simulink model "solar_pv_protected_c07_circuit"  (R2026b)
settings: Solver=VariableStepAuto
model workspace (MAT data in the model file):
  candidate_owner = 'pv_protection_integration_20261023_r01'
  solar_edit_metadata.source = 'micropython-connected-drawing-20261019-r03'
  solar_edit_metadata.transform.pixels_per_mm = 7.87401574803
  solar_edit_metadata.transform.offset_mm = [0 0]
  solar_edit_metadata.transform.offset_px = [80 80]
  solar_edit_metadata.behavior_models_implemented = 0
libraries: fl_lib x149, ee_lib x16, ltc4364demo_lib x3, batteryecm_lib x1, solarprotect_lib x1
(part 1 of 16)
settings Model: PreStartFcn=error('solar:NativeMigrationIncomplete','標準部品への移行版です。専用IC等の動作モデルと実部品パラメータを設定してから、試験計画に沿って実行してください。');  Creator=hosik  LastModifiedBy=hosik
settings SimscapeCC: SimscapeLogType=all  SimscapeNominalValues="[{\"value\":\"1\",\"unit\":\"A\"},{\"value\":\"1\",\"unit\":\"bar\"},{\"value\":\"1\",\"unit\":\"cm^2\"},{\"value\":\"1\",\"unit\":\"cm^3/s\"},{\"value\":\"1\",\"unit\":\"kJ/kg\"},{\"value\":\"1\",\"unit\":\"kW\"},{\"value\":\"1\",\"unit\":\"l\"},{\"value\":\"1\",\"unit\":\"N\"},{\"value\":\"1\",\"unit\":\"N*m\"},{\"value\":\"1\",\"unit\":\"V\"},{\"value\":\"0.001\",\"unit\":\"Wb\"}]"  SimscapeUseEnergyAccounting=off

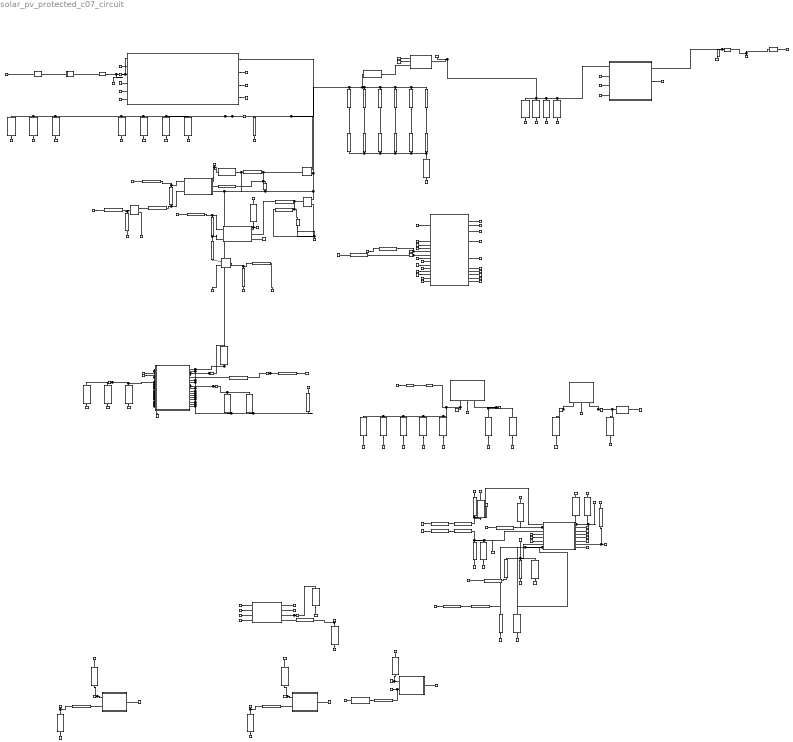
== system solar_pv_protected_c07_circuit ==
  note: 太陽光充電システム c07
  BT1 : batteryecm_lib/Battery  Description=|  Vnom=51.2 V  prm_dir=simscape.enum.battery.prm_dir.disabled  R1_dis=2 Ohm  R1_ch=2 Ohm  R1=2 Ohm  prm_AH=simscape.enum.battery.prm_AH.infinite  AH=100 A*hr  V1=11.5 V  AH1=25 A*hr  prm_R2=simscape.enum.battery.prm_R2.disabled  R2=2000 Ohm  Tmeas=298.15 K  charge_measurement_port=simscape.enum.battery.enable.no  prm_dyn=simscape.enum.battery.prm_dyn.off  Rp1=0.005 Ohm  tau1=30 s  Rp2=0.005 Ohm  tau2=30 s  Rp3=0.005 Ohm  tau3=30 s  Rp4=0.005 Ohm  tau4=30 s  Rp5=0.005 Ohm  tau5=30 s  prm_fade=simscape.enum.battery.prm_fade.disabled  N_fade=100  AH_fade=45 A*hr  R1_fade=2.02 Ohm  R1_ch_fade=2.02 Ohm  V1_fade=10.35 V  prm_age=simscape.enum.battery.prm_age.disabled  prm_age_OCV=simscape.enum.battery.prm_age_OCV.OCV  OCV_age=0.9  SOC_age=60  Tmeas_age=298.15 K  delta_time_age_vec=[0] d  temperature_age_vec=[273] K  OCV_scaling_age=2.2134e6  OCV_offset_age=1.632e6  temp_exp_age=0.515833569 V  t_exp_age=0.75  Vnom_T2=12 V  R1_T2=2.2 Ohm  R1_T2_dis=2.2 Ohm  R1_T2_ch=2.2 Ohm  V1_T2=11.4 V  R2_T2=2200 Ohm  Rp1_T2=0.005 Ohm  tau1_T2=30 s  Rp2_T2=0.005 Ohm  tau2_T2=30 s  Rp3_T2=0.005 Ohm  tau3_T2=30 s  Rp4_T2=0.005 Ohm  tau4_T2=30 s  Rp5_T2=0.005 Ohm  tau5_T2=30 s  Tmeas2=273.15 K  thermal_port=simscape.enum.thermaleffects.omit  thermal_mass=30000 J/K  i_specify=off  i_priority=None  i=0 A  i_nominal_specify=off  i_nominal_value=1  i_nominal_unit=A  v_specify=off  v_priority=None  v=0 V  v_nominal_specify=off  v_nominal_value=1  v_nominal_unit=V  charge_specify=off  charge_priority=High  charge=50 A*hr  charge_nominal_specify=off  charge_nominal_value=1  charge_nominal_unit=A*hr  num_cycles_specify=off  num_cycles_priority=High  num_cycles=0  num_cycles_nominal_specify=off  num_cycles_nominal_value=1  num_cycles_nominal_unit=1  temperature_specify=off  temperature_priority=High  temperature=298.15 K  temperature_nominal_specify=off  temperature_nominal_value=1  temperature_nominal_unit=K
      | この回路での名前　　; BT1
      | 部品名　　　　　　　; LiTime 51.2V 100Ah
      | この回路での役割　　; 太陽光で発電した電力を充電して蓄える、今回の設計対象の電池パック。
      | ここでの動き　　　　; 主充電経路から充電を受ける一方、別の補助電源分岐から制御回路などへ電力を供給する。充電器停止時にも電池側に電圧が残るため、逆流を防ぐ設計が必要になる。
      | 
      | 【詳しい働き・仕様・接続・確認の範囲】
      | 部品種別　　　　　　; 完成蓄電池パック
      | 公称値　　　　　　　; 51.2V 100Ah LiFePO4
      | 配置目的　　　　　　; 太陽光充電器の充電先。電池側に電圧源が存在することを表し、充電器停止時の逆流防止も検討対象にする。
      | 意図する動作　　　　; 公称51.2 V・100 AhのLiFePO4パックを設計対象とする。内部BMSの詳細動作、SOC・温度・内部抵抗の実測同定は未実施。
      | 端子と接続　　　　　; + + → BAT_RAW、- - → GND
      | モデルの範囲　　　　; Simscape電池ブロックへ既知の公称値を割り当てた図面用表現。LiTimeパックのSOC/温度依存・内部抵抗・BMSへ同定済みではない。
      | 確認の範囲　　　　　; 本説明は保存回路の部品情報・端子割当・既存設計意図を整理したもの。今回の説明更新によって新たな動作試験や実機検証を実施した意味ではない。
      | 設計記録　　　　　　; evaluation\component_annotations_20261022_r01\before_graph.json
      | evaluation\component_annotations_20261022_r01\before_metadata.json
      | evaluation\protection_capacitor_integration_20261021_r01\final_delivery\independent_readback\physical_bom.json
      | 
      | 【この説明欄の略語・記号】
      | 用語1　　　　　　　 ; BMS：Battery Management System（電池管理システム）。電池内部の監視・保護などを担当する仕組み。現モデルは実パックの詳細動作を同定したものではない。
      | 用語2　　　　　　　 ; SOC：State of Charge（充電状態）。電池に残る充電量の割合。電圧だけで正確に決まる量ではない。
      | 用語3　　　　　　　 ; LiFePO4：Lithium Iron Phosphate（リン酸鉄リチウム）。電池の正極材料を示す化学式。英語の頭文字を並べた略語ではない。
      | 用語4　　　　　　　 ; GND：Ground（回路の基準電位・電流帰路）。この図の共通基準。保護接地や大地への接続を意味するとは限らない。
      settings: AttributesFormatString=51.2V 100Ah LiFePO4
  C1 : fl_lib/Electrical/Electrical Elements/Capacitor  Description=|  c=2.2e-08 F  r=1e-6 Ohm  g=0 1/Ohm  i_specify=off  i_priority=None  i=0 A  i_nominal_specify=off  i_nominal_value=1  i_nominal_unit=A  v_specify=off  v_priority=None  v=0 V  v_nominal_specify=off  v_nominal_value=1  v_nominal_unit=V  vc_specify=off  vc_priority=High  vc=0 V  vc_nominal_specify=off  vc_nominal_value=1  vc_nominal_unit=V
      | この回路での名前　　; C1
      | 部品名　　　　　　　; C3225C0G2J223J230AA
      | この回路での役割　　; 主電力段のスイッチが切り替わった後に起こる、電圧の振動を抑えるためのコンデンサ。
      | ここでの動き　　　　; Q1・Q2の切替えで生じる振動に対し、抵抗R3〜R14と組み合わせて電流を流し、そのエネルギーを抵抗で消費する経路を作る。この組合せをスナバと呼ぶ。
      | 
      | 【詳しい働き・仕様・接続・確認の範囲】
      | 部品種別　　　　　　; 積層セラミックコンデンサ（MLCC）
      | 部品分類　　　　　　; 積層セラミックコンデンサ（MLCC）
      | 公称値　　　　　　　; 22 nF
      | 配置目的　　　　　　; SWスナバ。対象はQ1/Q2、R3〜R14、SW。
      | 意図する動作　　　　; スナバ抵抗とC1の往復ループをSW/QLソースに局所化。 スナバ機能は大容量CINと異なる。寄生・リンギング・パルス電力が未確認のため削除しない。
      | 端子と接続　　　　　; 1 p → SNUB_C、2 n → GND
      | モデルの範囲　　　　; Simscape標準コンデンサの集中定数表現。材質、DCバイアス、周波数依存ESR/ESL、寿命・温度特性を型番から自動再現するモデルではない。
      | モデル設定　　　　　; c=22 nF、r=1 µΩ、g=0 S。これらは保存モデルの設定値であり、すべてが実部品の保証値という意味ではない。
      | 損失の扱い　　　　　; 保存モデルの直列抵抗rと実部品の周波数・温度依存ESRは区別する。容量値が一致しても損失・リプル電流・寿命の成立確認にはならない。
      | 確認の範囲　　　　　; 本説明は保存回路の部品情報・端子割当・既存設計意図を整理したもの。今回の説明更新によって新たな動作試験や実機検証を実施した意味ではない。
      | 設計記録　　　　　　; evaluation\component_annotations_20261022_r01\before_graph.json
      | evaluation\component_annotations_20261022_r01\before_metadata.json
      | evaluation\protection_capacitor_integration_20261021_r01\final_delivery\independent_readback\physical_bom.json
      | evaluation\protection_capacitor_integration_20261021_r01\capacitor_review\capacitor_inventory_after_c04.json
      | 
      | 【周波数・ノイズと配置の説明】
      | 周波数面の役割　　　; スイッチング端の振動を抵抗と組み合わせて減衰させるスナバ容量。
      | 対象周波数の目安　　; 対象はQ1/Q2の切替えで励起される寄生共振の周波数。主スイッチング50 kHz仮定そのものより高い成分が対象になり得るが、現回路の共振周波数は未測定なのでMHzなどの固定値は割り当てない。
      | ノイズの発生源　　　; Q1/Q2、主配線の寄生インダクタンスとMOSFET等の寄生容量が、切替え時の急な電流・電圧変化によって振動する。
      | 他のコンデンサとの差; C8～C10は電源をまたぐバイパスで、本品22 nFはスナバ抵抗R3～R14と組み合わせて振動エネルギーを消費するための容量。
      | 周波数説明の範囲　　; この説明はスナバの設計意図。寄生共振、抵抗のパルス電力、損失、温度を含むこの値の最適性は未確認。
      | 周波数説明の根拠　　; 村田製作所：コンデンサのインピーダンス・ESRと周波数の関係
      | https://article.murata.com/en-global/article/impedance-esr-frequency-characteristics-in-capacitors
      | 
      | 【この説明欄の略語・記号】
      | 用語1　　　　　　　 ; MLCC：Multilayer Ceramic Capacitor（積層セラミックコンデンサ）。薄いセラミック誘電体と電極を重ねたコンデンサ。対象周波数は容量・実装・寄生成分で変わるため、MLCCという分類だけでは決めない。
      | 用語2　　　　　　　 ; ESR：Equivalent Series Resistance（等価直列抵抗）。コンデンサの損失を直列抵抗で表した量。周波数・温度で変わり、損失とリプル電圧に関係する。
      | 用語3　　　　　　　 ; ESL：Equivalent Series Inductance（等価直列インダクタンス）。端子や電極などの寄生インダクタンスを表す。高い周波数ではバイパス効果を制限する。
      | 用語4　　　　　　　 ; DC：Direct Current（直流）。ここでは直流電源または直流成分。DCバイアスはコンデンサに重なる直流電圧を指す。
      | 用語5　　　　　　　 ; MOSFET：Metal-Oxide-Semiconductor Field-Effect Transistor（金属・酸化膜・半導体構造の電界効果トランジスタ）。ゲートとソースの電圧でドレインとソースの導通を制御する素子。N-MOSはNチャネル型を表す。
      | 用語6　　　　　　　 ; GND：Ground（回路の基準電位・電流帰路）。この図の共通基準。保護接地や大地への接続を意味するとは限らない。
      | 用語7　　　　　　　 ; SW：Switching Node（スイッチング点）。主電力段の上下MOSFETとL1がつながる、電圧が高速に切り替わる点。GNDとは別電位。
      | 用語8　　　　　　　 ; CIN：Input Capacitor（入力側コンデンサ）。個別部品番号ではなく、入力側の容量群を指す機能名。
      | 用語9　　　　　　　 ; QH/QL：主電力段の上側・下側MOSFETを指す機能名。HはHigh側、LはLow側。この図のQ1/Q2との対応を回路説明で確認する。
      settings: AttributesFormatString=|
      | MLCC
      | 22 nF
  C10 : fl_lib/Electrical/Electrical Elements/Capacitor  Description=|  c=2.2000000000000001e-06 F  r=1e-6 Ohm  g=0 1/Ohm  i_specify=off  i_priority=None  i=0 A  i_nominal_specify=off  i_nominal_value=1  i_nominal_unit=A  v_specify=off  v_priority=None  v=0 V  v_nominal_specify=off  v_nominal_value=1  v_nominal_unit=V  vc_specify=off  vc_priority=High  vc=0 V  vc_nominal_specify=off  vc_nominal_value=1  vc_nominal_unit=V
      | この回路での名前　　; C10
      | 部品名　　　　　　　; C5750X7T2E225K250KE
      | この回路での役割　　; 主電力段のすぐ近くで速い電流変化を受け止め、遠い電源配線へ流れ出す高周波成分を減らすためのコンデンサ。
      | ここでの動き　　　　; 入力電源VINと共通GNDの間に2.2 µFを3個並列に置き、Q1・Q2が切り替わる瞬間の電流に短い往復経路を作る。C2〜C4の大きな電荷蓄積を補う役割。
      | 
      | 【詳しい働き・仕様・接続・確認の範囲】
      | 部品種別　　　　　　; 積層セラミックコンデンサ（MLCC）
      | 部品分類　　　　　　; 積層セラミックコンデンサ（MLCC）
      | 公称値　　　　　　　; 2.2 uF
      | 配置目的　　　　　　; 入力高速バイパス。対象はQ1ドレインとQ2ソース間のホットループ。
      | 意図する動作　　　　; 現構成は2.2 µFを3個。電力段付近でパルス電流の短い往復経路を作る意図。DCバイアス下の実効容量と高周波の分流・寄生は公称容量だけでは保証しない。
      | 端子と接続　　　　　; 2 n → GND、1 p → VIN
      | モデルの範囲　　　　; Simscape標準コンデンサの集中定数表現。材質、DCバイアス、周波数依存ESR/ESL、寿命・温度特性を型番から自動再現するモデルではない。
      | モデル設定　　　　　; c=2.2 µF、r=1 µΩ、g=0 S。これらは保存モデルの設定値であり、すべてが実部品の保証値という意味ではない。
      | 損失の扱い　　　　　; 保存モデルの直列抵抗rと実部品の周波数・温度依存ESRは区別する。容量値が一致しても損失・リプル電流・寿命の成立確認にはならない。
      | 確認の範囲　　　　　; 本説明は保存回路の部品情報・端子割当・既存設計意図を整理したもの。今回の説明更新によって新たな動作試験や実機検証を実施した意味ではない。
      | 設計記録　　　　　　; evaluation\component_annotations_20261022_r01\before_graph.json
      | evaluation\component_annotations_20261022_r01\before_metadata.json
      | evaluation\protection_capacitor_integration_20261021_r01\final_delivery\independent_readback\physical_bom.json
      | evaluation\protection_capacitor_integration_20261021_r01\capacitor_review\capacitor_inventory_after_c04.json
      | 
      | 【周波数・ノイズと配置の説明】
      | 材質の分類　　　　　; 本品の温度特性分類はX7T。-55～125 ℃の範囲で容量変化+22/-33%を規定する分類コードであり、英単語の略ではない。これは温度による変化の分類で、直流電圧を加えた際の実効容量や高周波特性は別に確認する。
      | 周波数面の役割　　　; 入力側の速い電流変化を電力段の近くで受け止め、遠い電源配線へ流れる高周波成分を減らす。
      | 対象周波数の目安　　; 主スイッチング周波数とその高調波、切替え端の速い変化を対象とする。主電力段の既存比較計算では50 kHzを仮定している。これは比較シナリオの値であり、今回の保存図から実行中PWM周波数を測定した値ではない。 50 kHzなら100 kHz、150 kHzなども成分となり、端の速さや寄生共振によってMHz域も検討対象になる。ただしMHz域での本品の有効性を保証した意味ではない。
      | ノイズの発生源　　　; Q1のオン期間に主電力段へ流れ込む入力電流が脈動し、Q1/Q2の切替え時には寄生容量の充放電電流も加わる。配線の寄生インダクタンスは急な電流変化を電圧の突起や振動に変える。
      | 他のコンデンサとの差; C2～C4の470 µF電解が比較的長い時間の電荷を補い、本品2.2 µFは短い局所経路を作る。C7フィルムとも分担し、3種類の役割には重なりがある。
      | 周波数説明の範囲　　; 狙うノイズの周波数と、この部品が実装後に有効な周波数範囲は別である。実効容量、等価直列抵抗、等価直列インダクタンス、配線を含む自己共振で変わるため、型番名や公称容量だけから有効帯域の上限を断定しない。
      | 周波数説明の根拠　　; TDK：C5750X7T2E225K250KE
      | https://product.tdk.com/ja/search/capacitor/ceramic/mlcc/info?part_no=C5750X7T2E225K250KE
      | 村田製作所：コンデンサのインピーダンス・ESRと周波数の関係
      | https://article.murata.com/en-global/article/impedance-esr-frequency-characteristics-in-capacitors
      | 村田製作所：コンデンサを使いこなす
      | https://www.murata.com/en-GB/products/emc/emifil/library/knowhow/basic/chapter06-p8
      | 
      | 【この説明欄の略語・記号】
      | 用語1　　　　　　　 ; MLCC：Multilayer Ceramic Capacitor（積層セラミックコンデンサ）。薄いセラミック誘電体と電極を重ねたコンデンサ。対象周波数は容量・実装・寄生成分で変わるため、MLCCという分類だけでは決めない。
      | 用語2　　　　　　　 ; ESR：Equivalent Series Resistance（等価直列抵抗）。コンデンサの損失を直列抵抗で表した量。周波数・温度で変わり、損失とリプル電圧に関係する。
      | 用語3　　　　　　　 ; ESL：Equivalent Series Inductance（等価直列インダクタンス）。端子や電極などの寄生インダクタンスを表す。高い周波数ではバイパス効果を制限する。
      | 用語4　　　　　　　 ; DC：Direct Current（直流）。ここでは直流電源または直流成分。DCバイアスはコンデンサに重なる直流電圧を指す。
      | 用語5　　　　　　　 ; X7T：セラミックコンデンサの温度特性記号。英語の頭文字ではなく分類コード。X＝下限−55 ℃、7＝上限+125 ℃、T＝容量変化+22%/−33%。直流バイアスによる容量変化は別に確認する。
      | 用語6　　　　　　　 ; PWM：Pulse Width Modulation（パルス幅変調）。周期に対するON時間の割合を変えて、スイッチの平均的な電力伝達を調整する方式。
      | 用語7　　　　　　　 ; GND：Ground（回路の基準電位・電流帰路）。この図の共通基準。保護接地や大地への接続を意味するとは限らない。
      | 用語8　　　　　　　 ; VIN/VOUT：入力電圧・出力電圧を表す端子／ネット名。INは入力、OUTは出力。電源変換器の電力端子なのか、検出用端子なのかは対象部品によって異なるため、端子と接続の説明に従う。
      settings: AttributesFormatString=|
      | MLCC
      | 2.2 µF
  C13 : fl_lib/Electrical/Electrical Elements/Capacitor  Description=|  c=0.00047 F  r=1e-6 Ohm  g=0 1/Ohm  i_specify=off  i_priority=None  i=0 A  i_nominal_specify=off  i_nominal_value=1  i_nominal_unit=A  v_specify=off  v_priority=None  v=0 V  v_nominal_specify=off  v_nominal_value=1  v_nominal_unit=V  vc_specify=off  vc_priority=High  vc=0 V  vc_nominal_specify=off  vc_nominal_value=1  vc_nominal_unit=V
      | この回路での名前　　; C13
      | 部品名　　　　　　　; 100ZLH470MEFC16X31.5
      | この回路での役割　　; インダクタL1から入る電流とバッテリーへ送る電流の差を、電荷の出し入れで一時的に受け持ち、降圧回路の出力電圧をならすためのコンデンサ。
      | ここでの動き　　　　; インダクタL1と電流検出抵抗R2を通った後の出力VOUTと共通GNDの間に、470 µFを2個並列に置く。保護回路が遮断すると、VOUTからバッテリー側のP_COUTへ向かう正側の給電経路が切り離される。GND側の基準は共通のまま。
      | 
      | 【詳しい働き・仕様・接続・確認の範囲】
      | 部品種別　　　　　　; アルミ電解コンデンサ（有極性）
      | 部品分類　　　　　　; アルミ電解コンデンサ（有極性）
      | 公称値　　　　　　　; 470 uF
      | 配置目的　　　　　　; 出力バルク。対象はL1・R2の後のVOUT、保護回路の入力側。
      | 意図する動作　　　　; 大容量電解として出力の電荷・エネルギーを受け持つ。C15/C16の高速バイパスと併用する。保護OFF時、下流BAT_PLUSのP_COUTとは別ノードになる。
      | 端子と接続　　　　　; 1 p → VOUT、2 n → GND
      | 比較する部品　　　　; C15/C16はMLCC 10 µF。本品は電解470 µFであり、同じ容量・材質の部品ではない。
      | モデルの範囲　　　　; Simscape標準コンデンサの集中定数表現。材質、DCバイアス、周波数依存ESR/ESL、寿命・温度特性を型番から自動再現するモデルではない。
      | モデル設定　　　　　; c=470 µF、r=1 µΩ、g=0 S。これらは保存モデルの設定値であり、すべてが実部品の保証値という意味ではない。
      | 損失の扱い　　　　　; 保存モデルの直列抵抗rと実部品の周波数・温度依存ESRは区別する。容量値が一致しても損失・リプル電流・寿命の成立確認にはならない。
      | 確認の範囲　　　　　; 本説明は保存回路の部品情報・端子割当・既存設計意図を整理したもの。今回の説明更新によって新たな動作試験や実機検証を実施した意味ではない。
      | 設計記録　　　　　　; evaluation\component_annotations_20261022_r01\before_graph.json
      | evaluation\component_annotations_20261022_r01\before_metadata.json
      | evaluation\protection_capacitor_integration_20261021_r01\final_delivery\independent_readback\physical_bom.json
      | evaluation\protection_capacitor_integration_20261021_r01\capacitor_review\capacitor_inventory_after_c04.json
      | 
      | 【周波数・ノイズと配置の説明】
      | 周波数面の役割　　　; 出力側で電荷を蓄え、インダクタ電流とバッテリーへ送る電流の差を受け止める。
      | 対象周波数の目安　　; 負荷や制御の変化による低い周波数側と、主スイッチング周期に残る出力リプルを対象とする。主電力段の既存比較計算では50 kHzを仮定している。これは比較シナリオの値であり、今回の保存図から実行中PWM周波数を測定した値ではない。
      | ノイズの発生源　　　; L1の電流はスイッチング周期で増減する。この電流と下流へ流れる電流の差がコンデンサへ入り、出力電圧の脈動を生む。
      | 他のコンデンサとの差; 470 µF×2個は蓄積量を担当し、10 µFのC15/C16はより速い高調波・突起への局所帰路を補う。保護出力側のP_COUTとは遮断時に別ノードとなる。
      | 周波数説明の範囲　　; 狙うノイズの周波数と、この部品が実装後に有効な周波数範囲は別である。実効容量、等価直列抵抗、等価直列インダクタンス、配線を含む自己共振で変わるため、型番名や公称容量だけから有効帯域の上限を断定しない。
      | 周波数説明の根拠　　; 村田製作所：コンデンサのインピーダンス・ESRと周波数の関係
      | https://article.murata.com/en-global/article/impedance-esr-frequency-characteristics-in-capacitors
      | 村田製作所：コンデンサを使いこなす
      | https://www.murata.com/en-GB/products/emc/emifil/library/knowhow/basic/chapter06-p8
      | 
      | 【この説明欄の略語・記号】
      | 用語1　　　　　　　 ; MLCC：Multilayer Ceramic Capacitor（積層セラミックコンデンサ）。薄いセラミック誘電体と電極を重ねたコンデンサ。対象周波数は容量・実装・寄生成分で変わるため、MLCCという分類だけでは決めない。
      | 用語2　　　　　　　 ; ESR：Equivalent Series Resistance（等価直列抵抗）。コンデンサの損失を直列抵抗で表した量。周波数・温度で変わり、損失とリプル電圧に関係する。
      | 用語3　　　　　　　 ; ESL：Equivalent Series Inductance（等価直列インダクタンス）。端子や電極などの寄生インダクタンスを表す。高い周波数ではバイパス効果を制限する。
      | 用語4　　　　　　　 ; DC：Direct Current（直流）。ここでは直流電源または直流成分。DCバイアスはコンデンサに重なる直流電圧を指す。
      | 用語5　　　　　　　 ; PWM：Pulse Width Modulation（パルス幅変調）。周期に対するON時間の割合を変えて、スイッチの平均的な電力伝達を調整する方式。
      | 用語6　　　　　　　 ; GND：Ground（回路の基準電位・電流帰路）。この図の共通基準。保護接地や大地への接続を意味するとは限らない。
      | 用語7　　　　　　　 ; VIN/VOUT：入力電圧・出力電圧を表す端子／ネット名。INは入力、OUTは出力。電源変換器の電力端子なのか、検出用端子なのかは対象部品によって異なるため、端子と接続の説明に従う。
      settings: AttributesFormatString=|
      | 電解
      | 470 µF
  C14 : fl_lib/Electrical/Electrical Elements/Capacitor  Description=|  c=0.00047 F  r=1e-6 Ohm  g=0 1/Ohm  i_specify=off  i_priority=None  i=0 A  i_nominal_specify=off  i_nominal_value=1  i_nominal_unit=A  v_specify=off  v_priority=None  v=0 V  v_nominal_specify=off  v_nominal_value=1  v_nominal_unit=V  vc_specify=off  vc_priority=High  vc=0 V  vc_nominal_specify=off  vc_nominal_value=1  vc_nominal_unit=V
      | この回路での名前　　; C14
      | 部品名　　　　　　　; 100ZLH470MEFC16X31.5
      | この回路での役割　　; インダクタL1から入る電流とバッテリーへ送る電流の差を、電荷の出し入れで一時的に受け持ち、降圧回路の出力電圧をならすためのコンデンサ。
      | ここでの動き　　　　; インダクタL1と電流検出抵抗R2を通った後の出力VOUTと共通GNDの間に、470 µFを2個並列に置く。保護回路が遮断すると、VOUTからバッテリー側のP_COUTへ向かう正側の給電経路が切り離される。GND側の基準は共通のまま。
      | 
      | 【詳しい働き・仕様・接続・確認の範囲】
      | 部品種別　　　　　　; アルミ電解コンデンサ（有極性）
      | 部品分類　　　　　　; アルミ電解コンデンサ（有極性）
      | 公称値　　　　　　　; 470 uF
      | 配置目的　　　　　　; 出力バルク。対象はL1・R2の後のVOUT、保護回路の入力側。
      | 意図する動作　　　　; 大容量電解として出力の電荷・エネルギーを受け持つ。C15/C16の高速バイパスと併用する。保護OFF時、下流BAT_PLUSのP_COUTとは別ノードになる。
      | 端子と接続　　　　　; 1 p → VOUT、2 n → GND
      | 比較する部品　　　　; C15/C16はMLCC 10 µF。本品は電解470 µFであり、同じ容量・材質の部品ではない。
      | モデルの範囲　　　　; Simscape標準コンデンサの集中定数表現。材質、DCバイアス、周波数依存ESR/ESL、寿命・温度特性を型番から自動再現するモデルではない。
      | モデル設定　　　　　; c=470 µF、r=1 µΩ、g=0 S。これらは保存モデルの設定値であり、すべてが実部品の保証値という意味ではない。
      | 損失の扱い　　　　　; 保存モデルの直列抵抗rと実部品の周波数・温度依存ESRは区別する。容量値が一致しても損失・リプル電流・寿命の成立確認にはならない。
      | 確認の範囲　　　　　; 本説明は保存回路の部品情報・端子割当・既存設計意図を整理したもの。今回の説明更新によって新たな動作試験や実機検証を実施した意味ではない。
      | 設計記録　　　　　　; evaluation\component_annotations_20261022_r01\before_graph.json
      | evaluation\component_annotations_20261022_r01\before_metadata.json
      | evaluation\protection_capacitor_integration_20261021_r01\final_delivery\independent_readback\physical_bom.json
      | evaluation\protection_capacitor_integration_20261021_r01\capacitor_review\capacitor_inventory_after_c04.json
      | 
      | 【周波数・ノイズと配置の説明】
      | 周波数面の役割　　　; 出力側で電荷を蓄え、インダクタ電流とバッテリーへ送る電流の差を受け止める。
      | 対象周波数の目安　　; 負荷や制御の変化による低い周波数側と、主スイッチング周期に残る出力リプルを対象とする。主電力段の既存比較計算では50 kHzを仮定している。これは比較シナリオの値であり、今回の保存図から実行中PWM周波数を測定した値ではない。
      | ノイズの発生源　　　; L1の電流はスイッチング周期で増減する。この電流と下流へ流れる電流の差がコンデンサへ入り、出力電圧の脈動を生む。
      | 他のコンデンサとの差; 470 µF×2個は蓄積量を担当し、10 µFのC15/C16はより速い高調波・突起への局所帰路を補う。保護出力側のP_COUTとは遮断時に別ノードとなる。
      | 周波数説明の範囲　　; 狙うノイズの周波数と、この部品が実装後に有効な周波数範囲は別である。実効容量、等価直列抵抗、等価直列インダクタンス、配線を含む自己共振で変わるため、型番名や公称容量だけから有効帯域の上限を断定しない。
      | 周波数説明の根拠　　; 村田製作所：コンデンサのインピーダンス・ESRと周波数の関係
      | https://article.murata.com/en-global/article/impedance-esr-frequency-characteristics-in-capacitors
      | 村田製作所：コンデンサを使いこなす
      | https://www.murata.com/en-GB/products/emc/emifil/library/knowhow/basic/chapter06-p8
      | 
      | 【この説明欄の略語・記号】
      | 用語1　　　　　　　 ; MLCC：Multilayer Ceramic Capacitor（積層セラミックコンデンサ）。薄いセラミック誘電体と電極を重ねたコンデンサ。対象周波数は容量・実装・寄生成分で変わるため、MLCCという分類だけでは決めない。
      | 用語2　　　　　　　 ; ESR：Equivalent Series Resistance（等価直列抵抗）。コンデンサの損失を直列抵抗で表した量。周波数・温度で変わり、損失とリプル電圧に関係する。
      | 用語3　　　　　　　 ; ESL：Equivalent Series Inductance（等価直列インダクタンス）。端子や電極などの寄生インダクタンスを表す。高い周波数ではバイパス効果を制限する。
      | 用語4　　　　　　　 ; DC：Direct Current（直流）。ここでは直流電源または直流成分。DCバイアスはコンデンサに重なる直流電圧を指す。
      | 用語5　　　　　　　 ; PWM：Pulse Width Modulation（パルス幅変調）。周期に対するON時間の割合を変えて、スイッチの平均的な電力伝達を調整する方式。
      | 用語6　　　　　　　 ; GND：Ground（回路の基準電位・電流帰路）。この図の共通基準。保護接地や大地への接続を意味するとは限らない。
      | 用語7　　　　　　　 ; VIN/VOUT：入力電圧・出力電圧を表す端子／ネット名。INは入力、OUTは出力。電源変換器の電力端子なのか、検出用端子なのかは対象部品によって異なるため、端子と接続の説明に従う。
      settings: AttributesFormatString=|
      | 電解
      | 470 µF
  C15 : fl_lib/Electrical/Electrical Elements/Capacitor  Description=|  c=1e-05 F  r=1e-6 Ohm  g=0 1/Ohm  i_specify=off  i_priority=None  i=0 A  i_nominal_specify=off  i_nominal_value=1  i_nominal_unit=A  v_specify=off  v_priority=None  v=0 V  v_nominal_specify=off  v_nominal_value=1  v_nominal_unit=V  vc_specify=off  vc_priority=High  vc=0 V  vc_nominal_specify=off  vc_nominal_value=1  vc_nominal_unit=V
      | この回路での名前　　; C15
      | 部品名　　　　　　　; GRM32EC72A106KE05L
      | この回路での役割　　; 降圧回路の出力側で速い電圧・電流の変化を受け止め、大容量の出力コンデンサを補うためのコンデンサ。
      | ここでの動き　　　　; 出力VOUTと共通GNDの間で、高周波の電流が近くを往復する経路を作る。電荷を多く蓄えるC13・C14と併用し、保護回路へ入る電源の変動を抑える設計。
      | 
      | 【詳しい働き・仕様・接続・確認の範囲】
      | 部品種別　　　　　　; 積層セラミックコンデンサ（MLCC）
      | 部品分類　　　　　　; 積層セラミックコンデンサ（MLCC）
      | 公称値　　　　　　　; 10 uF
      | 配置目的　　　　　　; 出力高速バイパス。対象はVOUT、出力バルク、保護VIN。
      | 意図する動作　　　　; MLCCとして出力側の高周波電流を局所的に受け持ち、C13/C14の大容量電解を補う。同じVOUT–GND接続でも材質・容量・周波数特性と役割が異なる。DCバイアス下の実効容量は10 µFより小さくなり得る。
      | 端子と接続　　　　　; 1 p → VOUT、2 n → GND
      | 比較する部品　　　　; C13/C14は電解470 µF。本品はMLCC 10 µF。並列でも担当する周波数域・電荷量・実効容量の条件が異なる。
      | モデルの範囲　　　　; Simscape標準コンデンサの集中定数表現。材質、DCバイアス、周波数依存ESR/ESL、寿命・温度特性を型番から自動再現するモデルではない。
      | モデル設定　　　　　; c=10 µF、r=1 µΩ、g=0 S。これらは保存モデルの設定値であり、すべてが実部品の保証値という意味ではない。
      | 損失の扱い　　　　　; 保存モデルの直列抵抗rと実部品の周波数・温度依存ESRは区別する。容量値が一致しても損失・リプル電流・寿命の成立確認にはならない。
      | 確認の範囲　　　　　; 本説明は保存回路の部品情報・端子割当・既存設計意図を整理したもの。今回の説明更新によって新たな動作試験や実機検証を実施した意味ではない。
      | 設計記録　　　　　　; evaluation\component_annotations_20261022_r01\before_graph.json
      | evaluation\component_annotations_20261022_r01\before_metadata.json
      | evaluation\protection_capacitor_integration_20261021_r01\final_delivery\independent_readback\physical_bom.json
      | evaluation\protection_capacitor_integration_20261021_r01\capacitor_review\capacitor_inventory_after_c04.json
      | 
      | 【周波数・ノイズと配置の説明】
      | 材質の分類　　　　　; 本品の温度特性分類はX7S。-55～125 ℃の範囲で容量変化±22%を規定する分類コードであり、英単語の略ではない。これは温度による変化の分類で、直流電圧を加えた際の実効容量や高周波特性は別に確認する。
      | 周波数面の役割　　　; 出力側の高周波電流を局所的に受け、C13/C14の電解を補う。
      | 対象周波数の目安　　; 主スイッチングの高調波や切替え端から結合する高周波成分を対象にする。主電力段の既存比較計算では50 kHzを仮定している。これは比較シナリオの値であり、今回の保存図から実行中PWM周波数を測定した値ではない。 MHz域まで調べるべき成分があり得るが、本品の有効帯域や実回路のノイズ分布は未測定。
      | ノイズの発生源　　　; L1のリプル電流、Q1/Q2の切替え、寄生容量/共通配線を通る結合が出力側に影響する。
      | 他のコンデンサとの差; C13/C14の470 µF電解と比較すると公称容量は小さいが、短い配線と低い寄生成分で速い変化への経路を作る意図。10 µFは直流電圧印加時の実効容量保証値ではない。
      | 周波数説明の範囲　　; 狙うノイズの周波数と、この部品が実装後に有効な周波数範囲は別である。実効容量、等価直列抵抗、等価直列インダクタンス、配線を含む自己共振で変わるため、型番名や公称容量だけから有効帯域の上限を断定しない。
      | 周波数説明の根拠　　; 村田製作所：GRM32EC72A106KE05 Reference Sheet
      | https://search.murata.co.jp/Ceramy/image/img/A01X/G101/ENG/GRM32EC72A106KE05-01.pdf
      | 村田製作所：コンデンサのインピーダンス・ESRと周波数の関係
      | https://article.murata.com/en-global/article/impedance-esr-frequency-characteristics-in-capacitors
      | 村田製作所：コンデンサを使いこなす
      | https://www.murata.com/en-GB/products/emc/emifil/library/knowhow/basic/chapter06-p8
      | TDK：電解コンデンサからMLCCへの置換ガイド
      | https://product.tdk.com/en/techlibrary/solutionguide/mlcc_replace-guide.html
      | 
      | 【この説明欄の略語・記号】
      | 用語1　　　　　　　 ; MLCC：Multilayer Ceramic Capacitor（積層セラミックコンデンサ）。薄いセラミック誘電体と電極を重ねたコンデンサ。対象周波数は容量・実装・寄生成分で変わるため、MLCCという分類だけでは決めない。
      | 用語2　　　　　　　 ; ESR：Equivalent Series Resistance（等価直列抵抗）。コンデンサの損失を直列抵抗で表した量。周波数・温度で変わり、損失とリプル電圧に関係する。
      | 用語3　　　　　　　 ; ESL：Equivalent Series Inductance（等価直列インダクタンス）。端子や電極などの寄生インダクタンスを表す。高い周波数ではバイパス効果を制限する。
      | 用語4　　　　　　　 ; DC：Direct Current（直流）。ここでは直流電源または直流成分。DCバイアスはコンデンサに重なる直流電圧を指す。
      | 用語5　　　　　　　 ; X7S：セラミックコンデンサの温度特性記号。英語の頭文字ではなく分類コード。X＝下限−55 ℃、7＝上限+125 ℃、S＝その範囲の容量変化±22%。直流バイアスによる容量変化は別に確認する。
      | 用語6　　　　　　　 ; PWM：Pulse Width Modulation（パルス幅変調）。周期に対するON時間の割合を変えて、スイッチの平均的な電力伝達を調整する方式。
      | 用語7　　　　　　　 ; GND：Ground（回路の基準電位・電流帰路）。この図の共通基準。保護接地や大地への接続を意味するとは限らない。
      | 用語8　　　　　　　 ; VIN/VOUT：入力電圧・出力電圧を表す端子／ネット名。INは入力、OUTは出力。電源変換器の電力端子なのか、検出用端子なのかは対象部品によって異なるため、端子と接続の説明に従う。
      settings: AttributesFormatString=|
      | MLCC
      | 10 µF
  C16 : fl_lib/Electrical/Electrical Elements/Capacitor  Description=|  c=1e-05 F  r=1e-6 Ohm  g=0 1/Ohm  i_specify=off  i_priority=None  i=0 A  i_nominal_specify=off  i_nominal_value=1  i_nominal_unit=A  v_specify=off  v_priority=None  v=0 V  v_nominal_specify=off  v_nominal_value=1  v_nominal_unit=V  vc_specify=off  vc_priority=High  vc=0 V  vc_nominal_specify=off  vc_nominal_value=1  vc_nominal_unit=V
      | この回路での名前　　; C16
      | 部品名　　　　　　　; GRM32EC72A106KE05L
      | この回路での役割　　; 降圧回路の出力側で速い電圧・電流の変化を受け止め、大容量の出力コンデンサを補うためのコンデンサ。
      | ここでの動き　　　　; 出力VOUTと共通GNDの間で、高周波の電流が近くを往復する経路を作る。電荷を多く蓄えるC13・C14と併用し、保護回路へ入る電源の変動を抑える設計。
      | 
      | 【詳しい働き・仕様・接続・確認の範囲】
      | 部品種別　　　　　　; 積層セラミックコンデンサ（MLCC）
      | 部品分類　　　　　　; 積層セラミックコンデンサ（MLCC）
      | 公称値　　　　　　　; 10 uF
      | 配置目的　　　　　　; 出力高速バイパス。対象はVOUT、出力バルク、保護VIN。
      | 意図する動作　　　　; MLCCとして出力側の高周波電流を局所的に受け持ち、C13/C14の大容量電解を補う。同じVOUT–GND接続でも材質・容量・周波数特性と役割が異なる。DCバイアス下の実効容量は10 µFより小さくなり得る。
      | 端子と接続　　　　　; 1 p → VOUT、2 n → GND
      | 比較する部品　　　　; C13/C14は電解470 µF。本品はMLCC 10 µF。並列でも担当する周波数域・電荷量・実効容量の条件が異なる。
      | モデルの範囲　　　　; Simscape標準コンデンサの集中定数表現。材質、DCバイアス、周波数依存ESR/ESL、寿命・温度特性を型番から自動再現するモデルではない。
      | モデル設定　　　　　; c=10 µF、r=1 µΩ、g=0 S。これらは保存モデルの設定値であり、すべてが実部品の保証値という意味ではない。
      | 損失の扱い　　　　　; 保存モデルの直列抵抗rと実部品の周波数・温度依存ESRは区別する。容量値が一致しても損失・リプル電流・寿命の成立確認にはならない。
      | 確認の範囲　　　　　; 本説明は保存回路の部品情報・端子割当・既存設計意図を整理したもの。今回の説明更新によって新たな動作試験や実機検証を実施した意味ではない。
      | 設計記録　　　　　　; evaluation\component_annotations_20261022_r01\before_graph.json
      | evaluation\component_annotations_20261022_r01\before_metadata.json
      | evaluation\protection_capacitor_integration_20261021_r01\final_delivery\independent_readback\physical_bom.json
      | evaluation\protection_capacitor_integration_20261021_r01\capacitor_review\capacitor_inventory_after_c04.json
      | 
      | 【周波数・ノイズと配置の説明】
      | 材質の分類　　　　　; 本品の温度特性分類はX7S。-55～125 ℃の範囲で容量変化±22%を規定する分類コードであり、英単語の略ではない。これは温度による変化の分類で、直流電圧を加えた際の実効容量や高周波特性は別に確認する。
      | 周波数面の役割　　　; 出力側の高周波電流を局所的に受け、C13/C14の電解を補う。
      | 対象周波数の目安　　; 主スイッチングの高調波や切替え端から結合する高周波成分を対象にする。主電力段の既存比較計算では50 kHzを仮定している。これは比較シナリオの値であり、今回の保存図から実行中PWM周波数を測定した値ではない。 MHz域まで調べるべき成分があり得るが、本品の有効帯域や実回路のノイズ分布は未測定。
      | ノイズの発生源　　　; L1のリプル電流、Q1/Q2の切替え、寄生容量/共通配線を通る結合が出力側に影響する。
      | 他のコンデンサとの差; C13/C14の470 µF電解と比較すると公称容量は小さいが、短い配線と低い寄生成分で速い変化への経路を作る意図。10 µFは直流電圧印加時の実効容量保証値ではない。
      | 周波数説明の範囲　　; 狙うノイズの周波数と、この部品が実装後に有効な周波数範囲は別である。実効容量、等価直列抵抗、等価直列インダクタンス、配線を含む自己共振で変わるため、型番名や公称容量だけから有効帯域の上限を断定しない。
      | 周波数説明の根拠　　; 村田製作所：GRM32EC72A106KE05 Reference Sheet
      | https://search.murata.co.jp/Ceramy/image/img/A01X/G101/ENG/GRM32EC72A106KE05-01.pdf
      | 村田製作所：コンデンサのインピーダンス・ESRと周波数の関係
      | https://article.murata.com/en-global/article/impedance-esr-frequency-characteristics-in-capacitors
      | 村田製作所：コンデンサを使いこなす
      | https://www.murata.com/en-GB/products/emc/emifil/library/knowhow/basic/chapter06-p8
      | TDK：電解コンデンサからMLCCへの置換ガイド
      | https://product.tdk.com/en/techlibrary/solutionguide/mlcc_replace-guide.html
      | 
      | 【この説明欄の略語・記号】
      | 用語1　　　　　　　 ; MLCC：Multilayer Ceramic Capacitor（積層セラミックコンデンサ）。薄いセラミック誘電体と電極を重ねたコンデンサ。対象周波数は容量・実装・寄生成分で変わるため、MLCCという分類だけでは決めない。
      | 用語2　　　　　　　 ; ESR：Equivalent Series Resistance（等価直列抵抗）。コンデンサの損失を直列抵抗で表した量。周波数・温度で変わり、損失とリプル電圧に関係する。
      | 用語3　　　　　　　 ; ESL：Equivalent Series Inductance（等価直列インダクタンス）。端子や電極などの寄生インダクタンスを表す。高い周波数ではバイパス効果を制限する。
      | 用語4　　　　　　　 ; DC：Direct Current（直流）。ここでは直流電源または直流成分。DCバイアスはコンデンサに重なる直流電圧を指す。
      | 用語5　　　　　　　 ; X7S：セラミックコンデンサの温度特性記号。英語の頭文字ではなく分類コード。X＝下限−55 ℃、7＝上限+125 ℃、S＝その範囲の容量変化±22%。直流バイアスによる容量変化は別に確認する。
      | 用語6　　　　　　　 ; PWM：Pulse Width Modulation（パルス幅変調）。周期に対するON時間の割合を変えて、スイッチの平均的な電力伝達を調整する方式。
      | 用語7　　　　　　　 ; GND：Ground（回路の基準電位・電流帰路）。この図の共通基準。保護接地や大地への接続を意味するとは限らない。
      | 用語8　　　　　　　 ; VIN/VOUT：入力電圧・出力電圧を表す端子／ネット名。INは入力、OUTは出力。電源変換器の電力端子なのか、検出用端子なのかは対象部品によって異なるため、端子と接続の説明に従う。
      settings: AttributesFormatString=|
      | MLCC
      | 10 µF
  C17 : fl_lib/Electrical/Electrical Elements/Capacitor  Description=|  c=1e-07 F  r=1e-6 Ohm  g=0 1/Ohm  i_specify=off  i_priority=None  i=0 A  i_nominal_specify=off  i_nominal_value=1  i_nominal_unit=A  v_specify=off  v_priority=None  v=0 V  v_nominal_specify=off  v_nominal_value=1  v_nominal_unit=V  vc_specify=off  vc_priority=High  vc=0 V  vc_nominal_specify=off  vc_nominal_value=1  vc_nominal_unit=V
      | この回路での名前　　; C17
      | 部品名　　　　　　　; C0805C104K4RACTU
      | この回路での役割　　; 測定電圧を数値に変換するU1の3.3 V電源を、瞬間的な変動から支えるためのコンデンサ。
      | ここでの動き　　　　; U1の電源端子の近くで一時的な電流を供給し、高周波の電流に短い帰り道を作る。離れた電源側の容量だけに任せず、U1自身の近くに置く役割。
      | 
      | 【詳しい働き・仕様・接続・確認の範囲】
      | 部品種別　　　　　　; 積層セラミックコンデンサ（MLCC）
      | 部品分類　　　　　　; 積層セラミックコンデンサ（MLCC）
      | 公称値　　　　　　　; 100 nF
      | 配置目的　　　　　　; ADC電源バイパス。対象ICはU1（MCP3208-CI/SL）。
      | 意図する動作　　　　; U1電源ピン直近、静かな帰路。SPIやゲート帰路と共有インピーダンスを抑える。 100nF局所バイパス。C18やPico搭載Cは配線インダクタンス越しの代替にならない。
      | 端子と接続　　　　　; 1 1 → 3V3、2 2 → GND
      | モデルの範囲　　　　; Simscape標準コンデンサの集中定数表現。材質、DCバイアス、周波数依存ESR/ESL、寿命・温度特性を型番から自動再現するモデルではない。
      | モデル設定　　　　　; c=100 nF、r=1 µΩ、g=0 S。これらは保存モデルの設定値であり、すべてが実部品の保証値という意味ではない。
      | 損失の扱い　　　　　; 保存モデルの直列抵抗rと実部品の周波数・温度依存ESRは区別する。容量値が一致しても損失・リプル電流・寿命の成立確認にはならない。
      | 確認の範囲　　　　　; 本説明は保存回路の部品情報・端子割当・既存設計意図を整理したもの。今回の説明更新によって新たな動作試験や実機検証を実施した意味ではない。
      | 設計記録　　　　　　; evaluation\component_annotations_20261022_r01\before_graph.json
      | evaluation\component_annotations_20261022_r01\before_metadata.json
      | evaluation\protection_capacitor_integration_20261021_r01\final_delivery\independent_readback\physical_bom.json
      | evaluation\protection_capacitor_integration_20261021_r01\capacitor_review\capacitor_inventory_after_c04.json
      | evaluation\layout_readability_20261022_r01\capacitor_review\exact_snapshot_capacitor_review.json
      | 
      | 【周波数・ノイズと配置の説明】
      | 周波数面の役割　　　; U1（MCP3208、アナログ電圧を数値に変換するIC）の電源端子直近で、瞬間的な電流を供給する局所バイパス。
      | 対象周波数の目安　　; そのICの内部動作や周辺の通信、周囲のスイッチングによる高周波成分を対象にする。100 nFという容量だけから「何MHzまで効く」とは決められない。
      | ノイズの発生源　　　; IC内部の回路動作に伴う電源電流の変化、3.3 V配線を経由する電源変動、近傍のデジタル信号やゲート駆動からの結合。
      | 他のコンデンサとの差; 離れたC18や電源装置側の大きな容量は低い周波数側の蓄積を補う。配線の寄生インダクタンスがあるため、同じ電源ネットでもIC直近の本品を完全に代替できない。
      | 周波数説明の範囲　　; 狙うノイズの周波数と、この部品が実装後に有効な周波数範囲は別である。実効容量、等価直列抵抗、等価直列インダクタンス、配線を含む自己共振で変わるため、型番名や公称容量だけから有効帯域の上限を断定しない。
      | 周波数説明の根拠　　; TDK：Low-ESL Multilayer Ceramic Capacitors
      | https://product.tdk.com/system/files/dam/doc/content/emc-guidebook/en/eemc_product_01.pdf
      | 村田製作所：コンデンサを使いこなす
      | https://www.murata.com/en-GB/products/emc/emifil/library/knowhow/basic/chapter06-p8
      | 
      | 【この説明欄の略語・記号】
      | 用語1　　　　　　　 ; MLCC：Multilayer Ceramic Capacitor（積層セラミックコンデンサ）。薄いセラミック誘電体と電極を重ねたコンデンサ。対象周波数は容量・実装・寄生成分で変わるため、MLCCという分類だけでは決めない。
      | 用語2　　　　　　　 ; ESR：Equivalent Series Resistance（等価直列抵抗）。コンデンサの損失を直列抵抗で表した量。周波数・温度で変わり、損失とリプル電圧に関係する。
      | 用語3　　　　　　　 ; ESL：Equivalent Series Inductance（等価直列インダクタンス）。端子や電極などの寄生インダクタンスを表す。高い周波数ではバイパス効果を制限する。
      | 用語4　　　　　　　 ; DC：Direct Current（直流）。ここでは直流電源または直流成分。DCバイアスはコンデンサに重なる直流電圧を指す。
      | 用語5　　　　　　　 ; ADC：Analog-to-Digital Converter（アナログ・デジタル変換器）。測定電圧をデジタル値へ変換する回路。電流や温度も、センサーで電圧へ変換した後に読み取る。
      | 用語6　　　　　　　 ; IC：Integrated Circuit（集積回路）。複数の電子素子と機能を小さな半導体チップに集積した部品。
      | 用語7　　　　　　　 ; SPI：Serial Peripheral Interface（同期式シリアル通信）。クロックとデータ線を使う通信方式。本回路ではRP2040と外付け測定用ADCの通信に使う。
      | 用語8　　　　　　　 ; GND：Ground（回路の基準電位・電流帰路）。この図の共通基準。保護接地や大地への接続を意味するとは限らない。
      settings: AttributesFormatString=|
      | MLCC
      | 100 nF
  C18 : fl_lib/Electrical/Electrical Elements/Capacitor  Description=|  c=2.2e-06 F  r=1e-6 Ohm  g=0 1/Ohm  i_specify=off  i_priority=None  i=0 A  i_nominal_specify=off  i_nominal_value=1  i_nominal_unit=A  v_specify=off  v_priority=None  v=0 V  v_nominal_specify=off  v_nominal_value=1  v_nominal_unit=V  vc_specify=off  vc_priority=High  vc=0 V  vc_nominal_specify=off  vc_nominal_value=1  vc_nominal_unit=V
      | この回路での名前　　; C18
      | 部品名　　　　　　　; C3225X7R2A225K230AB
      | この回路での役割　　; 3.3 Vで動く計測回路の近くに電荷を蓄え、計測回路全体の消費電流の変化を支えるためのコンデンサ。
      | ここでの動き　　　　; 計測回路へ給電する3V3と共通GNDの間に2.2 µFを置き、電流が一時的に増えたときに電荷を補う。各ICの直近にあるC17などの100 nFとは、蓄える量と配置先を分担する。
      | 
      | 【詳しい働き・仕様・接続・確認の範囲】
      | 部品種別　　　　　　; 積層セラミックコンデンサ（MLCC）
      | 部品分類　　　　　　; 積層セラミックコンデンサ（MLCC）
      | 公称値　　　　　　　; 2.2 uF
      | 配置目的　　　　　　; 3V3測定群の局所バルク。対象ICはU1（MCP3208-CI/SL）。
      | 意図する動作　　　　; ADC/計測群の3V3給電枝。旧名称LDO_OUTは機能確認なしに維持理由としない。 Pico3V3からの配線長と過渡が未確定。旧LDO出力由来だが計測群バルクとして残し、重複候補は保留。
      | 端子と接続　　　　　; 1 1 → 3V3、2 2 → GND
      | モデルの範囲　　　　; Simscape標準コンデンサの集中定数表現。材質、DCバイアス、周波数依存ESR/ESL、寿命・温度特性を型番から自動再現するモデルではない。
      | モデル設定　　　　　; c=2.2 µF、r=1 µΩ、g=0 S。これらは保存モデルの設定値であり、すべてが実部品の保証値という意味ではない。
      | 損失の扱い　　　　　; 保存モデルの直列抵抗rと実部品の周波数・温度依存ESRは区別する。容量値が一致しても損失・リプル電流・寿命の成立確認にはならない。
      | 確認の範囲　　　　　; 本説明は保存回路の部品情報・端子割当・既存設計意図を整理したもの。今回の説明更新によって新たな動作試験や実機検証を実施した意味ではない。
      | 設計記録　　　　　　; evaluation\component_annotations_20261022_r01\before_graph.json
      | evaluation\component_annotations_20261022_r01\before_metadata.json
      | evaluation\protection_capacitor_integration_20261021_r01\final_delivery\independent_readback\physical_bom.json
      | evaluation\protection_capacitor_integration_20261021_r01\capacitor_review\capacitor_inventory_after_c04.json
      | evaluation\layout_readability_20261022_r01\capacitor_review\exact_snapshot_capacitor_review.json
      | 
      | 【周波数・ノイズと配置の説明】
      | 周波数面の役割　　　; 3.3 V計測回路へまとまった電荷を供給する局所バルク。
      | 対象周波数の目安　　; 計測群の動作開始や複数ICの消費電流変化に伴う比較的低い周波数側の変動を、100 nF局所バイパス群と分担する。実効帯域の数値は未確定。
      | ノイズの発生源　　　; ADCや計測ICの消費電流変化、Pico側から計測群へ至る給電配線の電圧降下。
      | 他のコンデンサとの差; 本品はMLCCでも蓄積側の役割を持つ。C17等の100 nFを各IC直近へ置く理由とは異なり、MLCCをすべて高速ノイズ専用とは扱わない。
      | 周波数説明の範囲　　; 狙うノイズの周波数と、この部品が実装後に有効な周波数範囲は別である。実効容量、等価直列抵抗、等価直列インダクタンス、配線を含む自己共振で変わるため、型番名や公称容量だけから有効帯域の上限を断定しない。
      | 周波数説明の根拠　　; TDK：Low-ESL Multilayer Ceramic Capacitors
      | https://product.tdk.com/system/files/dam/doc/content/emc-guidebook/en/eemc_product_01.pdf
      | 村田製作所：コンデンサを使いこなす
      | https://www.murata.com/en-GB/products/emc/emifil/library/knowhow/basic/chapter06-p8
      | 
      | 【この説明欄の略語・記号】
      | 用語1　　　　　　　 ; MLCC：Multilayer Ceramic Capacitor（積層セラミックコンデンサ）。薄いセラミック誘電体と電極を重ねたコンデンサ。対象周波数は容量・実装・寄生成分で変わるため、MLCCという分類だけでは決めない。
      | 用語2　　　　　　　 ; ESR：Equivalent Series Resistance（等価直列抵抗）。コンデンサの損失を直列抵抗で表した量。周波数・温度で変わり、損失とリプル電圧に関係する。
      | 用語3　　　　　　　 ; ESL：Equivalent Series Inductance（等価直列インダクタンス）。端子や電極などの寄生インダクタンスを表す。高い周波数ではバイパス効果を制限する。
      | 用語4　　　　　　　 ; DC：Direct Current（直流）。ここでは直流電源または直流成分。DCバイアスはコンデンサに重なる直流電圧を指す。
      | 用語5　　　　　　　 ; ADC：Analog-to-Digital Converter（アナログ・デジタル変換器）。測定電圧をデジタル値へ変換する回路。電流や温度も、センサーで電圧へ変換した後に読み取る。
      | 用語6　　　　　　　 ; IC：Integrated Circuit（集積回路）。複数の電子素子と機能を小さな半導体チップに集積した部品。
      | 用語7　　　　　　　 ; LDO：Low-Dropout Regulator（低ドロップアウトのリニア電圧調整器）。入力と出力の電圧差が小さい条件でも動作できる電圧調整器。LDO_OUTはその出力を表す設計上の名前。
      | 用語8　　　　　　　 ; GND：Ground（回路の基準電位・電流帰路）。この図の共通基準。保護接地や大地への接続を意味するとは限らない。
      settings: AttributesFormatString=|
      | MLCC
      | 2.2 µF
  C19 : fl_lib/Electrical/Electrical Elements/Capacitor  Description=|  c=1e-07 F  r=1e-6 Ohm  g=0 1/Ohm  i_specify=off  i_priority=None  i=0 A  i_nominal_specify=off  i_nominal_value=1  i_nominal_unit=A  v_specify=off  v_priority=None  v=0 V  v_nominal_specify=off  v_nominal_value=1  v_nominal_unit=V  vc_specify=off  vc_priority=High  vc=0 V  vc_nominal_specify=off  vc_nominal_value=1  vc_nominal_unit=V
      | この回路での名前　　; C19
      | 部品名　　　　　　　; CC0603KRX7R9BB104
      | この回路での役割　　; 太陽光パネル側の入力電圧を測る信号の速い揺れを抑え、U1が読み取りやすくするためのコンデンサ。
      | ここでの動き　　　　; 分圧抵抗R16〜R18で下げた測定電圧を、U1のCH0へ入れる直前のADC_VPVと共通GNDの間で受ける。抵抗と組み合わせて速い変化を弱め、読み取り時の電荷を補う一方、測定値の変化には遅れが加わる。
      | 
      | 【詳しい働き・仕様・接続・確認の範囲】
      | 部品種別　　　　　　; 積層セラミックコンデンサ（MLCC）
      | 部品分類　　　　　　; 積層セラミックコンデンサ（MLCC）
      | 公称値　　　　　　　; 100 nF
      | 配置目的　　　　　　; 電圧分圧RC/ADC取得電荷。対象はR16/R17/R18→U1CH0。
      | 意図する動作　　　　; ADC入力近傍、分圧下側の静かなGNDへ帰還。 分圧Thevenin約3.229kΩとの100nFでτ≈323µs。削除はノイズ/取得と制御遅延を変える。維持して時定数を計測条件へ渡す。
      | 端子と接続　　　　　; 1 1 → ADC_VPV、2 2 → GND
      | モデルの範囲　　　　; Simscape標準コンデンサの集中定数表現。材質、DCバイアス、周波数依存ESR/ESL、寿命・温度特性を型番から自動再現するモデルではない。
      | モデル設定　　　　　; c=100 nF、r=1 µΩ、g=0 S。これらは保存モデルの設定値であり、すべてが実部品の保証値という意味ではない。
      | 損失の扱い　　　　　; 保存モデルの直列抵抗rと実部品の周波数・温度依存ESRは区別する。容量値が一致しても損失・リプル電流・寿命の成立確認にはならない。
      | 確認の範囲　　　　　; 本説明は保存回路の部品情報・端子割当・既存設計意図を整理したもの。今回の説明更新によって新たな動作試験や実機検証を実施した意味ではない。
      | 設計記録　　　　　　; evaluation\component_annotations_20261022_r01\before_graph.json
      | evaluation\component_annotations_20261022_r01\before_metadata.json
      | evaluation\protection_capacitor_integration_20261021_r01\final_delivery\independent_readback\physical_bom.json
      | evaluation\protection_capacitor_integration_20261021_r01\capacitor_review\capacitor_inventory_after_c04.json
      | 
      | 【周波数・ノイズと配置の説明】
      | 周波数面の役割　　　; パネル側入力電圧を測る分圧回路の低域通過フィルタと、ADCの取得時に必要な局所電荷の保持。
      | 対象周波数の目安　　; 公称値で(75 kΩ+75 kΩ)と3.3 kΩの並列合成抵抗は約3.229 kΩ。100 nFとの理想1次RC遮断周波数は約493 Hz、時定数は約323 µs。遮断周波数以上を徐々に弱める特性で、その周波数を超えると急にゼロになるものではない。
      | ノイズの発生源　　　; 電力段のリプルが分圧器へ入り、測定配線へスイッチングの突起や通信信号が結合する。ADCがCH0の入力電荷を取り込む際にも瞬間的な電流が流れる。
      | 他のコンデンサとの差; 同じ100 nFでも電源バイパスC17等とは役割が異なる。ここでは抵抗と組み合わせて測定値の変化を平滑化し、応答にも遅れを加える。
      | 周波数説明の範囲　　; この周波数は公称抵抗・公称容量、理想信号源、高入力インピーダンスを仮定した回路計算。ADCの取得スイッチ、実効容量、信号源インピーダンスを含む総整定時間やサンプリング適合の検証結果ではない。
      | 周波数説明の根拠　　; TI Precision Labs：Passive Components and Circuits
      | https://www.ti.com/content/dam/videos/external-videos/en-us/4/3816841626001/6119035031001.mp4/subassets/passive_components_and_circuits_2.pdf
      | Microchip：MCP3204/3208 datasheet
      | https://ww1.microchip.com/downloads/en/DeviceDoc/21298E.pdf
      | 
      | 【この説明欄の略語・記号】
      | 用語1　　　　　　　 ; MLCC：Multilayer Ceramic Capacitor（積層セラミックコンデンサ）。薄いセラミック誘電体と電極を重ねたコンデンサ。対象周波数は容量・実装・寄生成分で変わるため、MLCCという分類だけでは決めない。
      | 用語2　　　　　　　 ; ESR：Equivalent Series Resistance（等価直列抵抗）。コンデンサの損失を直列抵抗で表した量。周波数・温度で変わり、損失とリプル電圧に関係する。
      | 用語3　　　　　　　 ; ESL：Equivalent Series Inductance（等価直列インダクタンス）。端子や電極などの寄生インダクタンスを表す。高い周波数ではバイパス効果を制限する。
      | 用語4　　　　　　　 ; DC：Direct Current（直流）。ここでは直流電源または直流成分。DCバイアスはコンデンサに重なる直流電圧を指す。
      | 用語5　　　　　　　 ; ADC：Analog-to-Digital Converter（アナログ・デジタル変換器）。測定電圧をデジタル値へ変換する回路。電流や温度も、センサーで電圧へ変換した後に読み取る。
      | 用語6　　　　　　　 ; CH：Channel（測定チャネル）。CH0〜CH7はADCの入力番号であり、同時測定を意味しない。
      | 用語7　　　　　　　 ; RC：Resistor-Capacitor（抵抗とコンデンサの組合せ）。主に測定信号のフィルタや時定数を作る。カットオフ周波数は実際の接続と抵抗・容量から求める。
      | 用語8　　　　　　　 ; τ：Time Constant（時定数）。1次RC回路では抵抗Rと容量Cの積で、単位は秒。入力が急変した後の応答の速さを表す。τだけ経過すると最終変化量の約63%まで変化する。
      | 用語9　　　　　　　 ; GND：Ground（回路の基準電位・電流帰路）。この図の共通基準。保護接地や大地への接続を意味するとは限らない。
      settings: AttributesFormatString=|
      | MLCC
      | 100 nF
  C2 : fl_lib/Electrical/Electrical Elements/Capacitor  Description=|  c=0.00046999999999999999 F  r=1e-6 Ohm  g=0 1/Ohm  i_specify=off  i_priority=None  i=0 A  i_nominal_specify=off  i_nominal_value=1  i_nominal_unit=A  v_specify=off  v_priority=None  v=0 V  v_nominal_specify=off  v_nominal_value=1  v_nominal_unit=V  vc_specify=off  vc_priority=High  vc=0 V  vc_nominal_specify=off  vc_nominal_value=1  vc_nominal_unit=V
      | この回路での名前　　; C2
      | 部品名　　　　　　　; UCY2C471MHD
      | この回路での役割　　; 太陽光パネルから給電される主電力段の入力側に電荷を蓄え、入力電圧の落ち込みや変動を抑えるためのコンデンサ。
      | ここでの動き　　　　; 入力電源VINと共通GNDの間に470 µFを3個並列に置き、降圧回路が電流を必要とするときに電荷を補う。速い変化への対応は、近くのC7〜C10と分担する設計。
      | 
      | 【詳しい働き・仕様・接続・確認の範囲】
      | 部品種別　　　　　　; アルミ電解コンデンサ（有極性）
      | 部品分類　　　　　　; アルミ電解コンデンサ（有極性）
      | 公称値　　　　　　　; 470 uF
      | 配置目的　　　　　　; 入力バルク。対象はL2入力フィルタとQ1/Q2電力段。
      | 意図する動作　　　　; VIN–GND間の入力バルクとして、降圧電力段が必要とする電荷を供給し入力電圧変動を抑える。現構成は470 µFを3個。分流・ESR・温度上昇・配線寄生の適合は別評価。
      | 端子と接続　　　　　; 2 n → GND、1 p → VIN
      | モデルの範囲　　　　; Simscape標準コンデンサの集中定数表現。材質、DCバイアス、周波数依存ESR/ESL、寿命・温度特性を型番から自動再現するモデルではない。
      | モデル設定　　　　　; c=470 µF、r=1 µΩ、g=0 S。これらは保存モデルの設定値であり、すべてが実部品の保証値という意味ではない。
      | 損失の扱い　　　　　; 保存モデルの直列抵抗rと実部品の周波数・温度依存ESRは区別する。容量値が一致しても損失・リプル電流・寿命の成立確認にはならない。
      | 確認の範囲　　　　　; 本説明は保存回路の部品情報・端子割当・既存設計意図を整理したもの。今回の説明更新によって新たな動作試験や実機検証を実施した意味ではない。
      | 設計記録　　　　　　; evaluation\component_annotations_20261022_r01\before_graph.json
      | evaluation\component_annotations_20261022_r01\before_metadata.json
      | evaluation\protection_capacitor_integration_20261021_r01\final_delivery\independent_readback\physical_bom.json
      | evaluation\protection_capacitor_integration_20261021_r01\capacitor_review\capacitor_inventory_after_c04.json
      | 
      | 【周波数・ノイズと配置の説明】
      | 周波数面の役割　　　; 入力電圧の比較的ゆっくりした変動を抑え、主電力段が必要な電荷を蓄える。
      | 対象周波数の目安　　; 起動・日射/負荷変動などの低い周波数側から、主スイッチング周期の電荷出入りまでを受け持つ。主電力段の既存比較計算では50 kHzを仮定している。これは比較シナリオの値であり、今回の保存図から実行中PWM周波数を測定した値ではない。
      | ノイズの発生源　　　; Q1のオン期間に入力から電流を取り出すため、入力電流は脈動する。パネル/配線/L2側がすぐ補えない電流をこの容量群が補う。
      | 他のコンデンサとの差; 470 µF×3個の電解は蓄積量を担当する。C7のフィルムとC8～C10のMLCCは速い電流変化への局所経路を補う。同じ周波数で複数群が分担し、境界周波数で役割が切り替わるわけではない。
      | 周波数説明の範囲　　; 狙うノイズの周波数と、この部品が実装後に有効な周波数範囲は別である。実効容量、等価直列抵抗、等価直列インダクタンス、配線を含む自己共振で変わるため、型番名や公称容量だけから有効帯域の上限を断定しない。
      | 周波数説明の根拠　　; 村田製作所：コンデンサのインピーダンス・ESRと周波数の関係
      | https://article.murata.com/en-global/article/impedance-esr-frequency-characteristics-in-capacitors
      | 村田製作所：コンデンサを使いこなす
      | https://www.murata.com/en-GB/products/emc/emifil/library/knowhow/basic/chapter06-p8
      | 
      | 【この説明欄の略語・記号】
      | 用語1　　　　　　　 ; MLCC：Multilayer Ceramic Capacitor（積層セラミックコンデンサ）。薄いセラミック誘電体と電極を重ねたコンデンサ。対象周波数は容量・実装・寄生成分で変わるため、MLCCという分類だけでは決めない。
      | 用語2　　　　　　　 ; ESR：Equivalent Series Resistance（等価直列抵抗）。コンデンサの損失を直列抵抗で表した量。周波数・温度で変わり、損失とリプル電圧に関係する。
      | 用語3　　　　　　　 ; ESL：Equivalent Series Inductance（等価直列インダクタンス）。端子や電極などの寄生インダクタンスを表す。高い周波数ではバイパス効果を制限する。
      | 用語4　　　　　　　 ; DC：Direct Current（直流）。ここでは直流電源または直流成分。DCバイアスはコンデンサに重なる直流電圧を指す。
      | 用語5　　　　　　　 ; PWM：Pulse Width Modulation（パルス幅変調）。周期に対するON時間の割合を変えて、スイッチの平均的な電力伝達を調整する方式。
      | 用語6　　　　　　　 ; GND：Ground（回路の基準電位・電流帰路）。この図の共通基準。保護接地や大地への接続を意味するとは限らない。
      | 用語7　　　　　　　 ; VIN/VOUT：入力電圧・出力電圧を表す端子／ネット名。INは入力、OUTは出力。電源変換器の電力端子なのか、検出用端子なのかは対象部品によって異なるため、端子と接続の説明に従う。
      settings: AttributesFormatString=|
      | 電解
      | 470 µF
  C20 : fl_lib/Electrical/Electrical Elements/Capacitor  Description=|  c=1e-07 F  r=1e-6 Ohm  g=0 1/Ohm  i_specify=off  i_priority=None  i=0 A  i_nominal_specify=off  i_nominal_value=1  i_nominal_unit=A  v_specify=off  v_priority=None  v=0 V  v_nominal_specify=off  v_nominal_value=1  v_nominal_unit=V  vc_specify=off  vc_priority=High  vc=0 V  vc_nominal_specify=off  vc_nominal_value=1  vc_nominal_unit=V
      | この回路での名前　　; C20
      | 部品名　　　　　　　; CC0603KRX7R9BB104
      | この回路での役割　　; 保護回路に入る前の出力電圧を測る信号の速い揺れを抑え、U1が読み取りやすくするためのコンデンサ。
      | ここでの動き　　　　; 分圧抵抗R19〜R21で下げた測定電圧を、U1のCH2へ入れる直前のADC_VOUTと共通GNDの間で受ける。抵抗と組み合わせて速い変化を弱め、読み取り時の電荷を補う一方、測定値の変化には遅れが加わる。
      | 
      | 【詳しい働き・仕様・接続・確認の範囲】
      | 部品種別　　　　　　; 積層セラミックコンデンサ（MLCC）
      | 部品分類　　　　　　; 積層セラミックコンデンサ（MLCC）
      | 公称値　　　　　　　; 100 nF
      | 配置目的　　　　　　; 電圧分圧RC/ADC取得電荷。対象はR19/R20/R21→U1CH2。
      | 意図する動作　　　　; ADC入力近傍、分圧下側の静かなGNDへ帰還。 分圧Thevenin約3.229kΩとの100nFでτ≈323µs。削除はノイズ/取得と制御遅延を変える。維持して時定数を計測条件へ渡す。
      | 端子と接続　　　　　; 1 1 → ADC_VOUT、2 2 → GND
      | モデルの範囲　　　　; Simscape標準コンデンサの集中定数表現。材質、DCバイアス、周波数依存ESR/ESL、寿命・温度特性を型番から自動再現するモデルではない。
      | モデル設定　　　　　; c=100 nF、r=1 µΩ、g=0 S。これらは保存モデルの設定値であり、すべてが実部品の保証値という意味ではない。
      | 損失の扱い　　　　　; 保存モデルの直列抵抗rと実部品の周波数・温度依存ESRは区別する。容量値が一致しても損失・リプル電流・寿命の成立確認にはならない。
      | 確認の範囲　　　　　; 本説明は保存回路の部品情報・端子割当・既存設計意図を整理したもの。今回の説明更新によって新たな動作試験や実機検証を実施した意味ではない。
      | 設計記録　　　　　　; evaluation\component_annotations_20261022_r01\before_graph.json
      | evaluation\component_annotations_20261022_r01\before_metadata.json
      | evaluation\protection_capacitor_integration_20261021_r01\final_delivery\independent_readback\physical_bom.json
      | evaluation\protection_capacitor_integration_20261021_r01\capacitor_review\capacitor_inventory_after_c04.json
      | 
      | 【周波数・ノイズと配置の説明】
      | 周波数面の役割　　　; 保護前の出力電圧を測る分圧回路の低域通過フィルタと、ADCの取得時に必要な局所電荷の保持。
      | 対象周波数の目安　　; 公称値で(75 kΩ+75 kΩ)と3.3 kΩの並列合成抵抗は約3.229 kΩ。100 nFとの理想1次RC遮断周波数は約493 Hz、時定数は約323 µs。遮断周波数以上を徐々に弱める特性で、その周波数を超えると急にゼロになるものではない。
      | ノイズの発生源　　　; 電力段のリプルが分圧器へ入り、測定配線へスイッチングの突起や通信信号が結合する。ADCがCH2の入力電荷を取り込む際にも瞬間的な電流が流れる。
      | 他のコンデンサとの差; 同じ100 nFでも電源バイパスC17等とは役割が異なる。ここでは抵抗と組み合わせて測定値の変化を平滑化し、応答にも遅れを加える。
      | 周波数説明の範囲　　; この周波数は公称抵抗・公称容量、理想信号源、高入力インピーダンスを仮定した回路計算。ADCの取得スイッチ、実効容量、信号源インピーダンスを含む総整定時間やサンプリング適合の検証結果ではない。
      | 周波数説明の根拠　　; TI Precision Labs：Passive Components and Circuits
      | https://www.ti.com/content/dam/videos/external-videos/en-us/4/3816841626001/6119035031001.mp4/subassets/passive_components_and_circuits_2.pdf
      | Microchip：MCP3204/3208 datasheet
      | https://ww1.microchip.com/downloads/en/DeviceDoc/21298E.pdf
      | 
      | 【この説明欄の略語・記号】
      | 用語1　　　　　　　 ; MLCC：Multilayer Ceramic Capacitor（積層セラミックコンデンサ）。薄いセラミック誘電体と電極を重ねたコンデンサ。対象周波数は容量・実装・寄生成分で変わるため、MLCCという分類だけでは決めない。
      | 用語2　　　　　　　 ; ESR：Equivalent Series Resistance（等価直列抵抗）。コンデンサの損失を直列抵抗で表した量。周波数・温度で変わり、損失とリプル電圧に関係する。
      | 用語3　　　　　　　 ; ESL：Equivalent Series Inductance（等価直列インダクタンス）。端子や電極などの寄生インダクタンスを表す。高い周波数ではバイパス効果を制限する。
      | 用語4　　　　　　　 ; DC：Direct Current（直流）。ここでは直流電源または直流成分。DCバイアスはコンデンサに重なる直流電圧を指す。
      | 用語5　　　　　　　 ; ADC：Analog-to-Digital Converter（アナログ・デジタル変換器）。測定電圧をデジタル値へ変換する回路。電流や温度も、センサーで電圧へ変換した後に読み取る。
      | 用語6　　　　　　　 ; CH：Channel（測定チャネル）。CH0〜CH7はADCの入力番号であり、同時測定を意味しない。
      | 用語7　　　　　　　 ; RC：Resistor-Capacitor（抵抗とコンデンサの組合せ）。主に測定信号のフィルタや時定数を作る。カットオフ周波数は実際の接続と抵抗・容量から求める。
      | 用語8　　　　　　　 ; τ：Time Constant（時定数）。1次RC回路では抵抗Rと容量Cの積で、単位は秒。入力が急変した後の応答の速さを表す。τだけ経過すると最終変化量の約63%まで変化する。
      | 用語9　　　　　　　 ; GND：Ground（回路の基準電位・電流帰路）。この図の共通基準。保護接地や大地への接続を意味するとは限らない。
      | 用語10　　　　　　　; VIN/VOUT：入力電圧・出力電圧を表す端子／ネット名。INは入力、OUTは出力。電源変換器の電力端子なのか、検出用端子なのかは対象部品によって異なるため、端子と接続の説明に従う。
      settings: AttributesFormatString=|
      | MLCC
      | 100 nF
  C21 : fl_lib/Electrical/Electrical Elements/Capacitor  Description=|  c=1e-07 F  r=1e-6 Ohm  g=0 1/Ohm  i_specify=off  i_priority=None  i=0 A  i_nominal_specify=off  i_nominal_value=1  i_nominal_unit=A  v_specify=off  v_priority=None  v=0 V  v_nominal_specify=off  v_nominal_value=1  v_nominal_unit=V  vc_specify=off  vc_priority=High  vc=0 V  vc_nominal_specify=off  vc_nominal_value=1  vc_nominal_unit=V
      | この回路での名前　　; C21
      | 部品名　　　　　　　; CC0603KRX7R9BB104
      | この回路での役割　　; バッテリー電圧を測る信号の速い揺れを抑え、U1が読み取りやすくするためのコンデンサ。
      | ここでの動き　　　　; 分圧抵抗R22〜R24で下げた測定電圧を、U1のCH6へ入れる直前のADC_VBATと共通GNDの間で受ける。抵抗と組み合わせて速い変化を弱め、読み取り時の電荷を補う一方、測定値の変化には遅れが加わる。
      | 
      | 【詳しい働き・仕様・接続・確認の範囲】
      | 部品種別　　　　　　; 積層セラミックコンデンサ（MLCC）
      | 部品分類　　　　　　; 積層セラミックコンデンサ（MLCC）
      | 公称値　　　　　　　; 100 nF
      | 配置目的　　　　　　; 電圧分圧RC/ADC取得電荷。対象はR22/R23/R24→U1CH6。
      | 意図する動作　　　　; ADC入力近傍、分圧下側の静かなGNDへ帰還。 分圧Thevenin約3.229kΩとの100nFでτ≈323µs。削除はノイズ/取得と制御遅延を変える。維持して時定数を計測条件へ渡す。
      | 端子と接続　　　　　; 1 1 → ADC_VBAT、2 2 → GND
      | モデルの範囲　　　　; Simscape標準コンデンサの集中定数表現。材質、DCバイアス、周波数依存ESR/ESL、寿命・温度特性を型番から自動再現するモデルではない。
      | モデル設定　　　　　; c=100 nF、r=1 µΩ、g=0 S。これらは保存モデルの設定値であり、すべてが実部品の保証値という意味ではない。
      | 損失の扱い　　　　　; 保存モデルの直列抵抗rと実部品の周波数・温度依存ESRは区別する。容量値が一致しても損失・リプル電流・寿命の成立確認にはならない。
      | 確認の範囲　　　　　; 本説明は保存回路の部品情報・端子割当・既存設計意図を整理したもの。今回の説明更新によって新たな動作試験や実機検証を実施した意味ではない。
      | 設計記録　　　　　　; evaluation\component_annotations_20261022_r01\before_graph.json
      | evaluation\component_annotations_20261022_r01\before_metadata.json
      | evaluation\protection_capacitor_integration_20261021_r01\final_delivery\independent_readback\physical_bom.json
      | evaluation\protection_capacitor_integration_20261021_r01\capacitor_review\capacitor_inventory_after_c04.json
      | 
      | 【周波数・ノイズと配置の説明】
      | 周波数面の役割　　　; バッテリー電圧を測る分圧回路の低域通過フィルタと、ADCの取得時に必要な局所電荷の保持。
      | 対象周波数の目安　　; 公称値で(75 kΩ+75 kΩ)と3.3 kΩの並列合成抵抗は約3.229 kΩ。100 nFとの理想1次RC遮断周波数は約493 Hz、時定数は約323 µs。遮断周波数以上を徐々に弱める特性で、その周波数を超えると急にゼロになるものではない。
      | ノイズの発生源　　　; 電力段のリプルが分圧器へ入り、測定配線へスイッチングの突起や通信信号が結合する。ADCがCH6の入力電荷を取り込む際にも瞬間的な電流が流れる。
      | 他のコンデンサとの差; 同じ100 nFでも電源バイパスC17等とは役割が異なる。ここでは抵抗と組み合わせて測定値の変化を平滑化し、応答にも遅れを加える。
      | 周波数説明の範囲　　; この周波数は公称抵抗・公称容量、理想信号源、高入力インピーダンスを仮定した回路計算。ADCの取得スイッチ、実効容量、信号源インピーダンスを含む総整定時間やサンプリング適合の検証結果ではない。
      | 周波数説明の根拠　　; TI Precision Labs：Passive Components and Circuits
      | https://www.ti.com/content/dam/videos/external-videos/en-us/4/3816841626001/6119035031001.mp4/subassets/passive_components_and_circuits_2.pdf
      | Microchip：MCP3204/3208 datasheet
      | https://ww1.microchip.com/downloads/en/DeviceDoc/21298E.pdf
      | 
      | 【この説明欄の略語・記号】
      | 用語1　　　　　　　 ; MLCC：Multilayer Ceramic Capacitor（積層セラミックコンデンサ）。薄いセラミック誘電体と電極を重ねたコンデンサ。対象周波数は容量・実装・寄生成分で変わるため、MLCCという分類だけでは決めない。
      | 用語2　　　　　　　 ; ESR：Equivalent Series Resistance（等価直列抵抗）。コンデンサの損失を直列抵抗で表した量。周波数・温度で変わり、損失とリプル電圧に関係する。
      | 用語3　　　　　　　 ; ESL：Equivalent Series Inductance（等価直列インダクタンス）。端子や電極などの寄生インダクタンスを表す。高い周波数ではバイパス効果を制限する。
      | 用語4　　　　　　　 ; DC：Direct Current（直流）。ここでは直流電源または直流成分。DCバイアスはコンデンサに重なる直流電圧を指す。
      | 用語5　　　　　　　 ; ADC：Analog-to-Digital Converter（アナログ・デジタル変換器）。測定電圧をデジタル値へ変換する回路。電流や温度も、センサーで電圧へ変換した後に読み取る。
      | 用語6　　　　　　　 ; CH：Channel（測定チャネル）。CH0〜CH7はADCの入力番号であり、同時測定を意味しない。
      | 用語7　　　　　　　 ; RC：Resistor-Capacitor（抵抗とコンデンサの組合せ）。主に測定信号のフィルタや時定数を作る。カットオフ周波数は実際の接続と抵抗・容量から求める。
      | 用語8　　　　　　　 ; τ：Time Constant（時定数）。1次RC回路では抵抗Rと容量Cの積で、単位は秒。入力が急変した後の応答の速さを表す。τだけ経過すると最終変化量の約63%まで変化する。
      | 用語9　　　　　　　 ; GND：Ground（回路の基準電位・電流帰路）。この図の共通基準。保護接地や大地への接続を意味するとは限らない。
      settings: AttributesFormatString=|
      | MLCC
      | 100 nF
  C23 : fl_lib/Electrical/Electrical Elements/Capacitor  Description=|  c=1e-07 F  r=1e-6 Ohm  g=0 1/Ohm  i_specify=off  i_priority=None  i=0 A  i_nominal_specify=off  i_nominal_value=1  i_nominal_unit=A  v_specify=off  v_priority=None  v=0 V  v_nominal_specify=off  v_nominal_value=1  v_nominal_unit=V  vc_specify=off  vc_priority=High  vc=0 V  vc_nominal_specify=off  vc_nominal_value=1  vc_nominal_unit=V
      | この回路での名前　　; C23
      | 部品名　　　　　　　; CC0603KRX7R9BB104
      | この回路での役割　　; パネル電流の測定信号から速い電気的な揺れを減らし、U1が読み取りやすくするためのコンデンサ。
      | ここでの動き　　　　; 電流検出ICの出力を抵抗R25に通し、その先のADC_IPVと共通GNDの間に100 nFを置いてU1のCH1へ渡す。信号をならすため、容量を変えると測定とソフトウェア保護の応答速度にも影響する。
      | 
      | 【詳しい働き・仕様・接続・確認の範囲】
      | 部品種別　　　　　　; 積層セラミックコンデンサ（MLCC）
      | 部品分類　　　　　　; 積層セラミックコンデンサ（MLCC）
      | 公称値　　　　　　　; 100 nF
      | 配置目的　　　　　　; 電流信号RC/ADC取得電荷。対象はR25100ΩとU1CH1。
      | 意図する動作　　　　; ADC入力側のRC帰路、INA出力から100Ωで分離。 τ10µs/fc15.9kHz。電流変化をソフト停止へ使う時間応答に影響するため維持。
      | 端子と接続　　　　　; 1 1 → ADC_IPV、2 2 → GND
      | モデルの範囲　　　　; Simscape標準コンデンサの集中定数表現。材質、DCバイアス、周波数依存ESR/ESL、寿命・温度特性を型番から自動再現するモデルではない。
      | モデル設定　　　　　; c=100 nF、r=1 µΩ、g=0 S。これらは保存モデルの設定値であり、すべてが実部品の保証値という意味ではない。
      | 損失の扱い　　　　　; 保存モデルの直列抵抗rと実部品の周波数・温度依存ESRは区別する。容量値が一致しても損失・リプル電流・寿命の成立確認にはならない。
      | 確認の範囲　　　　　; 本説明は保存回路の部品情報・端子割当・既存設計意図を整理したもの。今回の説明更新によって新たな動作試験や実機検証を実施した意味ではない。
      | 設計記録　　　　　　; evaluation\component_annotations_20261022_r01\before_graph.json
      | evaluation\component_annotations_20261022_r01\before_metadata.json
      | evaluation\protection_capacitor_integration_20261021_r01\final_delivery\independent_readback\physical_bom.json
      | evaluation\protection_capacitor_integration_20261021_r01\capacitor_review\capacitor_inventory_after_c04.json
      | 
      | 【周波数・ノイズと配置の説明】
      | 周波数面の役割　　　; 電流検出ICの出力をR25の100 Ωで分離し、ADC入力側で高周波成分を弱めて取得用電荷を保持する。
      | 対象周波数の目安　　; 100 Ωと100 nFの理想1次RC遮断周波数は約15.9 kHz、時定数は10 µs。これより高い周波数の成分を徐々に弱める。
      | ノイズの発生源　　　; シャントで検出する電流リプル、電力段から検出系へ結合する切替えノイズ、ADCのCH1入力取得時の電荷移動。
      | 他のコンデンサとの差; 電流検出ICの電源用100 nF（C22/C24）は電源を支える。本品は信号に作用するため、容量を変えると測定速度やソフト保護の応答も変わる。
      | 周波数説明の範囲　　; 15.9 kHzは100 Ωと100 nFだけの理想計算。電流検出ICの出力インピーダンス・帯域、ADCの取得条件を含む実際の応答や折り返し雑音の抑制を保証しない。
      | 周波数説明の根拠　　; TI Precision Labs：Passive Components and Circuits
      | https://www.ti.com/content/dam/videos/external-videos/en-us/4/3816841626001/6119035031001.mp4/subassets/passive_components_and_circuits_2.pdf
      | Microchip：MCP3204/3208 datasheet
      | https://ww1.microchip.com/downloads/en/DeviceDoc/21298E.pdf
      | 
      | 【この説明欄の略語・記号】
      | 用語1　　　　　　　 ; MLCC：Multilayer Ceramic Capacitor（積層セラミックコンデンサ）。薄いセラミック誘電体と電極を重ねたコンデンサ。対象周波数は容量・実装・寄生成分で変わるため、MLCCという分類だけでは決めない。
      | 用語2　　　　　　　 ; ESR：Equivalent Series Resistance（等価直列抵抗）。コンデンサの損失を直列抵抗で表した量。周波数・温度で変わり、損失とリプル電圧に関係する。
      | 用語3　　　　　　　 ; ESL：Equivalent Series Inductance（等価直列インダクタンス）。端子や電極などの寄生インダクタンスを表す。高い周波数ではバイパス効果を制限する。
      | 用語4　　　　　　　 ; DC：Direct Current（直流）。ここでは直流電源または直流成分。DCバイアスはコンデンサに重なる直流電圧を指す。
      | 用語5　　　　　　　 ; ADC：Analog-to-Digital Converter（アナログ・デジタル変換器）。測定電圧をデジタル値へ変換する回路。電流や温度も、センサーで電圧へ変換した後に読み取る。
      | 用語6　　　　　　　 ; IC：Integrated Circuit（集積回路）。複数の電子素子と機能を小さな半導体チップに集積した部品。
      | 用語7　　　　　　　 ; CH：Channel（測定チャネル）。CH0〜CH7はADCの入力番号であり、同時測定を意味しない。
      | 用語8　　　　　　　 ; RC：Resistor-Capacitor（抵抗とコンデンサの組合せ）。主に測定信号のフィルタや時定数を作る。カットオフ周波数は実際の接続と抵抗・容量から求める。
      | 用語9　　　　　　　 ; INA：この説明ではTI製電流検出アンプU2/U3を指す型番系列の略記。INA241A3の先頭文字を使った呼び方。メーカーが定めた英語の正式展開を推測したものではない。
      | 用語10　　　　　　　; fc：Cutoff Frequency（遮断周波数）。フィルタの信号を通す側と弱める側を表す目安。ここでの理想1次RC回路では振幅が低周波側の約70.7%になる周波数で、これ以上が急にゼロになるわけではない。
      | 用語11　　　　　　　; τ：Time Constant（時定数）。1次RC回路では抵抗Rと容量Cの積で、単位は秒。入力が急変した後の応答の速さを表す。τだけ経過すると最終変化量の約63%まで変化する。
      | 用語12　　　　　　　; GND：Ground（回路の基準電位・電流帰路）。この図の共通基準。保護接地や大地への接続を意味するとは限らない。
      settings: AttributesFormatString=|
      | MLCC
      | 100 nF
  C24 : fl_lib/Electrical/Electrical Elements/Capacitor  Description=|  c=1e-07 F  r=1e-6 Ohm  g=0 1/Ohm  i_specify=off  i_priority=None  i=0 A  i_nominal_specify=off  i_nominal_value=1  i_nominal_unit=A  v_specify=off  v_priority=None  v=0 V  v_nominal_specify=off  v_nominal_value=1  v_nominal_unit=V  vc_specify=off  vc_priority=High  vc=0 V  vc_nominal_specify=off  vc_nominal_value=1  vc_nominal_unit=V
      | この回路での名前　　; C24
      | 部品名　　　　　　　; C1608X7R1H104K080AA
      | この回路での役割　　; インダクタL1を通った出力電流を測るU3の3.3 V電源を、瞬間的な変動から支えるためのコンデンサ。
      | ここでの動き　　　　; U3の電源端子と共通GNDの近くで一時的な電流を供給し、速い電流の帰り道を短くする。小さな電流検出信号の配線へ、電源電流の影響を持ち込みにくくする配置を意図する。
      | 
      | 【詳しい働き・仕様・接続・確認の範囲】
      | 部品種別　　　　　　; 積層セラミックコンデンサ（MLCC）
      | 部品分類　　　　　　; 積層セラミックコンデンサ（MLCC）
      | 公称値　　　　　　　; 100nF 50V
      | 配置目的　　　　　　; 電流検出IC電源バイパス。対象ICはU3（INA241A3IDDFR）。
      | 意図する動作　　　　; VS–GNDピン直近。シャントKelvin戻りと電源過渡電流を混ぜない。 各IC局所100nFは同じ3V3でも削減しない。
      | 端子と接続　　　　　; 1 1 → 3V3、2 2 → GND
      | モデルの範囲　　　　; Simscape標準コンデンサの集中定数表現。材質、DCバイアス、周波数依存ESR/ESL、寿命・温度特性を型番から自動再現するモデルではない。
      | モデル設定　　　　　; c=100 nF、r=1 µΩ、g=0 S。これらは保存モデルの設定値であり、すべてが実部品の保証値という意味ではない。
      | 損失の扱い　　　　　; 保存モデルの直列抵抗rと実部品の周波数・温度依存ESRは区別する。容量値が一致しても損失・リプル電流・寿命の成立確認にはならない。
      | 確認の範囲　　　　　; 本説明は保存回路の部品情報・端子割当・既存設計意図を整理したもの。今回の説明更新によって新たな動作試験や実機検証を実施した意味ではない。
      | 設計記録　　　　　　; evaluation\component_annotations_20261022_r01\before_graph.json
      | evaluation\component_annotations_20261022_r01\before_metadata.json
      | evaluation\protection_capacitor_integration_20261021_r01\final_delivery\independent_readback\physical_bom.json
      | evaluation\protection_capacitor_integration_20261021_r01\capacitor_review\capacitor_inventory_after_c04.json
      | evaluation\layout_readability_20261022_r01\capacitor_review\exact_snapshot_capacitor_review.json
      | 
      | 【周波数・ノイズと配置の説明】
      | 周波数面の役割　　　; U3（L1出力電流検出IC）の電源端子直近で、瞬間的な電流を供給する局所バイパス。
      | 対象周波数の目安　　; そのICの内部動作や周辺の通信、周囲のスイッチングによる高周波成分を対象にする。100 nFという容量だけから「何MHzまで効く」とは決められない。
      | ノイズの発生源　　　; IC内部の回路動作に伴う電源電流の変化、3.3 V配線を経由する電源変動、近傍のデジタル信号やゲート駆動からの結合。
      | 他のコンデンサとの差; 離れたC18や電源装置側の大きな容量は低い周波数側の蓄積を補う。配線の寄生インダクタンスがあるため、同じ電源ネットでもIC直近の本品を完全に代替できない。
      | 周波数説明の範囲　　; 狙うノイズの周波数と、この部品が実装後に有効な周波数範囲は別である。実効容量、等価直列抵抗、等価直列インダクタンス、配線を含む自己共振で変わるため、型番名や公称容量だけから有効帯域の上限を断定しない。
      | 周波数説明の根拠　　; TDK：Low-ESL Multilayer Ceramic Capacitors
      | https://product.tdk.com/system/files/dam/doc/content/emc-guidebook/en/eemc_product_01.pdf
      | 村田製作所：コンデンサを使いこなす
      | https://www.murata.com/en-GB/products/emc/emifil/library/knowhow/basic/chapter06-p8
      | 
      | 【この説明欄の略語・記号】
      | 用語1　　　　　　　 ; MLCC：Multilayer Ceramic Capacitor（積層セラミックコンデンサ）。薄いセラミック誘電体と電極を重ねたコンデンサ。対象周波数は容量・実装・寄生成分で変わるため、MLCCという分類だけでは決めない。
      | 用語2　　　　　　　 ; ESR：Equivalent Series Resistance（等価直列抵抗）。コンデンサの損失を直列抵抗で表した量。周波数・温度で変わり、損失とリプル電圧に関係する。
      | 用語3　　　　　　　 ; ESL：Equivalent Series Inductance（等価直列インダクタンス）。端子や電極などの寄生インダクタンスを表す。高い周波数ではバイパス効果を制限する。
      | 用語4　　　　　　　 ; DC：Direct Current（直流）。ここでは直流電源または直流成分。DCバイアスはコンデンサに重なる直流電圧を指す。
      | 用語5　　　　　　　 ; IC：Integrated Circuit（集積回路）。複数の電子素子と機能を小さな半導体チップに集積した部品。
      | 用語6　　　　　　　 ; MOSFET：Metal-Oxide-Semiconductor Field-Effect Transistor（金属・酸化膜・半導体構造の電界効果トランジスタ）。ゲートとソースの電圧でドレインとソースの導通を制御する素子。N-MOSはNチャネル型を表す。
      | 用語7　　　　　　　 ; GND：Ground（回路の基準電位・電流帰路）。この図の共通基準。保護接地や大地への接続を意味するとは限らない。
      | 用語8　　　　　　　 ; VCC/VDD/VEE/VS：ICの電源端子名。文字の歴史的な由来を現在の接続機能へ当てはめない。現回路のVEEはU8/U10では浮動基準SW、U9ではGND。各電圧・基準は端子と接続を参照する。
      | 用語9　　　　　　　 ; SW：Switching Node（スイッチング点）。主電力段の上下MOSFETとL1がつながる、電圧が高速に切り替わる点。GNDとは別電位。
      settings: AttributesFormatString=|
      | MLCC
      | 100 nF
  C25 : fl_lib/Electrical/Electrical Elements/Capacitor  Description=|  c=1e-07 F  r=1e-6 Ohm  g=0 1/Ohm  i_specify=off  i_priority=None  i=0 A  i_nominal_specify=off  i_nominal_value=1  i_nominal_unit=A  v_specify=off  v_priority=None  v=0 V  v_nominal_specify=off  v_nominal_value=1  v_nominal_unit=V  vc_specify=off  vc_priority=High  vc=0 V  vc_nominal_specify=off  vc_nominal_value=1  vc_nominal_unit=V
      | この回路での名前　　; C25
      | 部品名　　　　　　　; CC0603KRX7R9BB104
      | この回路での役割　　; インダクタL1を通る出力電流の測定信号から速い電気的な揺れを減らし、U1が読み取りやすくするためのコンデンサ。
      | ここでの動き　　　　; 電流検出ICの出力を抵抗R26に通し、その先のADC_ILと共通GNDの間に100 nFを置いてU1のCH3へ渡す。信号をならすため、容量を変えると測定とソフトウェア保護の応答速度にも影響する。
      | 
      | 【詳しい働き・仕様・接続・確認の範囲】
      | 部品種別　　　　　　; 積層セラミックコンデンサ（MLCC）
      | 部品分類　　　　　　; 積層セラミックコンデンサ（MLCC）
      | 公称値　　　　　　　; 100 nF
      | 配置目的　　　　　　; 電流信号RC/ADC取得電荷。対象はR26100ΩとU1CH3。
      | 意図する動作　　　　; ADC入力側のRC帰路、INA出力から100Ωで分離。 τ10µs/fc15.9kHz。電流変化をソフト停止へ使う時間応答に影響するため維持。
      | 端子と接続　　　　　; 1 1 → ADC_IL、2 2 → GND
      | モデルの範囲　　　　; Simscape標準コンデンサの集中定数表現。材質、DCバイアス、周波数依存ESR/ESL、寿命・温度特性を型番から自動再現するモデルではない。
      | モデル設定　　　　　; c=100 nF、r=1 µΩ、g=0 S。これらは保存モデルの設定値であり、すべてが実部品の保証値という意味ではない。
      | 損失の扱い　　　　　; 保存モデルの直列抵抗rと実部品の周波数・温度依存ESRは区別する。容量値が一致しても損失・リプル電流・寿命の成立確認にはならない。
      | 確認の範囲　　　　　; 本説明は保存回路の部品情報・端子割当・既存設計意図を整理したもの。今回の説明更新によって新たな動作試験や実機検証を実施した意味ではない。
      | 設計記録　　　　　　; evaluation\component_annotations_20261022_r01\before_graph.json
      | evaluation\component_annotations_20261022_r01\before_metadata.json
      | evaluation\protection_capacitor_integration_20261021_r01\final_delivery\independent_readback\physical_bom.json
      | evaluation\protection_capacitor_integration_20261021_r01\capacitor_review\capacitor_inventory_after_c04.json
      | 
      | 【周波数・ノイズと配置の説明】
      | 周波数面の役割　　　; 電流検出ICの出力をR26の100 Ωで分離し、ADC入力側で高周波成分を弱めて取得用電荷を保持する。
      | 対象周波数の目安　　; 100 Ωと100 nFの理想1次RC遮断周波数は約15.9 kHz、時定数は10 µs。これより高い周波数の成分を徐々に弱める。
      | ノイズの発生源　　　; シャントで検出する電流リプル、電力段から検出系へ結合する切替えノイズ、ADCのCH3入力取得時の電荷移動。
      | 他のコンデンサとの差; 電流検出ICの電源用100 nF（C22/C24）は電源を支える。本品は信号に作用するため、容量を変えると測定速度やソフト保護の応答も変わる。
      | 周波数説明の範囲　　; 15.9 kHzは100 Ωと100 nFだけの理想計算。電流検出ICの出力インピーダンス・帯域、ADCの取得条件を含む実際の応答や折り返し雑音の抑制を保証しない。
      | 周波数説明の根拠　　; TI Precision Labs：Passive Components and Circuits
      | https://www.ti.com/content/dam/videos/external-videos/en-us/4/3816841626001/6119035031001.mp4/subassets/passive_components_and_circuits_2.pdf
      | Microchip：MCP3204/3208 datasheet
      | https://ww1.microchip.com/downloads/en/DeviceDoc/21298E.pdf
      | 
      | 【この説明欄の略語・記号】
      | 用語1　　　　　　　 ; MLCC：Multilayer Ceramic Capacitor（積層セラミックコンデンサ）。薄いセラミック誘電体と電極を重ねたコンデンサ。対象周波数は容量・実装・寄生成分で変わるため、MLCCという分類だけでは決めない。
      | 用語2　　　　　　　 ; ESR：Equivalent Series Resistance（等価直列抵抗）。コンデンサの損失を直列抵抗で表した量。周波数・温度で変わり、損失とリプル電圧に関係する。
      | 用語3　　　　　　　 ; ESL：Equivalent Series Inductance（等価直列インダクタンス）。端子や電極などの寄生インダクタンスを表す。高い周波数ではバイパス効果を制限する。
      | 用語4　　　　　　　 ; DC：Direct Current（直流）。ここでは直流電源または直流成分。DCバイアスはコンデンサに重なる直流電圧を指す。
      | 用語5　　　　　　　 ; ADC：Analog-to-Digital Converter（アナログ・デジタル変換器）。測定電圧をデジタル値へ変換する回路。電流や温度も、センサーで電圧へ変換した後に読み取る。
      | 用語6　　　　　　　 ; IC：Integrated Circuit（集積回路）。複数の電子素子と機能を小さな半導体チップに集積した部品。
      | 用語7　　　　　　　 ; CH：Channel（測定チャネル）。CH0〜CH7はADCの入力番号であり、同時測定を意味しない。
      | 用語8　　　　　　　 ; RC：Resistor-Capacitor（抵抗とコンデンサの組合せ）。主に測定信号のフィルタや時定数を作る。カットオフ周波数は実際の接続と抵抗・容量から求める。
      | 用語9　　　　　　　 ; INA：この説明ではTI製電流検出アンプU2/U3を指す型番系列の略記。INA241A3の先頭文字を使った呼び方。メーカーが定めた英語の正式展開を推測したものではない。
      | 用語10　　　　　　　; fc：Cutoff Frequency（遮断周波数）。フィルタの信号を通す側と弱める側を表す目安。ここでの理想1次RC回路では振幅が低周波側の約70.7%になる周波数で、これ以上が急にゼロになるわけではない。
      | 用語11　　　　　　　; τ：Time Constant（時定数）。1次RC回路では抵抗Rと容量Cの積で、単位は秒。入力が急変した後の応答の速さを表す。τだけ経過すると最終変化量の約63%まで変化する。
      | 用語12　　　　　　　; GND：Ground（回路の基準電位・電流帰路）。この図の共通基準。保護接地や大地への接続を意味するとは限らない。
      settings: AttributesFormatString=|
      | MLCC
      | 100 nF
  C26 : fl_lib/Electrical/Electrical Elements/Capacitor  Description=|  c=1e-07 F  r=1e-6 Ohm  g=0 1/Ohm  i_specify=off  i_priority=None  i=0 A  i_nominal_specify=off  i_nominal_value=1  i_nominal_unit=A  v_specify=off  v_priority=None  v=0 V  v_nominal_specify=off  v_nominal_value=1  v_nominal_unit=V  vc_specify=off  vc_priority=High  vc=0 V  vc_nominal_specify=off  vc_nominal_value=1  vc_nominal_unit=V
      | この回路での名前　　; C26
      | 部品名　　　　　　　; CC0603KRX7R9BB104
      | この回路での役割　　; バッテリー側の温度センサーU4の3.3 V電源を、瞬間的な変動から支えるためのコンデンサ。
      | ここでの動き　　　　; 温度を測る場所にあるU4の電源端子の近くで電流を補い、高周波の電流に短い帰り道を作る。離れたマイコン基板のコンデンサだけで代用する配置にはしない。
      | 
      | 【詳しい働き・仕様・接続・確認の範囲】
      | 部品種別　　　　　　; 積層セラミックコンデンサ（MLCC）
      | 部品分類　　　　　　; 積層セラミックコンデンサ（MLCC）
      | 公称値　　　　　　　; 100 nF
      | 配置目的　　　　　　; 温度センサー電源バイパス。対象ICはU4（TMP235A2DBZR）。
      | 意図する動作　　　　; 実際の温度測定場所にあるセンサーの直近。離れたMCU基板Cと共用しない。 測定箇所が異なる2個のセンサーに各100nFを保持。
      | 端子と接続　　　　　; 1 1 → 3V3、2 2 → GND
      | モデルの範囲　　　　; Simscape標準コンデンサの集中定数表現。材質、DCバイアス、周波数依存ESR/ESL、寿命・温度特性を型番から自動再現するモデルではない。
      | モデル設定　　　　　; c=100 nF、r=1 µΩ、g=0 S。これらは保存モデルの設定値であり、すべてが実部品の保証値という意味ではない。
      | 損失の扱い　　　　　; 保存モデルの直列抵抗rと実部品の周波数・温度依存ESRは区別する。容量値が一致しても損失・リプル電流・寿命の成立確認にはならない。
      | 確認の範囲　　　　　; 本説明は保存回路の部品情報・端子割当・既存設計意図を整理したもの。今回の説明更新によって新たな動作試験や実機検証を実施した意味ではない。
      | 設計記録　　　　　　; evaluation\component_annotations_20261022_r01\before_graph.json
      | evaluation\component_annotations_20261022_r01\before_metadata.json
      | evaluation\protection_capacitor_integration_20261021_r01\final_delivery\independent_readback\physical_bom.json
      | evaluation\protection_capacitor_integration_20261021_r01\capacitor_review\capacitor_inventory_after_c04.json
      | evaluation\layout_readability_20261022_r01\capacitor_review\exact_snapshot_capacitor_review.json
      | 
      | 【周波数・ノイズと配置の説明】
      | 周波数面の役割　　　; U4（バッテリー側温度センサー）の電源端子直近で、瞬間的な電流を供給する局所バイパス。
      | 対象周波数の目安　　; そのICの内部動作や周辺の通信、周囲のスイッチングによる高周波成分を対象にする。100 nFという容量だけから「何MHzまで効く」とは決められない。
      | ノイズの発生源　　　; IC内部の回路動作に伴う電源電流の変化、3.3 V配線を経由する電源変動、近傍のデジタル信号やゲート駆動からの結合。
      | 他のコンデンサとの差; 離れたC18や電源装置側の大きな容量は低い周波数側の蓄積を補う。配線の寄生インダクタンスがあるため、同じ電源ネットでもIC直近の本品を完全に代替できない。
      | 周波数説明の範囲　　; 狙うノイズの周波数と、この部品が実装後に有効な周波数範囲は別である。実効容量、等価直列抵抗、等価直列インダクタンス、配線を含む自己共振で変わるため、型番名や公称容量だけから有効帯域の上限を断定しない。
      | 周波数説明の根拠　　; TDK：Low-ESL Multilayer Ceramic Capacitors
      | https://product.tdk.com/system/files/dam/doc/content/emc-guidebook/en/eemc_product_01.pdf
      | 村田製作所：コンデンサを使いこなす
      | https://www.murata.com/en-GB/products/emc/emifil/library/knowhow/basic/chapter06-p8
      | 
      | 【この説明欄の略語・記号】
      | 用語1　　　　　　　 ; MLCC：Multilayer Ceramic Capacitor（積層セラミックコンデンサ）。薄いセラミック誘電体と電極を重ねたコンデンサ。対象周波数は容量・実装・寄生成分で変わるため、MLCCという分類だけでは決めない。
      | 用語2　　　　　　　 ; ESR：Equivalent Series Resistance（等価直列抵抗）。コンデンサの損失を直列抵抗で表した量。周波数・温度で変わり、損失とリプル電圧に関係する。
      | 用語3　　　　　　　 ; ESL：Equivalent Series Inductance（等価直列インダクタンス）。端子や電極などの寄生インダクタンスを表す。高い周波数ではバイパス効果を制限する。
      | 用語4　　　　　　　 ; DC：Direct Current（直流）。ここでは直流電源または直流成分。DCバイアスはコンデンサに重なる直流電圧を指す。
      | 用語5　　　　　　　 ; IC：Integrated Circuit（集積回路）。複数の電子素子と機能を小さな半導体チップに集積した部品。
      | 用語6　　　　　　　 ; MCU：Microcontroller Unit（マイクロコントローラ）。プログラムを実行し、測定値の処理や出力制御を担当する小型計算機。
      | 用語7　　　　　　　 ; GND：Ground（回路の基準電位・電流帰路）。この図の共通基準。保護接地や大地への接続を意味するとは限らない。
      settings: AttributesFormatString=|
      | MLCC
      | 100 nF
  C27 : fl_lib/Electrical/Electrical Elements/Capacitor  Description=|  c=6.8e-10 F  r=1e-6 Ohm  g=0 1/Ohm  i_specify=off  i_priority=None  i=0 A  i_nominal_specify=off  i_nominal_value=1  i_nominal_unit=A  v_specify=off  v_priority=None  v=0 V  v_nominal_specify=off  v_nominal_value=1  v_nominal_unit=V  vc_specify=off  vc_priority=High  vc=0 V  vc_nominal_specify=off  vc_nominal_value=1  vc_nominal_unit=V
      | この回路での名前　　; C27
      | 部品名　　　　　　　; AC0603JPNPO9BN681
      | この回路での役割　　; バッテリーの温度信号に重なる速い電気的な乱れを、読み取り回路の入口で弱めるための小容量コンデンサ。
      | ここでの動き　　　　; 抵抗R28を通った信号のADC_TBATと共通GNDの間に680 pFを置き、U1のCH4で読み取る直前に小さな電荷を保持する。温度センサーの電源を支えるコンデンサとは別の役割。
      | 
      | 【詳しい働き・仕様・接続・確認の範囲】
      | 部品種別　　　　　　; 積層セラミックコンデンサ（MLCC）
      | 部品分類　　　　　　; 積層セラミックコンデンサ（MLCC）
      | 公称値　　　　　　　; 680 pF
      | 配置目的　　　　　　; 温度ADC取得/小信号フィルタ。対象はR2847Ω、U1CH4。
      | 意図する動作　　　　; ADC入力近傍。長い温度信号線とリターンを対で扱う。 680pFと47Ωの外付RC約32nsだけで総整定を主張できない。TMP235駆動能力・MCP3208取得時間を合わせるまで維持。
      | 端子と接続　　　　　; 1 1 → ADC_TBAT、2 2 → GND
      | モデルの範囲　　　　; Simscape標準コンデンサの集中定数表現。材質、DCバイアス、周波数依存ESR/ESL、寿命・温度特性を型番から自動再現するモデルではない。
      | モデル設定　　　　　; c=680 pF、r=1 µΩ、g=0 S。これらは保存モデルの設定値であり、すべてが実部品の保証値という意味ではない。
      | 損失の扱い　　　　　; 保存モデルの直列抵抗rと実部品の周波数・温度依存ESRは区別する。容量値が一致しても損失・リプル電流・寿命の成立確認にはならない。
      | 確認の範囲　　　　　; 本説明は保存回路の部品情報・端子割当・既存設計意図を整理したもの。今回の説明更新によって新たな動作試験や実機検証を実施した意味ではない。
      | 設計記録　　　　　　; evaluation\component_annotations_20261022_r01\before_graph.json
      | evaluation\component_annotations_20261022_r01\before_metadata.json
      | evaluation\protection_capacitor_integration_20261021_r01\final_delivery\independent_readback\physical_bom.json
      | evaluation\protection_capacitor_integration_20261021_r01\capacitor_review\capacitor_inventory_after_c04.json
      | 
      | 【周波数・ノイズと配置の説明】
      | 周波数面の役割　　　; 温度信号のADC入力付近で小さな電荷を蓄え、速い電気的な乱れをR28とともに抑える。
      | 対象周波数の目安　　; 47 Ωと680 pFだけの理想1次RC遮断周波数は約4.98 MHz、時定数は約32 ns。これは温度変化の帯域を表す数値ではなく、外付け電気回路だけの計算である。
      | ノイズの発生源　　　; 温度センサーとADCの間の配線に結合するスイッチング/通信の速い成分や、ADCのCH4取得時の電荷移動。温度そのものがMHzで変わるという意味ではない。
      | 他のコンデンサとの差; C26/C28の100 nFは温度センサーの電源を支える。本品680 pFは信号側の小容量で、大容量の電源平滑用コンデンサとは用途が異なる。
      | 周波数説明の範囲　　; TMP235の駆動能力、配線、MCP3208の取得時間を含む総整定時間は別評価。32 nsで測定が完成するとは主張しない。
      | 周波数説明の根拠　　; TI Precision Labs：Passive Components and Circuits
      | https://www.ti.com/content/dam/videos/external-videos/en-us/4/3816841626001/6119035031001.mp4/subassets/passive_components_and_circuits_2.pdf
      | Microchip：MCP3204/3208 datasheet
      | https://ww1.microchip.com/downloads/en/DeviceDoc/21298E.pdf
      | 
      | 【この説明欄の略語・記号】
      | 用語1　　　　　　　 ; MLCC：Multilayer Ceramic Capacitor（積層セラミックコンデンサ）。薄いセラミック誘電体と電極を重ねたコンデンサ。対象周波数は容量・実装・寄生成分で変わるため、MLCCという分類だけでは決めない。
      | 用語2　　　　　　　 ; ESR：Equivalent Series Resistance（等価直列抵抗）。コンデンサの損失を直列抵抗で表した量。周波数・温度で変わり、損失とリプル電圧に関係する。
      | 用語3　　　　　　　 ; ESL：Equivalent Series Inductance（等価直列インダクタンス）。端子や電極などの寄生インダクタンスを表す。高い周波数ではバイパス効果を制限する。
      | 用語4　　　　　　　 ; DC：Direct Current（直流）。ここでは直流電源または直流成分。DCバイアスはコンデンサに重なる直流電圧を指す。
      | 用語5　　　　　　　 ; ADC：Analog-to-Digital Converter（アナログ・デジタル変換器）。測定電圧をデジタル値へ変換する回路。電流や温度も、センサーで電圧へ変換した後に読み取る。
      | 用語6　　　　　　　 ; CH：Channel（測定チャネル）。CH0〜CH7はADCの入力番号であり、同時測定を意味しない。
      | 用語7　　　　　　　 ; RC：Resistor-Capacitor（抵抗とコンデンサの組合せ）。主に測定信号のフィルタや時定数を作る。カットオフ周波数は実際の接続と抵抗・容量から求める。
      | 用語8　　　　　　　 ; GND：Ground（回路の基準電位・電流帰路）。この図の共通基準。保護接地や大地への接続を意味するとは限らない。
      settings: AttributesFormatString=|
      | MLCC
      | 680 pF
  C28 : fl_lib/Electrical/Electrical Elements/Capacitor  Description=|  c=1e-07 F  r=1e-6 Ohm  g=0 1/Ohm  i_specify=off  i_priority=None  i=0 A  i_nominal_specify=off  i_nominal_value=1  i_nominal_unit=A  v_specify=off  v_priority=None  v=0 V  v_nominal_specify=off  v_nominal_value=1  v_nominal_unit=V  vc_specify=off  vc_priority=High  vc=0 V  vc_nominal_specify=off  vc_nominal_value=1  vc_nominal_unit=V
      | この回路での名前　　; C28
      | 部品名　　　　　　　; CC0603KRX7R9BB104
      | この回路での役割　　; 放熱器側の温度センサーU5の3.3 V電源を、瞬間的な変動から支えるためのコンデンサ。
      | ここでの動き　　　　; 温度を測る場所にあるU5の電源端子の近くで電流を補い、高周波の電流に短い帰り道を作る。離れたマイコン基板のコンデンサだけで代用する配置にはしない。
      | 
      | 【詳しい働き・仕様・接続・確認の範囲】
      | 部品種別　　　　　　; 積層セラミックコンデンサ（MLCC）
      | 部品分類　　　　　　; 積層セラミックコンデンサ（MLCC）
      | 公称値　　　　　　　; 100 nF
      | 配置目的　　　　　　; 温度センサー電源バイパス。対象ICはU5（TMP235A2DBZR）。
      | 意図する動作　　　　; 実際の温度測定場所にあるセンサーの直近。離れたMCU基板Cと共用しない。 測定箇所が異なる2個のセンサーに各100nFを保持。
      | 端子と接続　　　　　; 1 1 → 3V3、2 2 → GND
      | モデルの範囲　　　　; Simscape標準コンデンサの集中定数表現。材質、DCバイアス、周波数依存ESR/ESL、寿命・温度特性を型番から自動再現するモデルではない。
      | モデル設定　　　　　; c=100 nF、r=1 µΩ、g=0 S。これらは保存モデルの設定値であり、すべてが実部品の保証値という意味ではない。
      | 損失の扱い　　　　　; 保存モデルの直列抵抗rと実部品の周波数・温度依存ESRは区別する。容量値が一致しても損失・リプル電流・寿命の成立確認にはならない。
      | 確認の範囲　　　　　; 本説明は保存回路の部品情報・端子割当・既存設計意図を整理したもの。今回の説明更新によって新たな動作試験や実機検証を実施した意味ではない。
      | 設計記録　　　　　　; evaluation\component_annotations_20261022_r01\before_graph.json
      | evaluation\component_annotations_20261022_r01\before_metadata.json
      | evaluation\protection_capacitor_integration_20261021_r01\final_delivery\independent_readback\physical_bom.json
      | evaluation\protection_capacitor_integration_20261021_r01\capacitor_review\capacitor_inventory_after_c04.json
      | evaluation\layout_readability_20261022_r01\capacitor_review\exact_snapshot_capacitor_review.json
      | 
      | 【周波数・ノイズと配置の説明】
      | 周波数面の役割　　　; U5（放熱器側温度センサー）の電源端子直近で、瞬間的な電流を供給する局所バイパス。
      | 対象周波数の目安　　; そのICの内部動作や周辺の通信、周囲のスイッチングによる高周波成分を対象にする。100 nFという容量だけから「何MHzまで効く」とは決められない。
      | ノイズの発生源　　　; IC内部の回路動作に伴う電源電流の変化、3.3 V配線を経由する電源変動、近傍のデジタル信号やゲート駆動からの結合。
      | 他のコンデンサとの差; 離れたC18や電源装置側の大きな容量は低い周波数側の蓄積を補う。配線の寄生インダクタンスがあるため、同じ電源ネットでもIC直近の本品を完全に代替できない。
      | 周波数説明の範囲　　; 狙うノイズの周波数と、この部品が実装後に有効な周波数範囲は別である。実効容量、等価直列抵抗、等価直列インダクタンス、配線を含む自己共振で変わるため、型番名や公称容量だけから有効帯域の上限を断定しない。
      | 周波数説明の根拠　　; TDK：Low-ESL Multilayer Ceramic Capacitors
      | https://product.tdk.com/system/files/dam/doc/content/emc-guidebook/en/eemc_product_01.pdf
      | 村田製作所：コンデンサを使いこなす
      | https://www.murata.com/en-GB/products/emc/emifil/library/knowhow/basic/chapter06-p8
      | 
      | 【この説明欄の略語・記号】
      | 用語1　　　　　　　 ; MLCC：Multilayer Ceramic Capacitor（積層セラミックコンデンサ）。薄いセラミック誘電体と電極を重ねたコンデンサ。対象周波数は容量・実装・寄生成分で変わるため、MLCCという分類だけでは決めない。
      | 用語2　　　　　　　 ; ESR：Equivalent Series Resistance（等価直列抵抗）。コンデンサの損失を直列抵抗で表した量。周波数・温度で変わり、損失とリプル電圧に関係する。
      | 用語3　　　　　　　 ; ESL：Equivalent Series Inductance（等価直列インダクタンス）。端子や電極などの寄生インダクタンスを表す。高い周波数ではバイパス効果を制限する。
      | 用語4　　　　　　　 ; DC：Direct Current（直流）。ここでは直流電源または直流成分。DCバイアスはコンデンサに重なる直流電圧を指す。
      | 用語5　　　　　　　 ; IC：Integrated Circuit（集積回路）。複数の電子素子と機能を小さな半導体チップに集積した部品。
      | 用語6　　　　　　　 ; MCU：Microcontroller Unit（マイクロコントローラ）。プログラムを実行し、測定値の処理や出力制御を担当する小型計算機。
      | 用語7　　　　　　　 ; GND：Ground（回路の基準電位・電流帰路）。この図の共通基準。保護接地や大地への接続を意味するとは限らない。
      settings: AttributesFormatString=|
      | MLCC
      | 100 nF
  C29 : fl_lib/Electrical/Electrical Elements/Capacitor  Description=|  c=6.8e-10 F  r=1e-6 Ohm  g=0 1/Ohm  i_specify=off  i_priority=None  i=0 A  i_nominal_specify=off  i_nominal_value=1  i_nominal_unit=A  v_specify=off  v_priority=None  v=0 V  v_nominal_specify=off  v_nominal_value=1  v_nominal_unit=V  vc_specify=off  vc_priority=High  vc=0 V  vc_nominal_specify=off  vc_nominal_value=1  vc_nominal_unit=V
      | この回路での名前　　; C29
      | 部品名　　　　　　　; AC0603JPNPO9BN681
      | この回路での役割　　; 放熱器の温度信号に重なる速い電気的な乱れを、読み取り回路の入口で弱めるための小容量コンデンサ。
      | ここでの動き　　　　; 抵抗R29を通った信号のADC_TSINKと共通GNDの間に680 pFを置き、U1のCH5で読み取る直前に小さな電荷を保持する。温度センサーの電源を支えるコンデンサとは別の役割。
      | 
      | 【詳しい働き・仕様・接続・確認の範囲】
      | 部品種別　　　　　　; 積層セラミックコンデンサ（MLCC）
      | 部品分類　　　　　　; 積層セラミックコンデンサ（MLCC）
      | 公称値　　　　　　　; 680 pF
      | 配置目的　　　　　　; 温度ADC取得/小信号フィルタ。対象はR2947Ω、U1CH5。
      | 意図する動作　　　　; ADC入力近傍。長い温度信号線とリターンを対で扱う。 680pFと47Ωの外付RC約32nsだけで総整定を主張できない。TMP235駆動能力・MCP3208取得時間を合わせるまで維持。
      | 端子と接続　　　　　; 1 1 → ADC_TSINK、2 2 → GND
      | モデルの範囲　　　　; Simscape標準コンデンサの集中定数表現。材質、DCバイアス、周波数依存ESR/ESL、寿命・温度特性を型番から自動再現するモデルではない。
      | モデル設定　　　　　; c=680 pF、r=1 µΩ、g=0 S。これらは保存モデルの設定値であり、すべてが実部品の保証値という意味ではない。
      | 損失の扱い　　　　　; 保存モデルの直列抵抗rと実部品の周波数・温度依存ESRは区別する。容量値が一致しても損失・リプル電流・寿命の成立確認にはならない。
      | 確認の範囲　　　　　; 本説明は保存回路の部品情報・端子割当・既存設計意図を整理したもの。今回の説明更新によって新たな動作試験や実機検証を実施した意味ではない。
      | 設計記録　　　　　　; evaluation\component_annotations_20261022_r01\before_graph.json
      | evaluation\component_annotations_20261022_r01\before_metadata.json
      | evaluation\protection_capacitor_integration_20261021_r01\final_delivery\independent_readback\physical_bom.json
      | evaluation\protection_capacitor_integration_20261021_r01\capacitor_review\capacitor_inventory_after_c04.json
      | 
      | 【周波数・ノイズと配置の説明】
      | 周波数面の役割　　　; 温度信号のADC入力付近で小さな電荷を蓄え、速い電気的な乱れをR29とともに抑える。
      | 対象周波数の目安　　; 47 Ωと680 pFだけの理想1次RC遮断周波数は約4.98 MHz、時定数は約32 ns。これは温度変化の帯域を表す数値ではなく、外付け電気回路だけの計算である。
      | ノイズの発生源　　　; 温度センサーとADCの間の配線に結合するスイッチング/通信の速い成分や、ADCのCH5取得時の電荷移動。温度そのものがMHzで変わるという意味ではない。
      | 他のコンデンサとの差; C26/C28の100 nFは温度センサーの電源を支える。本品680 pFは信号側の小容量で、大容量の電源平滑用コンデンサとは用途が異なる。
      | 周波数説明の範囲　　; TMP235の駆動能力、配線、MCP3208の取得時間を含む総整定時間は別評価。32 nsで測定が完成するとは主張しない。
      | 周波数説明の根拠　　; TI Precision Labs：Passive Components and Circuits
      | https://www.ti.com/content/dam/videos/external-videos/en-us/4/3816841626001/6119035031001.mp4/subassets/passive_components_and_circuits_2.pdf
      | Microchip：MCP3204/3208 datasheet
      | https://ww1.microchip.com/downloads/en/DeviceDoc/21298E.pdf
      | 
      | 【この説明欄の略語・記号】
      | 用語1　　　　　　　 ; MLCC：Multilayer Ceramic Capacitor（積層セラミックコンデンサ）。薄いセラミック誘電体と電極を重ねたコンデンサ。対象周波数は容量・実装・寄生成分で変わるため、MLCCという分類だけでは決めない。
      | 用語2　　　　　　　 ; ESR：Equivalent Series Resistance（等価直列抵抗）。コンデンサの損失を直列抵抗で表した量。周波数・温度で変わり、損失とリプル電圧に関係する。
      | 用語3　　　　　　　 ; ESL：Equivalent Series Inductance（等価直列インダクタンス）。端子や電極などの寄生インダクタンスを表す。高い周波数ではバイパス効果を制限する。
      | 用語4　　　　　　　 ; DC：Direct Current（直流）。ここでは直流電源または直流成分。DCバイアスはコンデンサに重なる直流電圧を指す。
      | 用語5　　　　　　　 ; ADC：Analog-to-Digital Converter（アナログ・デジタル変換器）。測定電圧をデジタル値へ変換する回路。電流や温度も、センサーで電圧へ変換した後に読み取る。
      | 用語6　　　　　　　 ; CH：Channel（測定チャネル）。CH0〜CH7はADCの入力番号であり、同時測定を意味しない。
      | 用語7　　　　　　　 ; RC：Resistor-Capacitor（抵抗とコンデンサの組合せ）。主に測定信号のフィルタや時定数を作る。カットオフ周波数は実際の接続と抵抗・容量から求める。
      | 用語8　　　　　　　 ; GND：Ground（回路の基準電位・電流帰路）。この図の共通基準。保護接地や大地への接続を意味するとは限らない。
      settings: AttributesFormatString=|
      | MLCC
      | 680 pF
  C3 : fl_lib/Electrical/Electrical Elements/Capacitor  Description=|  c=0.00046999999999999999 F  r=1e-6 Ohm  g=0 1/Ohm  i_specify=off  i_priority=None  i=0 A  i_nominal_specify=off  i_nominal_value=1  i_nominal_unit=A  v_specify=off  v_priority=None  v=0 V  v_nominal_specify=off  v_nominal_value=1  v_nominal_unit=V  vc_specify=off  vc_priority=High  vc=0 V  vc_nominal_specify=off  vc_nominal_value=1  vc_nominal_unit=V
      | この回路での名前　　; C3
      | 部品名　　　　　　　; UCY2C471MHD
      | この回路での役割　　; 太陽光パネルから給電される主電力段の入力側に電荷を蓄え、入力電圧の落ち込みや変動を抑えるためのコンデンサ。
      | ここでの動き　　　　; 入力電源VINと共通GNDの間に470 µFを3個並列に置き、降圧回路が電流を必要とするときに電荷を補う。速い変化への対応は、近くのC7〜C10と分担する設計。
      | 
      | 【詳しい働き・仕様・接続・確認の範囲】
      | 部品種別　　　　　　; アルミ電解コンデンサ（有極性）
      | 部品分類　　　　　　; アルミ電解コンデンサ（有極性）
      | 公称値　　　　　　　; 470 uF
      | 配置目的　　　　　　; 入力バルク。対象はL2入力フィルタとQ1/Q2電力段。
      | 意図する動作　　　　; VIN–GND間の入力バルクとして、降圧電力段が必要とする電荷を供給し入力電圧変動を抑える。現構成は470 µFを3個。分流・ESR・温度上昇・配線寄生の適合は別評価。
      | 端子と接続　　　　　; 2 n → GND、1 p → VIN
      | モデルの範囲　　　　; Simscape標準コンデンサの集中定数表現。材質、DCバイアス、周波数依存ESR/ESL、寿命・温度特性を型番から自動再現するモデルではない。
      | モデル設定　　　　　; c=470 µF、r=1 µΩ、g=0 S。これらは保存モデルの設定値であり、すべてが実部品の保証値という意味ではない。
      | 損失の扱い　　　　　; 保存モデルの直列抵抗rと実部品の周波数・温度依存ESRは区別する。容量値が一致しても損失・リプル電流・寿命の成立確認にはならない。
      | 確認の範囲　　　　　; 本説明は保存回路の部品情報・端子割当・既存設計意図を整理したもの。今回の説明更新によって新たな動作試験や実機検証を実施した意味ではない。
      | 設計記録　　　　　　; evaluation\component_annotations_20261022_r01\before_graph.json
      | evaluation\component_annotations_20261022_r01\before_metadata.json
      | evaluation\protection_capacitor_integration_20261021_r01\final_delivery\independent_readback\physical_bom.json
      | evaluation\protection_capacitor_integration_20261021_r01\capacitor_review\capacitor_inventory_after_c04.json
      | 
      | 【周波数・ノイズと配置の説明】
      | 周波数面の役割　　　; 入力電圧の比較的ゆっくりした変動を抑え、主電力段が必要な電荷を蓄える。
      | 対象周波数の目安　　; 起動・日射/負荷変動などの低い周波数側から、主スイッチング周期の電荷出入りまでを受け持つ。主電力段の既存比較計算では50 kHzを仮定している。これは比較シナリオの値であり、今回の保存図から実行中PWM周波数を測定した値ではない。
      | ノイズの発生源　　　; Q1のオン期間に入力から電流を取り出すため、入力電流は脈動する。パネル/配線/L2側がすぐ補えない電流をこの容量群が補う。
      | 他のコンデンサとの差; 470 µF×3個の電解は蓄積量を担当する。C7のフィルムとC8～C10のMLCCは速い電流変化への局所経路を補う。同じ周波数で複数群が分担し、境界周波数で役割が切り替わるわけではない。
      | 周波数説明の範囲　　; 狙うノイズの周波数と、この部品が実装後に有効な周波数範囲は別である。実効容量、等価直列抵抗、等価直列インダクタンス、配線を含む自己共振で変わるため、型番名や公称容量だけから有効帯域の上限を断定しない。
      | 周波数説明の根拠　　; 村田製作所：コンデンサのインピーダンス・ESRと周波数の関係
      | https://article.murata.com/en-global/article/impedance-esr-frequency-characteristics-in-capacitors
      | 村田製作所：コンデンサを使いこなす
      | https://www.murata.com/en-GB/products/emc/emifil/library/knowhow/basic/chapter06-p8
      | 
      | 【この説明欄の略語・記号】
      | 用語1　　　　　　　 ; MLCC：Multilayer Ceramic Capacitor（積層セラミックコンデンサ）。薄いセラミック誘電体と電極を重ねたコンデンサ。対象周波数は容量・実装・寄生成分で変わるため、MLCCという分類だけでは決めない。
      | 用語2　　　　　　　 ; ESR：Equivalent Series Resistance（等価直列抵抗）。コンデンサの損失を直列抵抗で表した量。周波数・温度で変わり、損失とリプル電圧に関係する。
      | 用語3　　　　　　　 ; ESL：Equivalent Series Inductance（等価直列インダクタンス）。端子や電極などの寄生インダクタンスを表す。高い周波数ではバイパス効果を制限する。
      | 用語4　　　　　　　 ; DC：Direct Current（直流）。ここでは直流電源または直流成分。DCバイアスはコンデンサに重なる直流電圧を指す。
      | 用語5　　　　　　　 ; PWM：Pulse Width Modulation（パルス幅変調）。周期に対するON時間の割合を変えて、スイッチの平均的な電力伝達を調整する方式。
      | 用語6　　　　　　　 ; GND：Ground（回路の基準電位・電流帰路）。この図の共通基準。保護接地や大地への接続を意味するとは限らない。
      | 用語7　　　　　　　 ; VIN/VOUT：入力電圧・出力電圧を表す端子／ネット名。INは入力、OUTは出力。電源変換器の電力端子なのか、検出用端子なのかは対象部品によって異なるため、端子と接続の説明に従う。
      settings: AttributesFormatString=|
      | 電解
      | 470 µF
  C30 : fl_lib/Electrical/Electrical Elements/Capacitor  Description=|  c=1e-06 F  r=1e-6 Ohm  g=0 1/Ohm  i_specify=off  i_priority=None  i=0 A  i_nominal_specify=off  i_nominal_value=1  i_nominal_unit=A  v_specify=off  v_priority=None  v=0 V  v_nominal_specify=off  v_nominal_value=1  v_nominal_unit=V  vc_specify=off  vc_priority=High  vc=0 V  vc_nominal_specify=off  vc_nominal_value=1  vc_nominal_unit=V
      | この回路での名前　　; C30
      | 部品名　　　　　　　; C2012X7R1H105K125AB
      | この回路での役割　　; 計測の基準となる2.5 Vを作るU6へ、安定した入力電源を渡すためのコンデンサ。
      | ここでの動き　　　　; U6の3.3 V入力端子の近くで電荷を補い、入力電源の速い変動を抑える。U6が作る2.5 V出力側のC31とは、接続先も役割も異なる。
      | 
      | 【詳しい働き・仕様・接続・確認の範囲】
      | 部品種別　　　　　　; 積層セラミックコンデンサ（MLCC）
      | 部品分類　　　　　　; 積層セラミックコンデンサ（MLCC）
      | 公称値　　　　　　　; 1 uF
      | 配置目的　　　　　　; 基準源入力バイパス。対象ICはU6（REF3025EAIDBZR）。
      | 意図する動作　　　　; U6入力ピン直近で3V3→GNDへ。 低ノイズ基準源の入力局所C。出力C31とは別ノード・役割。
      | 端子と接続　　　　　; 1 1 → 3V3、2 2 → GND
      | モデルの範囲　　　　; Simscape標準コンデンサの集中定数表現。材質、DCバイアス、周波数依存ESR/ESL、寿命・温度特性を型番から自動再現するモデルではない。
      | モデル設定　　　　　; c=1 µF、r=1 µΩ、g=0 S。これらは保存モデルの設定値であり、すべてが実部品の保証値という意味ではない。
      | 損失の扱い　　　　　; 保存モデルの直列抵抗rと実部品の周波数・温度依存ESRは区別する。容量値が一致しても損失・リプル電流・寿命の成立確認にはならない。
      | 確認の範囲　　　　　; 本説明は保存回路の部品情報・端子割当・既存設計意図を整理したもの。今回の説明更新によって新たな動作試験や実機検証を実施した意味ではない。
      | 設計記録　　　　　　; evaluation\component_annotations_20261022_r01\before_graph.json
      | evaluation\component_annotations_20261022_r01\before_metadata.json
      | evaluation\protection_capacitor_integration_20261021_r01\final_delivery\independent_readback\physical_bom.json
      | evaluation\protection_capacitor_integration_20261021_r01\capacitor_review\capacitor_inventory_after_c04.json
      | evaluation\layout_readability_20261022_r01\capacitor_review\exact_snapshot_capacitor_review.json
      | 
      | 【周波数・ノイズと配置の説明】
      | 周波数面の役割　　　; 基準電圧IC U6の入力電源を局所的に安定させる。
      | 対象周波数の目安　　; 3.3 V電源の変動や高周波成分を対象とする。1 µFだけで遮断周波数は定まらず、供給元/配線のインピーダンスに依存する。
      | ノイズの発生源　　　; 3.3 VにつながるADC・マイコン・計測ICの消費電流変化と、補助電源のスイッチング成分。
      | 他のコンデンサとの差; C31は2.5 V基準の出力側にあり、ADCが取り出す電荷と基準源の安定性に関係する。本品はその入力側であり同じノードではない。
      | 周波数説明の範囲　　; 狙うノイズの周波数と、この部品が実装後に有効な周波数範囲は別である。実効容量、等価直列抵抗、等価直列インダクタンス、配線を含む自己共振で変わるため、型番名や公称容量だけから有効帯域の上限を断定しない。
      | 周波数説明の根拠　　; TDK：Low-ESL Multilayer Ceramic Capacitors
      | https://product.tdk.com/system/files/dam/doc/content/emc-guidebook/en/eemc_product_01.pdf
      | 村田製作所：コンデンサを使いこなす
      | https://www.murata.com/en-GB/products/emc/emifil/library/knowhow/basic/chapter06-p8
      | 
      | 【この説明欄の略語・記号】
      | 用語1　　　　　　　 ; MLCC：Multilayer Ceramic Capacitor（積層セラミックコンデンサ）。薄いセラミック誘電体と電極を重ねたコンデンサ。対象周波数は容量・実装・寄生成分で変わるため、MLCCという分類だけでは決めない。
      | 用語2　　　　　　　 ; ESR：Equivalent Series Resistance（等価直列抵抗）。コンデンサの損失を直列抵抗で表した量。周波数・温度で変わり、損失とリプル電圧に関係する。
      | 用語3　　　　　　　 ; ESL：Equivalent Series Inductance（等価直列インダクタンス）。端子や電極などの寄生インダクタンスを表す。高い周波数ではバイパス効果を制限する。
      | 用語4　　　　　　　 ; DC：Direct Current（直流）。ここでは直流電源または直流成分。DCバイアスはコンデンサに重なる直流電圧を指す。
      | 用語5　　　　　　　 ; ADC：Analog-to-Digital Converter（アナログ・デジタル変換器）。測定電圧をデジタル値へ変換する回路。電流や温度も、センサーで電圧へ変換した後に読み取る。
      | 用語6　　　　　　　 ; IC：Integrated Circuit（集積回路）。複数の電子素子と機能を小さな半導体チップに集積した部品。
      | 用語7　　　　　　　 ; GND：Ground（回路の基準電位・電流帰路）。この図の共通基準。保護接地や大地への接続を意味するとは限らない。
      settings: AttributesFormatString=|
      | MLCC
      | 1 µF
  C31 : fl_lib/Electrical/Electrical Elements/Capacitor  Description=|  c=1e-06 F  r=1e-6 Ohm  g=0 1/Ohm  i_specify=off  i_priority=None  i=0 A  i_nominal_specify=off  i_nominal_value=1  i_nominal_unit=A  v_specify=off  v_priority=None  v=0 V  v_nominal_specify=off  v_nominal_value=1  v_nominal_unit=V  vc_specify=off  vc_priority=High  vc=0 V  vc_nominal_specify=off  vc_nominal_value=1  vc_nominal_unit=V
      | この回路での名前　　; C31
      | 部品名　　　　　　　; C2012X7R1H105K125AB
      | この回路での役割　　; 計測の物差しとなる2.5 V基準電圧を支え、読み取り時に必要な電荷を近くで補うためのコンデンサ。
      | ここでの動き　　　　; 基準電圧IC U6の出力につながる枝に、抵抗R30と直列で1 µFを置く。R30はこのコンデンサの枝にだけ入り、U1などへ渡す基準電圧の本線に直列に入るものではない。
      | 
      | 【詳しい働き・仕様・接続・確認の範囲】
      | 部品種別　　　　　　; 積層セラミックコンデンサ（MLCC）
      | 部品分類　　　　　　; 積層セラミックコンデンサ（MLCC）
      | 公称値　　　　　　　; 1 uF
      | 配置目的　　　　　　; 基準源出力安定化/電荷供給。対象はU6OUT2、R30=0.1Ω、U1VREF15、U2/U3REF。
      | 意図する動作　　　　; VREF_CAP_NODEからGND。R30はCの枝だけ、ADC基準net本流に直列挿入しない。 既存R2-P11を維持。1µFと0.1Ωを勝手に削除せずREF3025EのESR窓を再確認。
      | 端子と接続　　　　　; 1 1 → VREF_CAP_NODE、2 2 → GND
      | モデルの範囲　　　　; Simscape標準コンデンサの集中定数表現。材質、DCバイアス、周波数依存ESR/ESL、寿命・温度特性を型番から自動再現するモデルではない。
      | モデル設定　　　　　; c=1 µF、r=1 µΩ、g=0 S。これらは保存モデルの設定値であり、すべてが実部品の保証値という意味ではない。
      | 損失の扱い　　　　　; 保存モデルの直列抵抗rと実部品の周波数・温度依存ESRは区別する。容量値が一致しても損失・リプル電流・寿命の成立確認にはならない。
      | 確認の範囲　　　　　; 本説明は保存回路の部品情報・端子割当・既存設計意図を整理したもの。今回の説明更新によって新たな動作試験や実機検証を実施した意味ではない。
      | 設計記録　　　　　　; evaluation\component_annotations_20261022_r01\before_graph.json
      | evaluation\component_annotations_20261022_r01\before_metadata.json
      | evaluation\protection_capacitor_integration_20261021_r01\final_delivery\independent_readback\physical_bom.json
      | evaluation\protection_capacitor_integration_20261021_r01\capacitor_review\capacitor_inventory_after_c04.json
      | 
      | 【周波数・ノイズと配置の説明】
      | 周波数面の役割　　　; 基準電圧の局所電荷を保持し、U6の応答とADC基準端子への負荷変動を支える。
      | 対象周波数の目安　　; 基準源の過渡応答とADCが基準端子から電荷を取り出す際の変動が対象。R30=0.1 Ωはコンデンサ枝にだけ入るため、これと1 µFから算出した周波数を「ADC基準信号全体の遮断周波数」とはしない。
      | ノイズの発生源　　　; ADCの変換動作で基準端子の負荷が変化すること、電流検出ICの基準端子を含む2.5 V系の電流変化。
      | 他のコンデンサとの差; C30は3.3 V入力のバイパス。本品は2.5 V側の出力容量で、低い等価直列抵抗にすれば必ず良いわけではなく、REF3025Eの容量/直列抵抗条件が関わる。
      | 周波数説明の範囲　　; ここでは既存R30-C31枝の意味を説明する。REF3025Eの安定性条件の適合や動的試験完了を新たに主張しない。
      | 周波数説明の根拠　　; Microchip：MCP3204/3208 datasheet
      | https://ww1.microchip.com/downloads/en/DeviceDoc/21298E.pdf
      | TDK：電解コンデンサからMLCCへの置換ガイド
      | https://product.tdk.com/en/techlibrary/solutionguide/mlcc_replace-guide.html
      | 
      | 【この説明欄の略語・記号】
      | 用語1　　　　　　　 ; MLCC：Multilayer Ceramic Capacitor（積層セラミックコンデンサ）。薄いセラミック誘電体と電極を重ねたコンデンサ。対象周波数は容量・実装・寄生成分で変わるため、MLCCという分類だけでは決めない。
      | 用語2　　　　　　　 ; ESR：Equivalent Series Resistance（等価直列抵抗）。コンデンサの損失を直列抵抗で表した量。周波数・温度で変わり、損失とリプル電圧に関係する。
      | 用語3　　　　　　　 ; ESL：Equivalent Series Inductance（等価直列インダクタンス）。端子や電極などの寄生インダクタンスを表す。高い周波数ではバイパス効果を制限する。
      | 用語4　　　　　　　 ; DC：Direct Current（直流）。ここでは直流電源または直流成分。DCバイアスはコンデンサに重なる直流電圧を指す。
      | 用語5　　　　　　　 ; ADC：Analog-to-Digital Converter（アナログ・デジタル変換器）。測定電圧をデジタル値へ変換する回路。電流や温度も、センサーで電圧へ変換した後に読み取る。
      | 用語6　　　　　　　 ; IC：Integrated Circuit（集積回路）。複数の電子素子と機能を小さな半導体チップに集積した部品。
      | 用語7　　　　　　　 ; GND：Ground（回路の基準電位・電流帰路）。この図の共通基準。保護接地や大地への接続を意味するとは限らない。
      | 用語8　　　　　　　 ; VREF/REF：基準電圧を表す端子名。REFはReference（基準）の意味。ADCの変換尺度や電流アンプの出力基準に使う。REF1/REF2の接続電位は個別に確認する。
      settings: AttributesFormatString=|
      | MLCC
      | 1 µF
  C32 : fl_lib/Electrical/Electrical Elements/Capacitor  Description=|  c=1e-06 F  r=1e-6 Ohm  g=0 1/Ohm  i_specify=off  i_priority=None  i=0 A  i_nominal_specify=off  i_nominal_value=1  i_nominal_unit=A  v_specify=off  v_priority=None  v=0 V  v_nominal_specify=off  v_nominal_value=1  v_nominal_unit=V  vc_specify=off  vc_priority=High  vc=0 V  vc_nominal_specify=off  vc_nominal_value=1  vc_nominal_unit=V
      | この回路での名前　　; C32
      | 部品名　　　　　　　; GRM21BR71H105KA12L
      | この回路での役割　　; 上側ゲートドライバU8がQ1をオンにする瞬間に、ゲートへ送る電荷を近くで供給するためのコンデンサ。
      | ここでの動き　　　　; U8の電源H12と、その基準となるSWの間に1 µFを置く。SWと一緒に電位が動く上側専用の電源を支えるもので、共通GNDへ戻す下側用のC33とは接続を分ける。
      | 
      | 【詳しい働き・仕様・接続・確認の範囲】
      | 部品種別　　　　　　; 積層セラミックコンデンサ（MLCC）
      | 部品分類　　　　　　; 積層セラミックコンデンサ（MLCC）
      | 公称値　　　　　　　; 1uF 50V X7R
      | 配置目的　　　　　　; 光ゲートドライバ局所バイパス。対象ICはU8（ACPL-P346-560E）。
      | 意図する動作　　　　; C32はH12–SW、C33はP12–GND。VCC/VEE直近。 Q1/Q2のゲート電荷供給。U10出力bulkとIC間配線の影響が異なる。高低の帰路を共有してはならない。
      | 端子と接続　　　　　; 1 1 → H12、2 2 → SW
      | モデルの範囲　　　　; Simscape標準コンデンサの集中定数表現。材質、DCバイアス、周波数依存ESR/ESL、寿命・温度特性を型番から自動再現するモデルではない。
      | モデル設定　　　　　; c=1 µF、r=1 µΩ、g=0 S。これらは保存モデルの設定値であり、すべてが実部品の保証値という意味ではない。
      | 損失の扱い　　　　　; 保存モデルの直列抵抗rと実部品の周波数・温度依存ESRは区別する。容量値が一致しても損失・リプル電流・寿命の成立確認にはならない。
      | 確認の範囲　　　　　; 本説明は保存回路の部品情報・端子割当・既存設計意図を整理したもの。今回の説明更新によって新たな動作試験や実機検証を実施した意味ではない。
      | 設計記録　　　　　　; evaluation\component_annotations_20261022_r01\before_graph.json
      | evaluation\component_annotations_20261022_r01\before_metadata.json
      | evaluation\protection_capacitor_integration_20261021_r01\final_delivery\independent_readback\physical_bom.json
      | evaluation\protection_capacitor_integration_20261021_r01\capacitor_review\capacitor_inventory_after_c04.json
      | evaluation\layout_readability_20261022_r01\capacitor_review\exact_snapshot_capacitor_review.json
      | 
      | 【周波数・ノイズと配置の説明】
      | 周波数面の役割　　　; U8がQ1のゲートを充電する瞬間に、ドライバ直近から電流を供給する。
      | 対象周波数の目安　　; 主スイッチング周期で繰り返す短いゲート電流パルスと、その高周波成分を対象とする。主電力段の既存比較計算では50 kHzを仮定している。これは比較シナリオの値であり、今回の保存図から実行中PWM周波数を測定した値ではない。 ゲート電流の速さは繰返し周波数だけでは決まらない。
      | ノイズの発生源　　　; U8がQ1をオンにするときにゲート電荷を充電し、電源電流が短時間だけ増える。電源配線の寄生成分はこの変化を電圧変動にする。
      | 他のコンデンサとの差; 上流電源の22 µFや470 µFは平均的/比較的長い変化を補う。本品1 µFはドライバ直近の短い経路を担当。帰路はSWであり、高側と低側を混同しない。
      | 周波数説明の範囲　　; 狙うノイズの周波数と、この部品が実装後に有効な周波数範囲は別である。実効容量、等価直列抵抗、等価直列インダクタンス、配線を含む自己共振で変わるため、型番名や公称容量だけから有効帯域の上限を断定しない。
      | 周波数説明の根拠　　; Broadcom：ACPL-P346/ACPL-W346
      | https://docs.broadcom.com/doc/AV02-4078EN
      | TDK：Low-ESL Multilayer Ceramic Capacitors
      | https://product.tdk.com/system/files/dam/doc/content/emc-guidebook/en/eemc_product_01.pdf
      | 村田製作所：コンデンサを使いこなす
      | https://www.murata.com/en-GB/products/emc/emifil/library/knowhow/basic/chapter06-p8
      | 
      | 【この説明欄の略語・記号】
      | 用語1　　　　　　　 ; MLCC：Multilayer Ceramic Capacitor（積層セラミックコンデンサ）。薄いセラミック誘電体と電極を重ねたコンデンサ。対象周波数は容量・実装・寄生成分で変わるため、MLCCという分類だけでは決めない。
      | 用語2　　　　　　　 ; ESR：Equivalent Series Resistance（等価直列抵抗）。コンデンサの損失を直列抵抗で表した量。周波数・温度で変わり、損失とリプル電圧に関係する。
      | 用語3　　　　　　　 ; ESL：Equivalent Series Inductance（等価直列インダクタンス）。端子や電極などの寄生インダクタンスを表す。高い周波数ではバイパス効果を制限する。
      | 用語4　　　　　　　 ; DC：Direct Current（直流）。ここでは直流電源または直流成分。DCバイアスはコンデンサに重なる直流電圧を指す。
      | 用語5　　　　　　　 ; X7R：セラミックコンデンサの温度特性記号。英語の頭文字ではなく分類コード。X＝下限−55 ℃、7＝上限+125 ℃、R＝その範囲の容量変化±15%。直流バイアスによる容量変化は別に確認する。
      | 用語6　　　　　　　 ; IC：Integrated Circuit（集積回路）。複数の電子素子と機能を小さな半導体チップに集積した部品。
      | 用語7　　　　　　　 ; PWM：Pulse Width Modulation（パルス幅変調）。周期に対するON時間の割合を変えて、スイッチの平均的な電力伝達を調整する方式。
      | 用語8　　　　　　　 ; MOSFET：Metal-Oxide-Semiconductor Field-Effect Transistor（金属・酸化膜・半導体構造の電界効果トランジスタ）。ゲートとソースの電圧でドレインとソースの導通を制御する素子。N-MOSはNチャネル型を表す。
      | 用語9　　　　　　　 ; GND：Ground（回路の基準電位・電流帰路）。この図の共通基準。保護接地や大地への接続を意味するとは限らない。
      | 用語10　　　　　　　; VCC/VDD/VEE/VS：ICの電源端子名。文字の歴史的な由来を現在の接続機能へ当てはめない。現回路のVEEはU8/U10では浮動基準SW、U9ではGND。各電圧・基準は端子と接続を参照する。
      | 用語11　　　　　　　; SW：Switching Node（スイッチング点）。主電力段の上下MOSFETとL1がつながる、電圧が高速に切り替わる点。GNDとは別電位。
      settings: AttributesFormatString=|
      | MLCC
      | 1 µF
  C33 : fl_lib/Electrical/Electrical Elements/Capacitor  Description=|  c=1e-06 F  r=1e-6 Ohm  g=0 1/Ohm  i_specify=off  i_priority=None  i=0 A  i_nominal_specify=off  i_nominal_value=1  i_nominal_unit=A  v_specify=off  v_priority=None  v=0 V  v_nominal_specify=off  v_nominal_value=1  v_nominal_unit=V  vc_specify=off  vc_priority=High  vc=0 V  vc_nominal_specify=off  vc_nominal_value=1  vc_nominal_unit=V
      | この回路での名前　　; C33
      | 部品名　　　　　　　; GRM21BR71H105KA12L
      | この回路での役割　　; 下側ゲートドライバU9がQ2をオンにする瞬間に、ゲートへ送る電荷を近くで供給するためのコンデンサ。
      | ここでの動き　　　　; U9の12 V電源P12と共通GNDの間に1 µFを置き、ゲート駆動に必要な短い電流をドライバの近くで補う。上側用のC32と異なり、こちらの基準は共通GND。
      | 
      | 【詳しい働き・仕様・接続・確認の範囲】
      | 部品種別　　　　　　; 積層セラミックコンデンサ（MLCC）
      | 部品分類　　　　　　; 積層セラミックコンデンサ（MLCC）
      | 公称値　　　　　　　; 1uF 50V X7R
      | 配置目的　　　　　　; 光ゲートドライバ局所バイパス。対象ICはU9（ACPL-P346-560E）。
      | 意図する動作　　　　; C32はH12–SW、C33はP12–GND。VCC/VEE直近。 Q1/Q2のゲート電荷供給。U10出力bulkとIC間配線の影響が異なる。高低の帰路を共有してはならない。
      | 端子と接続　　　　　; 1 1 → P12、2 2 → GND
      | モデルの範囲　　　　; Simscape標準コンデンサの集中定数表現。材質、DCバイアス、周波数依存ESR/ESL、寿命・温度特性を型番から自動再現するモデルではない。
      | モデル設定　　　　　; c=1 µF、r=1 µΩ、g=0 S。これらは保存モデルの設定値であり、すべてが実部品の保証値という意味ではない。
      | 損失の扱い　　　　　; 保存モデルの直列抵抗rと実部品の周波数・温度依存ESRは区別する。容量値が一致しても損失・リプル電流・寿命の成立確認にはならない。
      | 確認の範囲　　　　　; 本説明は保存回路の部品情報・端子割当・既存設計意図を整理したもの。今回の説明更新によって新たな動作試験や実機検証を実施した意味ではない。
      | 設計記録　　　　　　; evaluation\component_annotations_20261022_r01\before_graph.json
      | evaluation\component_annotations_20261022_r01\before_metadata.json
      | evaluation\protection_capacitor_integration_20261021_r01\final_delivery\independent_readback\physical_bom.json
      | evaluation\protection_capacitor_integration_20261021_r01\capacitor_review\capacitor_inventory_after_c04.json
      | evaluation\layout_readability_20261022_r01\capacitor_review\exact_snapshot_capacitor_review.json
      | 
      | 【周波数・ノイズと配置の説明】
      | 周波数面の役割　　　; U9がQ2のゲートを充電する瞬間に、ドライバ直近から電流を供給する。
      | 対象周波数の目安　　; 主スイッチング周期で繰り返す短いゲート電流パルスと、その高周波成分を対象とする。主電力段の既存比較計算では50 kHzを仮定している。これは比較シナリオの値であり、今回の保存図から実行中PWM周波数を測定した値ではない。 ゲート電流の速さは繰返し周波数だけでは決まらない。
      | ノイズの発生源　　　; U9がQ2をオンにするときにゲート電荷を充電し、電源電流が短時間だけ増える。電源配線の寄生成分はこの変化を電圧変動にする。
      | 他のコンデンサとの差; 上流電源の22 µFや470 µFは平均的/比較的長い変化を補う。本品1 µFはドライバ直近の短い経路を担当。帰路はGNDであり、高側と低側を混同しない。
      | 周波数説明の範囲　　; 狙うノイズの周波数と、この部品が実装後に有効な周波数範囲は別である。実効容量、等価直列抵抗、等価直列インダクタンス、配線を含む自己共振で変わるため、型番名や公称容量だけから有効帯域の上限を断定しない。
      | 周波数説明の根拠　　; Broadcom：ACPL-P346/ACPL-W346
      | https://docs.broadcom.com/doc/AV02-4078EN
      | TDK：Low-ESL Multilayer Ceramic Capacitors
      | https://product.tdk.com/system/files/dam/doc/content/emc-guidebook/en/eemc_product_01.pdf
      | 村田製作所：コンデンサを使いこなす
      | https://www.murata.com/en-GB/products/emc/emifil/library/knowhow/basic/chapter06-p8
      | 
      | 【この説明欄の略語・記号】
      | 用語1　　　　　　　 ; MLCC：Multilayer Ceramic Capacitor（積層セラミックコンデンサ）。薄いセラミック誘電体と電極を重ねたコンデンサ。対象周波数は容量・実装・寄生成分で変わるため、MLCCという分類だけでは決めない。
      | 用語2　　　　　　　 ; ESR：Equivalent Series Resistance（等価直列抵抗）。コンデンサの損失を直列抵抗で表した量。周波数・温度で変わり、損失とリプル電圧に関係する。
      | 用語3　　　　　　　 ; ESL：Equivalent Series Inductance（等価直列インダクタンス）。端子や電極などの寄生インダクタンスを表す。高い周波数ではバイパス効果を制限する。
      | 用語4　　　　　　　 ; DC：Direct Current（直流）。ここでは直流電源または直流成分。DCバイアスはコンデンサに重なる直流電圧を指す。
      | 用語5　　　　　　　 ; X7R：セラミックコンデンサの温度特性記号。英語の頭文字ではなく分類コード。X＝下限−55 ℃、7＝上限+125 ℃、R＝その範囲の容量変化±15%。直流バイアスによる容量変化は別に確認する。
      | 用語6　　　　　　　 ; IC：Integrated Circuit（集積回路）。複数の電子素子と機能を小さな半導体チップに集積した部品。
      | 用語7　　　　　　　 ; PWM：Pulse Width Modulation（パルス幅変調）。周期に対するON時間の割合を変えて、スイッチの平均的な電力伝達を調整する方式。
      | 用語8　　　　　　　 ; MOSFET：Metal-Oxide-Semiconductor Field-Effect Transistor（金属・酸化膜・半導体構造の電界効果トランジスタ）。ゲートとソースの電圧でドレインとソースの導通を制御する素子。N-MOSはNチャネル型を表す。
      | 用語9　　　　　　　 ; GND：Ground（回路の基準電位・電流帰路）。この図の共通基準。保護接地や大地への接続を意味するとは限らない。
      | 用語10　　　　　　　; VCC/VDD/VEE/VS：ICの電源端子名。文字の歴史的な由来を現在の接続機能へ当てはめない。現回路のVEEはU8/U10では浮動基準SW、U9ではGND。各電圧・基準は端子と接続を参照する。
      | 用語11　　　　　　　; SW：Switching Node（スイッチング点）。主電力段の上下MOSFETとL1がつながる、電圧が高速に切り替わる点。GNDとは別電位。
      settings: AttributesFormatString=|
      | MLCC
      | 1 µF
  C34 : fl_lib/Electrical/Electrical Elements/Capacitor  Description=|  c=2.2e-05 F  r=1e-6 Ohm  g=0 1/Ohm  i_specify=off  i_priority=None  i=0 A  i_nominal_specify=off  i_nominal_value=1  i_nominal_unit=A  v_specify=off  v_priority=None  v=0 V  v_nominal_specify=off  v_nominal_value=1  v_nominal_unit=V  vc_specify=off  vc_priority=High  vc=0 V  vc_nominal_specify=off  vc_nominal_value=1  vc_nominal_unit=V
      | この回路での名前　　; C34
      | 部品名　　　　　　　; GRM32ER71E226KE15L
      | この回路での役割　　; 上側ゲート駆動用の絶縁電源U10へ入る12 Vを支え、入力電流の変化を近くで受け止めるためのコンデンサ。
      | ここでの動き　　　　; U10の入力側P12と共通GNDの間に22 µFを2個並列に置き、U10が電流を必要とするときの電荷を補う。すぐ近くのC36は、より速い電流の短い帰り道を分担する。
      | 
      | 【詳しい働き・仕様・接続・確認の範囲】
      | 部品種別　　　　　　; 積層セラミックコンデンサ（MLCC）
      | 部品分類　　　　　　; 積層セラミックコンデンサ（MLCC）
      | 公称値　　　　　　　; 22uF 25V X7R
      | 配置目的　　　　　　; 絶縁DC/DC入力バルク。対象ICはU10（UCC14131QDWNRQ1）。
      | 意図する動作　　　　; U10一次側のVIN/GNDP直近、C36と並列。 TIピン表2×10µFとDCbiasを考慮した2×22µFを維持。C45遠方との単純共用は不可。
      | 端子と接続　　　　　; 1 1 → P12、2 2 → GND
      | モデルの範囲　　　　; Simscape標準コンデンサの集中定数表現。材質、DCバイアス、周波数依存ESR/ESL、寿命・温度特性を型番から自動再現するモデルではない。
      | モデル設定　　　　　; c=22 µF、r=1 µΩ、g=0 S。これらは保存モデルの設定値であり、すべてが実部品の保証値という意味ではない。
      | 損失の扱い　　　　　; 保存モデルの直列抵抗rと実部品の周波数・温度依存ESRは区別する。容量値が一致しても損失・リプル電流・寿命の成立確認にはならない。
      | 確認の範囲　　　　　; 本説明は保存回路の部品情報・端子割当・既存設計意図を整理したもの。今回の説明更新によって新たな動作試験や実機検証を実施した意味ではない。
      | 設計記録　　　　　　; evaluation\component_annotations_20261022_r01\before_graph.json
      | evaluation\component_annotations_20261022_r01\before_metadata.json
      | evaluation\protection_capacitor_integration_20261021_r01\final_delivery\independent_readback\physical_bom.json
      | evaluation\protection_capacitor_integration_20261021_r01\capacitor_review\capacitor_inventory_after_c04.json
      | evaluation\layout_readability_20261022_r01\capacitor_review\exact_snapshot_capacitor_review.json
      | 
      | 【周波数・ノイズと配置の説明】
      | 周波数面の役割　　　; 絶縁電源U10の一次側へ局所的な電荷を供給するバルク。
      | 対象周波数の目安　　; U10の入力電流の包絡変動やゲート駆動負荷の変化を受け、C36と周波数成分を分担する。U10の内部スイッチングはメーカー条件で20.5 MHz典型だが、本品22 µFが20.5 MHzの主な経路であるとは断定しない。
      | ノイズの発生源　　　; U10内部の絶縁電力変換と、高側ゲートドライバU8の負荷が変わること。
      | 他のコンデンサとの差; C36=100 nFはU10端子直近の高周波帰路を狙う。本品は同じMLCCでも22 µFの電荷蓄積側で、低い周波数側を分担する。
      | 周波数説明の範囲　　; 狙うノイズの周波数と、この部品が実装後に有効な周波数範囲は別である。実効容量、等価直列抵抗、等価直列インダクタンス、配線を含む自己共振で変わるため、型番名や公称容量だけから有効帯域の上限を断定しない。
      | 周波数説明の根拠　　; TI：UCC14131-Q1、SLUSF12A
      | https://www.ti.com/lit/ds/symlink/ucc14131-q1.pdf
      | 村田製作所：コンデンサを使いこなす
      | https://www.murata.com/en-GB/products/emc/emifil/library/knowhow/basic/chapter06-p8
      | TDK：電解コンデンサからMLCCへの置換ガイド
      | https://product.tdk.com/en/techlibrary/solutionguide/mlcc_replace-guide.html
      | 
      | 【この説明欄の略語・記号】
      | 用語1　　　　　　　 ; MLCC：Multilayer Ceramic Capacitor（積層セラミックコンデンサ）。薄いセラミック誘電体と電極を重ねたコンデンサ。対象周波数は容量・実装・寄生成分で変わるため、MLCCという分類だけでは決めない。
      | 用語2　　　　　　　 ; ESR：Equivalent Series Resistance（等価直列抵抗）。コンデンサの損失を直列抵抗で表した量。周波数・温度で変わり、損失とリプル電圧に関係する。
      | 用語3　　　　　　　 ; ESL：Equivalent Series Inductance（等価直列インダクタンス）。端子や電極などの寄生インダクタンスを表す。高い周波数ではバイパス効果を制限する。
      | 用語4　　　　　　　 ; DC：Direct Current（直流）。ここでは直流電源または直流成分。DCバイアスはコンデンサに重なる直流電圧を指す。
      | 用語5　　　　　　　 ; DC/DC：DC-to-DC Converter（直流電圧変換器）。直流入力を別の直流電圧へ変換する電源回路。絶縁の有無は個々の部品説明で確認する。
      | 用語6　　　　　　　 ; X7R：セラミックコンデンサの温度特性記号。英語の頭文字ではなく分類コード。X＝下限−55 ℃、7＝上限+125 ℃、R＝その範囲の容量変化±15%。直流バイアスによる容量変化は別に確認する。
      | 用語7　　　　　　　 ; IC：Integrated Circuit（集積回路）。複数の電子素子と機能を小さな半導体チップに集積した部品。
      | 用語8　　　　　　　 ; MOSFET：Metal-Oxide-Semiconductor Field-Effect Transistor（金属・酸化膜・半導体構造の電界効果トランジスタ）。ゲートとソースの電圧でドレインとソースの導通を制御する素子。N-MOSはNチャネル型を表す。
      | 用語9　　　　　　　 ; GND：Ground（回路の基準電位・電流帰路）。この図の共通基準。保護接地や大地への接続を意味するとは限らない。
      | 用語10　　　　　　　; VIN/VOUT：入力電圧・出力電圧を表す端子／ネット名。INは入力、OUTは出力。電源変換器の電力端子なのか、検出用端子なのかは対象部品によって異なるため、端子と接続の説明に従う。
      | 用語11　　　　　　　; VCC/VDD/VEE/VS：ICの電源端子名。文字の歴史的な由来を現在の接続機能へ当てはめない。現回路のVEEはU8/U10では浮動基準SW、U9ではGND。各電圧・基準は端子と接続を参照する。
      | 用語12　　　　　　　; GNDP：U10の一次側電源の基準端子。絶縁電源の入力側GND。二次側基準VEE=SWと直接同一の導体ではない。
      | 用語13　　　　　　　; SW：Switching Node（スイッチング点）。主電力段の上下MOSFETとL1がつながる、電圧が高速に切り替わる点。GNDとは別電位。
      settings: AttributesFormatString=|
      | MLCC
      | 22 µF
  C35 : fl_lib/Electrical/Electrical Elements/Capacitor  Description=|  c=2.2e-05 F  r=1e-6 Ohm  g=0 1/Ohm  i_specify=off  i_priority=None  i=0 A  i_nominal_specify=off  i_nominal_value=1  i_nominal_unit=A  v_specify=off  v_priority=None  v=0 V  v_nominal_specify=off  v_nominal_value=1  v_nominal_unit=V  vc_specify=off  vc_priority=High  vc=0 V  vc_nominal_specify=off  vc_nominal_value=1  vc_nominal_unit=V
      | この回路での名前　　; C35
      | 部品名　　　　　　　; GRM32ER71E226KE15L
      | この回路での役割　　; 上側ゲート駆動用の絶縁電源U10へ入る12 Vを支え、入力電流の変化を近くで受け止めるためのコンデンサ。
      | ここでの動き　　　　; U10の入力側P12と共通GNDの間に22 µFを2個並列に置き、U10が電流を必要とするときの電荷を補う。すぐ近くのC36は、より速い電流の短い帰り道を分担する。
      | 
      | 【詳しい働き・仕様・接続・確認の範囲】
      | 部品種別　　　　　　; 積層セラミックコンデンサ（MLCC）
      | 部品分類　　　　　　; 積層セラミックコンデンサ（MLCC）
      | 公称値　　　　　　　; 22uF 25V X7R
      | 配置目的　　　　　　; 絶縁DC/DC入力バルク。対象ICはU10（UCC14131QDWNRQ1）。
      | 意図する動作　　　　; U10一次側のVIN/GNDP直近、C36と並列。 TIピン表2×10µFとDCbiasを考慮した2×22µFを維持。C45遠方との単純共用は不可。
      | 端子と接続　　　　　; 1 1 → P12、2 2 → GND
      | モデルの範囲　　　　; Simscape標準コンデンサの集中定数表現。材質、DCバイアス、周波数依存ESR/ESL、寿命・温度特性を型番から自動再現するモデルではない。
      | モデル設定　　　　　; c=22 µF、r=1 µΩ、g=0 S。これらは保存モデルの設定値であり、すべてが実部品の保証値という意味ではない。
      | 損失の扱い　　　　　; 保存モデルの直列抵抗rと実部品の周波数・温度依存ESRは区別する。容量値が一致しても損失・リプル電流・寿命の成立確認にはならない。
      | 確認の範囲　　　　　; 本説明は保存回路の部品情報・端子割当・既存設計意図を整理したもの。今回の説明更新によって新たな動作試験や実機検証を実施した意味ではない。
      | 設計記録　　　　　　; evaluation\component_annotations_20261022_r01\before_graph.json
      | evaluation\component_annotations_20261022_r01\before_metadata.json
      | evaluation\protection_capacitor_integration_20261021_r01\final_delivery\independent_readback\physical_bom.json
      | evaluation\protection_capacitor_integration_20261021_r01\capacitor_review\capacitor_inventory_after_c04.json
      | evaluation\layout_readability_20261022_r01\capacitor_review\exact_snapshot_capacitor_review.json
      | 
      | 【周波数・ノイズと配置の説明】
      | 周波数面の役割　　　; 絶縁電源U10の一次側へ局所的な電荷を供給するバルク。
      | 対象周波数の目安　　; U10の入力電流の包絡変動やゲート駆動負荷の変化を受け、C36と周波数成分を分担する。U10の内部スイッチングはメーカー条件で20.5 MHz典型だが、本品22 µFが20.5 MHzの主な経路であるとは断定しない。
      | ノイズの発生源　　　; U10内部の絶縁電力変換と、高側ゲートドライバU8の負荷が変わること。
      | 他のコンデンサとの差; C36=100 nFはU10端子直近の高周波帰路を狙う。本品は同じMLCCでも22 µFの電荷蓄積側で、低い周波数側を分担する。
      | 周波数説明の範囲　　; 狙うノイズの周波数と、この部品が実装後に有効な周波数範囲は別である。実効容量、等価直列抵抗、等価直列インダクタンス、配線を含む自己共振で変わるため、型番名や公称容量だけから有効帯域の上限を断定しない。
      | 周波数説明の根拠　　; TI：UCC14131-Q1、SLUSF12A
      | https://www.ti.com/lit/ds/symlink/ucc14131-q1.pdf
      | 村田製作所：コンデンサを使いこなす
      | https://www.murata.com/en-GB/products/emc/emifil/library/knowhow/basic/chapter06-p8
      | TDK：電解コンデンサからMLCCへの置換ガイド
      | https://product.tdk.com/en/techlibrary/solutionguide/mlcc_replace-guide.html
      | 
      | 【この説明欄の略語・記号】
      | 用語1　　　　　　　 ; MLCC：Multilayer Ceramic Capacitor（積層セラミックコンデンサ）。薄いセラミック誘電体と電極を重ねたコンデンサ。対象周波数は容量・実装・寄生成分で変わるため、MLCCという分類だけでは決めない。
      | 用語2　　　　　　　 ; ESR：Equivalent Series Resistance（等価直列抵抗）。コンデンサの損失を直列抵抗で表した量。周波数・温度で変わり、損失とリプル電圧に関係する。
      | 用語3　　　　　　　 ; ESL：Equivalent Series Inductance（等価直列インダクタンス）。端子や電極などの寄生インダクタンスを表す。高い周波数ではバイパス効果を制限する。
      | 用語4　　　　　　　 ; DC：Direct Current（直流）。ここでは直流電源または直流成分。DCバイアスはコンデンサに重なる直流電圧を指す。
      | 用語5　　　　　　　 ; DC/DC：DC-to-DC Converter（直流電圧変換器）。直流入力を別の直流電圧へ変換する電源回路。絶縁の有無は個々の部品説明で確認する。
      | 用語6　　　　　　　 ; X7R：セラミックコンデンサの温度特性記号。英語の頭文字ではなく分類コード。X＝下限−55 ℃、7＝上限+125 ℃、R＝その範囲の容量変化±15%。直流バイアスによる容量変化は別に確認する。
      | 用語7　　　　　　　 ; IC：Integrated Circuit（集積回路）。複数の電子素子と機能を小さな半導体チップに集積した部品。
      | 用語8　　　　　　　 ; MOSFET：Metal-Oxide-Semiconductor Field-Effect Transistor（金属・酸化膜・半導体構造の電界効果トランジスタ）。ゲートとソースの電圧でドレインとソースの導通を制御する素子。N-MOSはNチャネル型を表す。
      | 用語9　　　　　　　 ; GND：Ground（回路の基準電位・電流帰路）。この図の共通基準。保護接地や大地への接続を意味するとは限らない。
      | 用語10　　　　　　　; VIN/VOUT：入力電圧・出力電圧を表す端子／ネット名。INは入力、OUTは出力。電源変換器の電力端子なのか、検出用端子なのかは対象部品によって異なるため、端子と接続の説明に従う。
      | 用語11　　　　　　　; VCC/VDD/VEE/VS：ICの電源端子名。文字の歴史的な由来を現在の接続機能へ当てはめない。現回路のVEEはU8/U10では浮動基準SW、U9ではGND。各電圧・基準は端子と接続を参照する。
      | 用語12　　　　　　　; GNDP：U10の一次側電源の基準端子。絶縁電源の入力側GND。二次側基準VEE=SWと直接同一の導体ではない。
      | 用語13　　　　　　　; SW：Switching Node（スイッチング点）。主電力段の上下MOSFETとL1がつながる、電圧が高速に切り替わる点。GNDとは別電位。
      settings: AttributesFormatString=|
      | MLCC
      | 22 µF
  C36 : fl_lib/Electrical/Electrical Elements/Capacitor  Description=|  c=1e-07 F  r=1e-6 Ohm  g=0 1/Ohm  i_specify=off  i_priority=None  i=0 A  i_nominal_specify=off  i_nominal_value=1  i_nominal_unit=A  v_specify=off  v_priority=None  v=0 V  v_nominal_specify=off  v_nominal_value=1  v_nominal_unit=V  vc_specify=off  vc_priority=High  vc=0 V  vc_nominal_specify=off  vc_nominal_value=1  vc_nominal_unit=V
      | この回路での名前　　; C36
      | 部品名　　　　　　　; GRM21BR71H104KA01L
      | この回路での役割　　; 絶縁電源U10の入力側で、内部の速いスイッチングに伴う電流を近くで受け止めるためのコンデンサ。
      | ここでの動き　　　　; U10の入力側P12と共通GNDの間に100 nFを置き、端子直近に高周波電流の短い往復経路を作る。C34・C35の大きな電荷蓄積とは、配置と受け持つ変化の速さを分担する設計。
      | 
      | 【詳しい働き・仕様・接続・確認の範囲】
      | 部品種別　　　　　　; 積層セラミックコンデンサ（MLCC）
      | 部品分類　　　　　　; 積層セラミックコンデンサ（MLCC）
      | 公称値　　　　　　　; 100nF 50V X7R
      | 配置目的　　　　　　; 絶縁DC/DC一次側HFバイパス。対象ICはU10（UCC14131QDWNRQ1）。
      | 意図する動作　　　　; U10同面ピン直近、ピン–C間にviaを置かないのがメーカー推奨。0402以下推奨だが現行0805は実装見直し事項。 20MHz級内部スイッチングの局所帰路。bulkで代用不可。
      | 端子と接続　　　　　; 1 1 → P12、2 2 → GND
      | モデルの範囲　　　　; Simscape標準コンデンサの集中定数表現。材質、DCバイアス、周波数依存ESR/ESL、寿命・温度特性を型番から自動再現するモデルではない。
      | モデル設定　　　　　; c=100 nF、r=1 µΩ、g=0 S。これらは保存モデルの設定値であり、すべてが実部品の保証値という意味ではない。
      | 損失の扱い　　　　　; 保存モデルの直列抵抗rと実部品の周波数・温度依存ESRは区別する。容量値が一致しても損失・リプル電流・寿命の成立確認にはならない。
      | 確認の範囲　　　　　; 本説明は保存回路の部品情報・端子割当・既存設計意図を整理したもの。今回の説明更新によって新たな動作試験や実機検証を実施した意味ではない。
      | 設計記録　　　　　　; evaluation\component_annotations_20261022_r01\before_graph.json
      | evaluation\component_annotations_20261022_r01\before_metadata.json
      | evaluation\protection_capacitor_integration_20261021_r01\final_delivery\independent_readback\physical_bom.json
      | evaluation\protection_capacitor_integration_20261021_r01\capacitor_review\capacitor_inventory_after_c04.json
      | evaluation\layout_readability_20261022_r01\capacitor_review\exact_snapshot_capacitor_review.json
      | 
      | 【周波数・ノイズと配置の説明】
      | 周波数面の役割　　　; U10の一次側P12–GNDで、高周波電流の短い帰路を作る100 nFの局所バイパス。
      | 対象周波数の目安　　; U10内部の20.5 MHz典型のスイッチングとその高調波が具体的な検討対象。これは絶縁電源U10内部の変換周波数で、RP2040が主電力段へ出すPWM周波数とは別。20.5 MHzはメーカー指定条件の値であり、本モデルの実測スペクトルではない。
      | ノイズの発生源　　　; U10内蔵の絶縁電力変換回路で高速スイッチングが行われ、電源/出力帰路に高周波電流が生じる。
      | 他のコンデンサとの差; 並列の22 µF群は電荷量を補う。100 nF側は短い実装経路を狙い、TIはIC同面の端子直近・端子との間にビアを置かない配置と0402以下を推奨。現行0805品での実装性能は未確認。
      | 周波数説明の範囲　　; 狙うノイズの周波数と、この部品が実装後に有効な周波数範囲は別である。実効容量、等価直列抵抗、等価直列インダクタンス、配線を含む自己共振で変わるため、型番名や公称容量だけから有効帯域の上限を断定しない。
      | 周波数説明の根拠　　; TI：UCC14131-Q1、SLUSF12A
      | https://www.ti.com/lit/ds/symlink/ucc14131-q1.pdf
      | 村田製作所：コンデンサを使いこなす
      | https://www.murata.com/en-GB/products/emc/emifil/library/knowhow/basic/chapter06-p8
      | 
      | 【この説明欄の略語・記号】
      | 用語1　　　　　　　 ; MLCC：Multilayer Ceramic Capacitor（積層セラミックコンデンサ）。薄いセラミック誘電体と電極を重ねたコンデンサ。対象周波数は容量・実装・寄生成分で変わるため、MLCCという分類だけでは決めない。
      | 用語2　　　　　　　 ; ESR：Equivalent Series Resistance（等価直列抵抗）。コンデンサの損失を直列抵抗で表した量。周波数・温度で変わり、損失とリプル電圧に関係する。
      | 用語3　　　　　　　 ; ESL：Equivalent Series Inductance（等価直列インダクタンス）。端子や電極などの寄生インダクタンスを表す。高い周波数ではバイパス効果を制限する。
      | 用語4　　　　　　　 ; DC：Direct Current（直流）。ここでは直流電源または直流成分。DCバイアスはコンデンサに重なる直流電圧を指す。
      | 用語5　　　　　　　 ; DC/DC：DC-to-DC Converter（直流電圧変換器）。直流入力を別の直流電圧へ変換する電源回路。絶縁の有無は個々の部品説明で確認する。
      | 用語6　　　　　　　 ; HF：High Frequency（高周波）。速い電圧・電流変化に対応する成分。具体的な周波数帯は対象回路ごとに説明する。
      | 用語7　　　　　　　 ; X7R：セラミックコンデンサの温度特性記号。英語の頭文字ではなく分類コード。X＝下限−55 ℃、7＝上限+125 ℃、R＝その範囲の容量変化±15%。直流バイアスによる容量変化は別に確認する。
      | 用語8　　　　　　　 ; IC：Integrated Circuit（集積回路）。複数の電子素子と機能を小さな半導体チップに集積した部品。
      | 用語9　　　　　　　 ; PWM：Pulse Width Modulation（パルス幅変調）。周期に対するON時間の割合を変えて、スイッチの平均的な電力伝達を調整する方式。
      | 用語10　　　　　　　; GND：Ground（回路の基準電位・電流帰路）。この図の共通基準。保護接地や大地への接続を意味するとは限らない。
      settings: AttributesFormatString=|
      | MLCC
      | 100 nF
  C37 : fl_lib/Electrical/Electrical Elements/Capacitor  Description=|  c=2.2e-05 F  r=1e-6 Ohm  g=0 1/Ohm  i_specify=off  i_priority=None  i=0 A  i_nominal_specify=off  i_nominal_value=1  i_nominal_unit=A  v_specify=off  v_priority=None  v=0 V  v_nominal_specify=off  v_nominal_value=1  v_nominal_unit=V  vc_specify=off  vc_priority=High  vc=0 V  vc_nominal_specify=off  vc_nominal_value=1  vc_nominal_unit=V
      | この回路での名前　　; C37
      | 部品名　　　　　　　; GRM32ER71E226KE15L
      | この回路での役割　　; 絶縁電源U10が作る上側ゲート駆動用の約12 Vを支え、U8へ渡す電荷を蓄えるためのコンデンサ。
      | ここでの動き　　　　; U10の出力H12と、上側の基準となるSWの間に22 µFを置く。共通GND側の入力コンデンサとは絶縁の境界を挟むため共用できず、SWと一緒に電位が動く出力側を支える。
      | 
      | 【詳しい働き・仕様・接続・確認の範囲】
      | 部品種別　　　　　　; 積層セラミックコンデンサ（MLCC）
      | 部品分類　　　　　　; 積層セラミックコンデンサ（MLCC）
      | 公称値　　　　　　　; 22uF 25V X7R
      | 配置目的　　　　　　; 絶縁DC/DC二次側バルク。対象ICはU10（UCC14131QDWNRQ1）。
      | 意図する動作　　　　; U10二次側H12–SW、C38と並列。 単一浮動出力。C34/35やGND側容量と共用できない。
      | 端子と接続　　　　　; 1 1 → H12、2 2 → SW
      | モデルの範囲　　　　; Simscape標準コンデンサの集中定数表現。材質、DCバイアス、周波数依存ESR/ESL、寿命・温度特性を型番から自動再現するモデルではない。
      | モデル設定　　　　　; c=22 µF、r=1 µΩ、g=0 S。これらは保存モデルの設定値であり、すべてが実部品の保証値という意味ではない。
      | 損失の扱い　　　　　; 保存モデルの直列抵抗rと実部品の周波数・温度依存ESRは区別する。容量値が一致しても損失・リプル電流・寿命の成立確認にはならない。
      | 確認の範囲　　　　　; 本説明は保存回路の部品情報・端子割当・既存設計意図を整理したもの。今回の説明更新によって新たな動作試験や実機検証を実施した意味ではない。
      | 設計記録　　　　　　; evaluation\component_annotations_20261022_r01\before_graph.json
      | evaluation\component_annotations_20261022_r01\before_metadata.json
      | evaluation\protection_capacitor_integration_20261021_r01\final_delivery\independent_readback\physical_bom.json
      | evaluation\protection_capacitor_integration_20261021_r01\capacitor_review\capacitor_inventory_after_c04.json
      | evaluation\layout_readability_20261022_r01\capacitor_review\exact_snapshot_capacitor_review.json
      | 
      | 【周波数・ノイズと配置の説明】
      | 周波数面の役割　　　; 絶縁電源U10の二次側H12–SWに電荷を蓄え、高側ドライバ負荷に供給する。
      | 対象周波数の目安　　; U10の出力リプルとU8のゲート駆動に伴う負荷変化を対象とする。内部変換の20.5 MHz典型成分はC38と分担し、本品22 µFだけの帯域保証にはしない。
      | ノイズの発生源　　　; U10内部の絶縁電力変換と、高側ゲートQ1を繰り返し充電するU8の電源負荷。
      | 他のコンデンサとの差; C38=100 nFはU10直近の高速帰路、C32=1 µFはU8直近のゲート電荷供給。本品22 µFは二次側の局所蓄積で、それぞれ配置先が異なる。
      | 周波数説明の範囲　　; 狙うノイズの周波数と、この部品が実装後に有効な周波数範囲は別である。実効容量、等価直列抵抗、等価直列インダクタンス、配線を含む自己共振で変わるため、型番名や公称容量だけから有効帯域の上限を断定しない。
      | 周波数説明の根拠　　; TI：UCC14131-Q1、SLUSF12A
      | https://www.ti.com/lit/ds/symlink/ucc14131-q1.pdf
      | Broadcom：ACPL-P346/ACPL-W346
      | https://docs.broadcom.com/doc/AV02-4078EN
      | 村田製作所：コンデンサを使いこなす
      | https://www.murata.com/en-GB/products/emc/emifil/library/knowhow/basic/chapter06-p8
      | 
      | 【この説明欄の略語・記号】
      | 用語1　　　　　　　 ; MLCC：Multilayer Ceramic Capacitor（積層セラミックコンデンサ）。薄いセラミック誘電体と電極を重ねたコンデンサ。対象周波数は容量・実装・寄生成分で変わるため、MLCCという分類だけでは決めない。
      | 用語2　　　　　　　 ; ESR：Equivalent Series Resistance（等価直列抵抗）。コンデンサの損失を直列抵抗で表した量。周波数・温度で変わり、損失とリプル電圧に関係する。
      | 用語3　　　　　　　 ; ESL：Equivalent Series Inductance（等価直列インダクタンス）。端子や電極などの寄生インダクタンスを表す。高い周波数ではバイパス効果を制限する。
      | 用語4　　　　　　　 ; DC：Direct Current（直流）。ここでは直流電源または直流成分。DCバイアスはコンデンサに重なる直流電圧を指す。
      | 用語5　　　　　　　 ; DC/DC：DC-to-DC Converter（直流電圧変換器）。直流入力を別の直流電圧へ変換する電源回路。絶縁の有無は個々の部品説明で確認する。
      | 用語6　　　　　　　 ; X7R：セラミックコンデンサの温度特性記号。英語の頭文字ではなく分類コード。X＝下限−55 ℃、7＝上限+125 ℃、R＝その範囲の容量変化±15%。直流バイアスによる容量変化は別に確認する。
      | 用語7　　　　　　　 ; IC：Integrated Circuit（集積回路）。複数の電子素子と機能を小さな半導体チップに集積した部品。
      | 用語8　　　　　　　 ; MOSFET：Metal-Oxide-Semiconductor Field-Effect Transistor（金属・酸化膜・半導体構造の電界効果トランジスタ）。ゲートとソースの電圧でドレインとソースの導通を制御する素子。N-MOSはNチャネル型を表す。
      | 用語9　　　　　　　 ; GND：Ground（回路の基準電位・電流帰路）。この図の共通基準。保護接地や大地への接続を意味するとは限らない。
      | 用語10　　　　　　　; SW：Switching Node（スイッチング点）。主電力段の上下MOSFETとL1がつながる、電圧が高速に切り替わる点。GNDとは別電位。
      settings: AttributesFormatString=|
      | MLCC
      | 22 µF
  C38 : fl_lib/Electrical/Electrical Elements/Capacitor  Description=|  c=1e-07 F  r=1e-6 Ohm  g=0 1/Ohm  i_specify=off  i_priority=None  i=0 A  i_nominal_specify=off  i_nominal_value=1  i_nominal_unit=A  v_specify=off  v_priority=None  v=0 V  v_nominal_specify=off  v_nominal_value=1  v_nominal_unit=V  vc_specify=off  vc_priority=High  vc=0 V  vc_nominal_specify=off  vc_nominal_value=1  vc_nominal_unit=V
      | この回路での名前　　; C38
      | 部品名　　　　　　　; GRM21BR71H104KA01L
      | この回路での役割　　; 絶縁電源U10の出力側で、内部の速いスイッチングに伴う電流を近くで受け止めるためのコンデンサ。
      | ここでの動き　　　　; U10の出力H12と、上側の基準となるSWの間に100 nFを置き、端子直近に高周波電流の短い往復経路を作る。電荷を多く蓄えるC37やU8の直近にあるC32とは、配置先と役割を分担する。
      | 
      | 【詳しい働き・仕様・接続・確認の範囲】
      | 部品種別　　　　　　; 積層セラミックコンデンサ（MLCC）
      | 部品分類　　　　　　; 積層セラミックコンデンサ（MLCC）
      | 公称値　　　　　　　; 100nF 50V X7R
      | 配置目的　　　　　　; 絶縁DC/DC二次側HFバイパス。対象ICはU10（UCC14131QDWNRQ1）。
      | 意図する動作　　　　; U10同面ピン直近でH12–SWに短い閉路。 C37やC32と作用周波数/局所性が異なる。
      | 端子と接続　　　　　; 1 1 → H12、2 2 → SW
      | モデルの範囲　　　　; Simscape標準コンデンサの集中定数表現。材質、DCバイアス、周波数依存ESR/ESL、寿命・温度特性を型番から自動再現するモデルではない。
      | モデル設定　　　　　; c=100 nF、r=1 µΩ、g=0 S。これらは保存モデルの設定値であり、すべてが実部品の保証値という意味ではない。
      | 損失の扱い　　　　　; 保存モデルの直列抵抗rと実部品の周波数・温度依存ESRは区別する。容量値が一致しても損失・リプル電流・寿命の成立確認にはならない。
      | 確認の範囲　　　　　; 本説明は保存回路の部品情報・端子割当・既存設計意図を整理したもの。今回の説明更新によって新たな動作試験や実機検証を実施した意味ではない。
      | 設計記録　　　　　　; evaluation\component_annotations_20261022_r01\before_graph.json
      | evaluation\component_annotations_20261022_r01\before_metadata.json
      | evaluation\protection_capacitor_integration_20261021_r01\final_delivery\independent_readback\physical_bom.json
      | evaluation\protection_capacitor_integration_20261021_r01\capacitor_review\capacitor_inventory_after_c04.json
      | evaluation\layout_readability_20261022_r01\capacitor_review\exact_snapshot_capacitor_review.json
      | 
      | 【周波数・ノイズと配置の説明】
      | 周波数面の役割　　　; U10の二次側H12–SWで、高周波電流の短い帰路を作る100 nFの局所バイパス。
      | 対象周波数の目安　　; U10内部の20.5 MHz典型のスイッチングとその高調波が具体的な検討対象。これは絶縁電源U10内部の変換周波数で、RP2040が主電力段へ出すPWM周波数とは別。20.5 MHzはメーカー指定条件の値であり、本モデルの実測スペクトルではない。
      | ノイズの発生源　　　; U10内蔵の絶縁電力変換回路で高速スイッチングが行われ、電源/出力帰路に高周波電流が生じる。
      | 他のコンデンサとの差; 並列の22 µF群は電荷量を補う。100 nF側は短い実装経路を狙い、TIはIC同面の端子直近・端子との間にビアを置かない配置と0402以下を推奨。現行0805品での実装性能は未確認。
      | 周波数説明の範囲　　; 狙うノイズの周波数と、この部品が実装後に有効な周波数範囲は別である。実効容量、等価直列抵抗、等価直列インダクタンス、配線を含む自己共振で変わるため、型番名や公称容量だけから有効帯域の上限を断定しない。
      | 周波数説明の根拠　　; TI：UCC14131-Q1、SLUSF12A
      | https://www.ti.com/lit/ds/symlink/ucc14131-q1.pdf
      | 村田製作所：コンデンサを使いこなす
      | https://www.murata.com/en-GB/products/emc/emifil/library/knowhow/basic/chapter06-p8
      | 
      | 【この説明欄の略語・記号】
      | 用語1　　　　　　　 ; MLCC：Multilayer Ceramic Capacitor（積層セラミックコンデンサ）。薄いセラミック誘電体と電極を重ねたコンデンサ。対象周波数は容量・実装・寄生成分で変わるため、MLCCという分類だけでは決めない。
      | 用語2　　　　　　　 ; ESR：Equivalent Series Resistance（等価直列抵抗）。コンデンサの損失を直列抵抗で表した量。周波数・温度で変わり、損失とリプル電圧に関係する。
      | 用語3　　　　　　　 ; ESL：Equivalent Series Inductance（等価直列インダクタンス）。端子や電極などの寄生インダクタンスを表す。高い周波数ではバイパス効果を制限する。
      | 用語4　　　　　　　 ; DC：Direct Current（直流）。ここでは直流電源または直流成分。DCバイアスはコンデンサに重なる直流電圧を指す。
      | 用語5　　　　　　　 ; DC/DC：DC-to-DC Converter（直流電圧変換器）。直流入力を別の直流電圧へ変換する電源回路。絶縁の有無は個々の部品説明で確認する。
      | 用語6　　　　　　　 ; HF：High Frequency（高周波）。速い電圧・電流変化に対応する成分。具体的な周波数帯は対象回路ごとに説明する。
      | 用語7　　　　　　　 ; X7R：セラミックコンデンサの温度特性記号。英語の頭文字ではなく分類コード。X＝下限−55 ℃、7＝上限+125 ℃、R＝その範囲の容量変化±15%。直流バイアスによる容量変化は別に確認する。
      | 用語8　　　　　　　 ; IC：Integrated Circuit（集積回路）。複数の電子素子と機能を小さな半導体チップに集積した部品。
      | 用語9　　　　　　　 ; PWM：Pulse Width Modulation（パルス幅変調）。周期に対するON時間の割合を変えて、スイッチの平均的な電力伝達を調整する方式。
      | 用語10　　　　　　　; MOSFET：Metal-Oxide-Semiconductor Field-Effect Transistor（金属・酸化膜・半導体構造の電界効果トランジスタ）。ゲートとソースの電圧でドレインとソースの導通を制御する素子。N-MOSはNチャネル型を表す。
      | 用語11　　　　　　　; GND：Ground（回路の基準電位・電流帰路）。この図の共通基準。保護接地や大地への接続を意味するとは限らない。
      | 用語12　　　　　　　; SW：Switching Node（スイッチング点）。主電力段の上下MOSFETとL1がつながる、電圧が高速に切り替わる点。GNDとは別電位。
      settings: AttributesFormatString=|
      | MLCC
      | 100 nF
  C39 : fl_lib/Electrical/Electrical Elements/Capacitor  Description=|  c=3.3e-10 F  r=1e-6 Ohm  g=0 1/Ohm  i_specify=off  i_priority=None  i=0 A  i_nominal_specify=off  i_nominal_value=1  i_nominal_unit=A  v_specify=off  v_priority=None  v=0 V  v_nominal_specify=off  v_nominal_value=1  v_nominal_unit=V  vc_specify=off  vc_priority=High  vc=0 V  vc_nominal_specify=off  vc_nominal_value=1  vc_nominal_unit=V
      | この回路での名前　　; C39
      | 部品名　　　　　　　; C0805C331J5GACTU
      | この回路での役割　　; 絶縁電源U10が自分の出力電圧を読み取る信号から、速い揺れを減らすためのコンデンサ。
      | ここでの動き　　　　; 出力電圧をR45・R46で下げた帰還信号H_FBと、その基準SWの間に330 pFを置く。電源の電荷を蓄える部品ではなく、U10の電圧調整へ戻す信号を整える部品。
      | 
      | 【詳しい働き・仕様・接続・確認の範囲】
      | 部品種別　　　　　　; 積層セラミックコンデンサ（MLCC）
      | 部品分類　　　　　　; 積層セラミックコンデンサ（MLCC）
      | 公称値　　　　　　　; 330pF 50V C0G 5%
      | 配置目的　　　　　　; 浮動出力フィードバックフィルタ。対象ICはU10（UCC14131QDWNRQ1）。
      | 意図する動作　　　　; H_FB–SW、U10FB端子直近、SW基準を汚さない。 安定性・誤検出に関わる330pF。バイパス群と集約しない。
      | 端子と接続　　　　　; 1 1 → H_FB、2 2 → SW
      | モデルの範囲　　　　; Simscape標準コンデンサの集中定数表現。材質、DCバイアス、周波数依存ESR/ESL、寿命・温度特性を型番から自動再現するモデルではない。
      | モデル設定　　　　　; c=330 pF、r=1 µΩ、g=0 S。これらは保存モデルの設定値であり、すべてが実部品の保証値という意味ではない。
      | 損失の扱い　　　　　; 保存モデルの直列抵抗rと実部品の周波数・温度依存ESRは区別する。容量値が一致しても損失・リプル電流・寿命の成立確認にはならない。
      | 確認の範囲　　　　　; 本説明は保存回路の部品情報・端子割当・既存設計意図を整理したもの。今回の説明更新によって新たな動作試験や実機検証を実施した意味ではない。
      | 設計記録　　　　　　; evaluation\component_annotations_20261022_r01\before_graph.json
      | evaluation\component_annotations_20261022_r01\before_metadata.json
      | evaluation\protection_capacitor_integration_20261021_r01\final_delivery\independent_readback\physical_bom.json
      | evaluation\protection_capacitor_integration_20261021_r01\capacitor_review\capacitor_inventory_after_c04.json
      | evaluation\layout_readability_20261022_r01\capacitor_review\exact_snapshot_capacitor_review.json
      | 
      | 【周波数・ノイズと配置の説明】
      | 周波数面の役割　　　; U10の出力電圧を読み取る帰還端子の速い電圧変化を抑える。
      | 対象周波数の目安　　; R45=38.3 kΩとR46=10 kΩを理想電圧源に対する合成抵抗とし、330 pFだけを見ると約60.8 kHzの1次極を作る。これは帰還回路の要素であり、U10全体の制御帯域や安定性をこの値だけでは決められない。
      | ノイズの発生源　　　; H12出力のスイッチングリプル、U10の内部20.5 MHz典型成分や主電力段SWからの寄生結合が帰還配線へ入る可能性。
      | 他のコンデンサとの差; C37/C38は電源電流を流す容量。本品330 pFは帰還信号を扱う小容量で、大容量バイパスへ置き換えると制御応答も変わる。
      | 周波数説明の範囲　　; 約60.8 kHzは公称値による独立した1次RC計算。IC入力の特性、全制御ループ、配線寄生を含む安定性判定ではない。
      | 周波数説明の根拠　　; TI：UCC14131-Q1、SLUSF12A
      | https://www.ti.com/lit/ds/symlink/ucc14131-q1.pdf
      | 
      | 【この説明欄の略語・記号】
      | 用語1　　　　　　　 ; MLCC：Multilayer Ceramic Capacitor（積層セラミックコンデンサ）。薄いセラミック誘電体と電極を重ねたコンデンサ。対象周波数は容量・実装・寄生成分で変わるため、MLCCという分類だけでは決めない。
      | 用語2　　　　　　　 ; ESR：Equivalent Series Resistance（等価直列抵抗）。コンデンサの損失を直列抵抗で表した量。周波数・温度で変わり、損失とリプル電圧に関係する。
      | 用語3　　　　　　　 ; ESL：Equivalent Series Inductance（等価直列インダクタンス）。端子や電極などの寄生インダクタンスを表す。高い周波数ではバイパス効果を制限する。
      | 用語4　　　　　　　 ; DC：Direct Current（直流）。ここでは直流電源または直流成分。DCバイアスはコンデンサに重なる直流電圧を指す。
      | 用語5　　　　　　　 ; C0G：温度補償系セラミックコンデンサの温度特性記号。英語の頭文字ではなく分類コード。−55〜+125 ℃で容量の温度係数が0±30 ppm/℃の特性を表す。ppmはparts per million（100万分の1）で、30 ppm/℃は1 ℃当たり0.003%に相当する。
      | 用語6　　　　　　　 ; IC：Integrated Circuit（集積回路）。複数の電子素子と機能を小さな半導体チップに集積した部品。
      | 用語7　　　　　　　 ; MOSFET：Metal-Oxide-Semiconductor Field-Effect Transistor（金属・酸化膜・半導体構造の電界効果トランジスタ）。ゲートとソースの電圧でドレインとソースの導通を制御する素子。N-MOSはNチャネル型を表す。
      | 用語8　　　　　　　 ; RC：Resistor-Capacitor（抵抗とコンデンサの組合せ）。主に測定信号のフィルタや時定数を作る。カットオフ周波数は実際の接続と抵抗・容量から求める。
      | 用語9　　　　　　　 ; GND：Ground（回路の基準電位・電流帰路）。この図の共通基準。保護接地や大地への接続を意味するとは限らない。
      | 用語10　　　　　　　; FB：Feedback（帰還）。出力などを検出して内部制御へ戻すための信号・端子。
      | 用語11　　　　　　　; SW：Switching Node（スイッチング点）。主電力段の上下MOSFETとL1がつながる、電圧が高速に切り替わる点。GNDとは別電位。
      settings: AttributesFormatString=|
      | MLCC
      | 330 pF
  C4 : fl_lib/Electrical/Electrical Elements/Capacitor  Description=|  c=0.00046999999999999999 F  r=1e-6 Ohm  g=0 1/Ohm  i_specify=off  i_priority=None  i=0 A  i_nominal_specify=off  i_nominal_value=1  i_nominal_unit=A  v_specify=off  v_priority=None  v=0 V  v_nominal_specify=off  v_nominal_value=1  v_nominal_unit=V  vc_specify=off  vc_priority=High  vc=0 V  vc_nominal_specify=off  vc_nominal_value=1  vc_nominal_unit=V
      | この回路での名前　　; C4
      | 部品名　　　　　　　; UCY2C471MHD
      | この回路での役割　　; 太陽光パネルから給電される主電力段の入力側に電荷を蓄え、入力電圧の落ち込みや変動を抑えるためのコンデンサ。
      | ここでの動き　　　　; 入力電源VINと共通GNDの間に470 µFを3個並列に置き、降圧回路が電流を必要とするときに電荷を補う。速い変化への対応は、近くのC7〜C10と分担する設計。
      | 
      | 【詳しい働き・仕様・接続・確認の範囲】
      | 部品種別　　　　　　; アルミ電解コンデンサ（有極性）
      | 部品分類　　　　　　; アルミ電解コンデンサ（有極性）
      | 公称値　　　　　　　; 470 uF
      | 配置目的　　　　　　; 入力バルク。対象はL2入力フィルタとQ1/Q2電力段。
      | 意図する動作　　　　; VIN–GND間の入力バルクとして、降圧電力段が必要とする電荷を供給し入力電圧変動を抑える。現構成は470 µFを3個。分流・ESR・温度上昇・配線寄生の適合は別評価。
      | 端子と接続　　　　　; 2 n → GND、1 p → VIN
      | モデルの範囲　　　　; Simscape標準コンデンサの集中定数表現。材質、DCバイアス、周波数依存ESR/ESL、寿命・温度特性を型番から自動再現するモデルではない。
      | モデル設定　　　　　; c=470 µF、r=1 µΩ、g=0 S。これらは保存モデルの設定値であり、すべてが実部品の保証値という意味ではない。
      | 損失の扱い　　　　　; 保存モデルの直列抵抗rと実部品の周波数・温度依存ESRは区別する。容量値が一致しても損失・リプル電流・寿命の成立確認にはならない。
      | 確認の範囲　　　　　; 本説明は保存回路の部品情報・端子割当・既存設計意図を整理したもの。今回の説明更新によって新たな動作試験や実機検証を実施した意味ではない。
      | 設計記録　　　　　　; evaluation\component_annotations_20261022_r01\before_graph.json
      | evaluation\component_annotations_20261022_r01\before_metadata.json
      | evaluation\protection_capacitor_integration_20261021_r01\final_delivery\independent_readback\physical_bom.json
      | evaluation\protection_capacitor_integration_20261021_r01\capacitor_review\capacitor_inventory_after_c04.json
      | 
      | 【周波数・ノイズと配置の説明】
      | 周波数面の役割　　　; 入力電圧の比較的ゆっくりした変動を抑え、主電力段が必要な電荷を蓄える。
      | 対象周波数の目安　　; 起動・日射/負荷変動などの低い周波数側から、主スイッチング周期の電荷出入りまでを受け持つ。主電力段の既存比較計算では50 kHzを仮定している。これは比較シナリオの値であり、今回の保存図から実行中PWM周波数を測定した値ではない。
      | ノイズの発生源　　　; Q1のオン期間に入力から電流を取り出すため、入力電流は脈動する。パネル/配線/L2側がすぐ補えない電流をこの容量群が補う。
      | 他のコンデンサとの差; 470 µF×3個の電解は蓄積量を担当する。C7のフィルムとC8～C10のMLCCは速い電流変化への局所経路を補う。同じ周波数で複数群が分担し、境界周波数で役割が切り替わるわけではない。
      | 周波数説明の範囲　　; 狙うノイズの周波数と、この部品が実装後に有効な周波数範囲は別である。実効容量、等価直列抵抗、等価直列インダクタンス、配線を含む自己共振で変わるため、型番名や公称容量だけから有効帯域の上限を断定しない。
      | 周波数説明の根拠　　; 村田製作所：コンデンサのインピーダンス・ESRと周波数の関係
      | https://article.murata.com/en-global/article/impedance-esr-frequency-characteristics-in-capacitors
      | 村田製作所：コンデンサを使いこなす
      | https://www.murata.com/en-GB/products/emc/emifil/library/knowhow/basic/chapter06-p8
      | 
      | 【この説明欄の略語・記号】
      | 用語1　　　　　　　 ; MLCC：Multilayer Ceramic Capacitor（積層セラミックコンデンサ）。薄いセラミック誘電体と電極を重ねたコンデンサ。対象周波数は容量・実装・寄生成分で変わるため、MLCCという分類だけでは決めない。
      | 用語2　　　　　　　 ; ESR：Equivalent Series Resistance（等価直列抵抗）。コンデンサの損失を直列抵抗で表した量。周波数・温度で変わり、損失とリプル電圧に関係する。
      | 用語3　　　　　　　 ; ESL：Equivalent Series Inductance（等価直列インダクタンス）。端子や電極などの寄生インダクタンスを表す。高い周波数ではバイパス効果を制限する。
      | 用語4　　　　　　　 ; DC：Direct Current（直流）。ここでは直流電源または直流成分。DCバイアスはコンデンサに重なる直流電圧を指す。
      | 用語5　　　　　　　 ; PWM：Pulse Width Modulation（パルス幅変調）。周期に対するON時間の割合を変えて、スイッチの平均的な電力伝達を調整する方式。
      | 用語6　　　　　　　 ; GND：Ground（回路の基準電位・電流帰路）。この図の共通基準。保護接地や大地への接続を意味するとは限らない。
      | 用語7　　　　　　　 ; VIN/VOUT：入力電圧・出力電圧を表す端子／ネット名。INは入力、OUTは出力。電源変換器の電力端子なのか、検出用端子なのかは対象部品によって異なるため、端子と接続の説明に従う。
      settings: AttributesFormatString=|
      | 電解
      | 470 µF
  C40 : fl_lib/Electrical/Electrical Elements/Capacitor  Description=|  c=2.2e-06 F  r=1e-6 Ohm  g=0 1/Ohm  i_specify=off  i_priority=None  i=0 A  i_nominal_specify=off  i_nominal_value=1  i_nominal_unit=A  v_specify=off  v_priority=None  v=0 V  v_nominal_specify=off  v_nominal_value=1  v_nominal_unit=V  vc_specify=off  vc_priority=High  vc=0 V  vc_nominal_specify=off  vc_nominal_value=1  vc_nominal_unit=V
      | この回路での名前　　; C40
      | 部品名　　　　　　　; C1210X225K1RACAUTO
      | この回路での役割　　; バッテリーから12 Vを作る補助電源U11の入力を支え、電流の脈動を近くで受け止めるためのコンデンサ。
      | ここでの動き　　　　; U11へ入るバッテリー側電源BAT_AUXと共通GNDの間に、2.2 µFを5個並列に置いて入力電荷を補う。5個が必要最小数かどうかはまだ確定していない。
      | 
      | 【詳しい働き・仕様・接続・確認の範囲】
      | 部品種別　　　　　　; 積層セラミックコンデンサ（MLCC）
      | 部品分類　　　　　　; 積層セラミックコンデンサ（MLCC）
      | 公称値　　　　　　　; 2.2uF 100V X7R
      | 配置目的　　　　　　; 12V補助電源入力バイパス群。対象ICはU11（TSR 1-48120WI）。
      | 意図する動作　　　　; U11入力端子付近で給電の瞬間的変動を抑える。現構成は2.2 µF×5個=公称11 µF。5個が最小必要数という根拠は未確認であり、実効容量・入力フィルタ・EMCと合わせた削減評価が残る。
      | 端子と接続　　　　　; 1 1 → BAT_AUX、2 2 → GND
      | モデルの範囲　　　　; Simscape標準コンデンサの集中定数表現。材質、DCバイアス、周波数依存ESR/ESL、寿命・温度特性を型番から自動再現するモデルではない。
      | モデル設定　　　　　; c=2.2 µF、r=1 µΩ、g=0 S。これらは保存モデルの設定値であり、すべてが実部品の保証値という意味ではない。
      | 損失の扱い　　　　　; 保存モデルの直列抵抗rと実部品の周波数・温度依存ESRは区別する。容量値が一致しても損失・リプル電流・寿命の成立確認にはならない。
      | 確認の範囲　　　　　; 本説明は保存回路の部品情報・端子割当・既存設計意図を整理したもの。今回の説明更新によって新たな動作試験や実機検証を実施した意味ではない。
      | 設計記録　　　　　　; evaluation\component_annotations_20261022_r01\before_graph.json
      | evaluation\component_annotations_20261022_r01\before_metadata.json
      | evaluation\protection_capacitor_integration_20261021_r01\final_delivery\independent_readback\physical_bom.json
      | evaluation\protection_capacitor_integration_20261021_r01\capacitor_review\capacitor_inventory_after_c04.json
      | evaluation\layout_readability_20261022_r01\capacitor_review\exact_snapshot_capacitor_review.json
      | 
      | 【周波数・ノイズと配置の説明】
      | 周波数面の役割　　　; 12 V補助電源U11の入力端子近くで、入力電流の脈動に必要な電荷を供給する。
      | 対象周波数の目安　　; U11の12 V出力モデルはメーカー資料で263～438 kHzのスイッチング。この成分と高調波、負荷変化による遅い変動を対象にする。
      | ノイズの発生源　　　; U11内部の降圧スイッチングがバッテリー側から電流を脈動的に取り出すため。バッテリーまでの配線インダクタンスも局所的な電圧変動を生む。
      | 他のコンデンサとの差; 本品群は2.2 µF×5個の入力側容量。C45/C46は12 V出力側で別ノード。5個が最小必要数、またはこの構成だけで電磁ノイズ規格を満たすとは確認していない。
      | 周波数説明の範囲　　; 狙うノイズの周波数と、この部品が実装後に有効な周波数範囲は別である。実効容量、等価直列抵抗、等価直列インダクタンス、配線を含む自己共振で変わるため、型番名や公称容量だけから有効帯域の上限を断定しない。
      | 周波数説明の根拠　　; TRACO POWER：TSR 1WI datasheet
      | https://www.tracopower.com/tsr1wi-datasheet
      | 村田製作所：コンデンサを使いこなす
      | https://www.murata.com/en-GB/products/emc/emifil/library/knowhow/basic/chapter06-p8
      | TDK：電解コンデンサからMLCCへの置換ガイド
      | https://product.tdk.com/en/techlibrary/solutionguide/mlcc_replace-guide.html
      | 
      | 【この説明欄の略語・記号】
      | 用語1　　　　　　　 ; MLCC：Multilayer Ceramic Capacitor（積層セラミックコンデンサ）。薄いセラミック誘電体と電極を重ねたコンデンサ。対象周波数は容量・実装・寄生成分で変わるため、MLCCという分類だけでは決めない。
      | 用語2　　　　　　　 ; ESR：Equivalent Series Resistance（等価直列抵抗）。コンデンサの損失を直列抵抗で表した量。周波数・温度で変わり、損失とリプル電圧に関係する。
      | 用語3　　　　　　　 ; ESL：Equivalent Series Inductance（等価直列インダクタンス）。端子や電極などの寄生インダクタンスを表す。高い周波数ではバイパス効果を制限する。
      | 用語4　　　　　　　 ; DC：Direct Current（直流）。ここでは直流電源または直流成分。DCバイアスはコンデンサに重なる直流電圧を指す。
      | 用語5　　　　　　　 ; X7R：セラミックコンデンサの温度特性記号。英語の頭文字ではなく分類コード。X＝下限−55 ℃、7＝上限+125 ℃、R＝その範囲の容量変化±15%。直流バイアスによる容量変化は別に確認する。
      | 用語6　　　　　　　 ; IC：Integrated Circuit（集積回路）。複数の電子素子と機能を小さな半導体チップに集積した部品。
      | 用語7　　　　　　　 ; EMC：Electromagnetic Compatibility（電磁両立性）。他の機器を電磁ノイズで妨害せず、外来ノイズでも必要な動作を保てる性質。
      | 用語8　　　　　　　 ; GND：Ground（回路の基準電位・電流帰路）。この図の共通基準。保護接地や大地への接続を意味するとは限らない。
      settings: AttributesFormatString=|
      | MLCC
      | 2.2 µF
  C41 : fl_lib/Electrical/Electrical Elements/Capacitor  Description=|  c=2.2e-06 F  r=1e-6 Ohm  g=0 1/Ohm  i_specify=off  i_priority=None  i=0 A  i_nominal_specify=off  i_nominal_value=1  i_nominal_unit=A  v_specify=off  v_priority=None  v=0 V  v_nominal_specify=off  v_nominal_value=1  v_nominal_unit=V  vc_specify=off  vc_priority=High  vc=0 V  vc_nominal_specify=off  vc_nominal_value=1  vc_nominal_unit=V
      | この回路での名前　　; C41
      | 部品名　　　　　　　; C1210X225K1RACAUTO
      | この回路での役割　　; バッテリーから12 Vを作る補助電源U11の入力を支え、電流の脈動を近くで受け止めるためのコンデンサ。
      | ここでの動き　　　　; U11へ入るバッテリー側電源BAT_AUXと共通GNDの間に、2.2 µFを5個並列に置いて入力電荷を補う。5個が必要最小数かどうかはまだ確定していない。
      | 
      | 【詳しい働き・仕様・接続・確認の範囲】
      | 部品種別　　　　　　; 積層セラミックコンデンサ（MLCC）
      | 部品分類　　　　　　; 積層セラミックコンデンサ（MLCC）
      | 公称値　　　　　　　; 2.2uF 100V X7R
      | 配置目的　　　　　　; 12V補助電源入力バイパス群。対象ICはU11（TSR 1-48120WI）。
      | 意図する動作　　　　; U11入力端子付近で給電の瞬間的変動を抑える。現構成は2.2 µF×5個=公称11 µF。5個が最小必要数という根拠は未確認であり、実効容量・入力フィルタ・EMCと合わせた削減評価が残る。
      | 端子と接続　　　　　; 1 1 → BAT_AUX、2 2 → GND
      | モデルの範囲　　　　; Simscape標準コンデンサの集中定数表現。材質、DCバイアス、周波数依存ESR/ESL、寿命・温度特性を型番から自動再現するモデルではない。
      | モデル設定　　　　　; c=2.2 µF、r=1 µΩ、g=0 S。これらは保存モデルの設定値であり、すべてが実部品の保証値という意味ではない。
      | 損失の扱い　　　　　; 保存モデルの直列抵抗rと実部品の周波数・温度依存ESRは区別する。容量値が一致しても損失・リプル電流・寿命の成立確認にはならない。
      | 確認の範囲　　　　　; 本説明は保存回路の部品情報・端子割当・既存設計意図を整理したもの。今回の説明更新によって新たな動作試験や実機検証を実施した意味ではない。
      | 設計記録　　　　　　; evaluation\component_annotations_20261022_r01\before_graph.json
      | evaluation\component_annotations_20261022_r01\before_metadata.json
      | evaluation\protection_capacitor_integration_20261021_r01\final_delivery\independent_readback\physical_bom.json
      | evaluation\protection_capacitor_integration_20261021_r01\capacitor_review\capacitor_inventory_after_c04.json
      | evaluation\layout_readability_20261022_r01\capacitor_review\exact_snapshot_capacitor_review.json
      | 
      | 【周波数・ノイズと配置の説明】
      | 周波数面の役割　　　; 12 V補助電源U11の入力端子近くで、入力電流の脈動に必要な電荷を供給する。
      | 対象周波数の目安　　; U11の12 V出力モデルはメーカー資料で263～438 kHzのスイッチング。この成分と高調波、負荷変化による遅い変動を対象にする。
      | ノイズの発生源　　　; U11内部の降圧スイッチングがバッテリー側から電流を脈動的に取り出すため。バッテリーまでの配線インダクタンスも局所的な電圧変動を生む。
      | 他のコンデンサとの差; 本品群は2.2 µF×5個の入力側容量。C45/C46は12 V出力側で別ノード。5個が最小必要数、またはこの構成だけで電磁ノイズ規格を満たすとは確認していない。
      | 周波数説明の範囲　　; 狙うノイズの周波数と、この部品が実装後に有効な周波数範囲は別である。実効容量、等価直列抵抗、等価直列インダクタンス、配線を含む自己共振で変わるため、型番名や公称容量だけから有効帯域の上限を断定しない。
      | 周波数説明の根拠　　; TRACO POWER：TSR 1WI datasheet
      | https://www.tracopower.com/tsr1wi-datasheet
      | 村田製作所：コンデンサを使いこなす
      | https://www.murata.com/en-GB/products/emc/emifil/library/knowhow/basic/chapter06-p8
      | TDK：電解コンデンサからMLCCへの置換ガイド
      | https://product.tdk.com/en/techlibrary/solutionguide/mlcc_replace-guide.html
      | 
      | 【この説明欄の略語・記号】
      | 用語1　　　　　　　 ; MLCC：Multilayer Ceramic Capacitor（積層セラミックコンデンサ）。薄いセラミック誘電体と電極を重ねたコンデンサ。対象周波数は容量・実装・寄生成分で変わるため、MLCCという分類だけでは決めない。
      | 用語2　　　　　　　 ; ESR：Equivalent Series Resistance（等価直列抵抗）。コンデンサの損失を直列抵抗で表した量。周波数・温度で変わり、損失とリプル電圧に関係する。
      | 用語3　　　　　　　 ; ESL：Equivalent Series Inductance（等価直列インダクタンス）。端子や電極などの寄生インダクタンスを表す。高い周波数ではバイパス効果を制限する。
      | 用語4　　　　　　　 ; DC：Direct Current（直流）。ここでは直流電源または直流成分。DCバイアスはコンデンサに重なる直流電圧を指す。
      | 用語5　　　　　　　 ; X7R：セラミックコンデンサの温度特性記号。英語の頭文字ではなく分類コード。X＝下限−55 ℃、7＝上限+125 ℃、R＝その範囲の容量変化±15%。直流バイアスによる容量変化は別に確認する。
      | 用語6　　　　　　　 ; IC：Integrated Circuit（集積回路）。複数の電子素子と機能を小さな半導体チップに集積した部品。
      | 用語7　　　　　　　 ; EMC：Electromagnetic Compatibility（電磁両立性）。他の機器を電磁ノイズで妨害せず、外来ノイズでも必要な動作を保てる性質。
      | 用語8　　　　　　　 ; GND：Ground（回路の基準電位・電流帰路）。この図の共通基準。保護接地や大地への接続を意味するとは限らない。
      settings: AttributesFormatString=|
      | MLCC
      | 2.2 µF
  C42 : fl_lib/Electrical/Electrical Elements/Capacitor  Description=|  c=2.2e-06 F  r=1e-6 Ohm  g=0 1/Ohm  i_specify=off  i_priority=None  i=0 A  i_nominal_specify=off  i_nominal_value=1  i_nominal_unit=A  v_specify=off  v_priority=None  v=0 V  v_nominal_specify=off  v_nominal_value=1  v_nominal_unit=V  vc_specify=off  vc_priority=High  vc=0 V  vc_nominal_specify=off  vc_nominal_value=1  vc_nominal_unit=V
      | この回路での名前　　; C42
      | 部品名　　　　　　　; C1210X225K1RACAUTO
      | この回路での役割　　; バッテリーから12 Vを作る補助電源U11の入力を支え、電流の脈動を近くで受け止めるためのコンデンサ。
      | ここでの動き　　　　; U11へ入るバッテリー側電源BAT_AUXと共通GNDの間に、2.2 µFを5個並列に置いて入力電荷を補う。5個が必要最小数かどうかはまだ確定していない。
      | 
      | 【詳しい働き・仕様・接続・確認の範囲】
      | 部品種別　　　　　　; 積層セラミックコンデンサ（MLCC）
      | 部品分類　　　　　　; 積層セラミックコンデンサ（MLCC）
      | 公称値　　　　　　　; 2.2uF 100V X7R
      | 配置目的　　　　　　; 12V補助電源入力バイパス群。対象ICはU11（TSR 1-48120WI）。
      | 意図する動作　　　　; U11入力端子付近で給電の瞬間的変動を抑える。現構成は2.2 µF×5個=公称11 µF。5個が最小必要数という根拠は未確認であり、実効容量・入力フィルタ・EMCと合わせた削減評価が残る。
      | 端子と接続　　　　　; 1 1 → BAT_AUX、2 2 → GND
      | モデルの範囲　　　　; Simscape標準コンデンサの集中定数表現。材質、DCバイアス、周波数依存ESR/ESL、寿命・温度特性を型番から自動再現するモデルではない。
      | モデル設定　　　　　; c=2.2 µF、r=1 µΩ、g=0 S。これらは保存モデルの設定値であり、すべてが実部品の保証値という意味ではない。
      | 損失の扱い　　　　　; 保存モデルの直列抵抗rと実部品の周波数・温度依存ESRは区別する。容量値が一致しても損失・リプル電流・寿命の成立確認にはならない。
      | 確認の範囲　　　　　; 本説明は保存回路の部品情報・端子割当・既存設計意図を整理したもの。今回の説明更新によって新たな動作試験や実機検証を実施した意味ではない。
      | 設計記録　　　　　　; evaluation\component_annotations_20261022_r01\before_graph.json
      | evaluation\component_annotations_20261022_r01\before_metadata.json
      | evaluation\protection_capacitor_integration_20261021_r01\final_delivery\independent_readback\physical_bom.json
      | evaluation\protection_capacitor_integration_20261021_r01\capacitor_review\capacitor_inventory_after_c04.json
      | evaluation\layout_readability_20261022_r01\capacitor_review\exact_snapshot_capacitor_review.json
      | 
      | 【周波数・ノイズと配置の説明】
      | 周波数面の役割　　　; 12 V補助電源U11の入力端子近くで、入力電流の脈動に必要な電荷を供給する。
      | 対象周波数の目安　　; U11の12 V出力モデルはメーカー資料で263～438 kHzのスイッチング。この成分と高調波、負荷変化による遅い変動を対象にする。
      | ノイズの発生源　　　; U11内部の降圧スイッチングがバッテリー側から電流を脈動的に取り出すため。バッテリーまでの配線インダクタンスも局所的な電圧変動を生む。
      | 他のコンデンサとの差; 本品群は2.2 µF×5個の入力側容量。C45/C46は12 V出力側で別ノード。5個が最小必要数、またはこの構成だけで電磁ノイズ規格を満たすとは確認していない。
      | 周波数説明の範囲　　; 狙うノイズの周波数と、この部品が実装後に有効な周波数範囲は別である。実効容量、等価直列抵抗、等価直列インダクタンス、配線を含む自己共振で変わるため、型番名や公称容量だけから有効帯域の上限を断定しない。
      | 周波数説明の根拠　　; TRACO POWER：TSR 1WI datasheet
      | https://www.tracopower.com/tsr1wi-datasheet
      | 村田製作所：コンデンサを使いこなす
      | https://www.murata.com/en-GB/products/emc/emifil/library/knowhow/basic/chapter06-p8
      | TDK：電解コンデンサからMLCCへの置換ガイド
      | https://product.tdk.com/en/techlibrary/solutionguide/mlcc_replace-guide.html
      | 
      | 【この説明欄の略語・記号】
      | 用語1　　　　　　　 ; MLCC：Multilayer Ceramic Capacitor（積層セラミックコンデンサ）。薄いセラミック誘電体と電極を重ねたコンデンサ。対象周波数は容量・実装・寄生成分で変わるため、MLCCという分類だけでは決めない。
      | 用語2　　　　　　　 ; ESR：Equivalent Series Resistance（等価直列抵抗）。コンデンサの損失を直列抵抗で表した量。周波数・温度で変わり、損失とリプル電圧に関係する。
      | 用語3　　　　　　　 ; ESL：Equivalent Series Inductance（等価直列インダクタンス）。端子や電極などの寄生インダクタンスを表す。高い周波数ではバイパス効果を制限する。
      | 用語4　　　　　　　 ; DC：Direct Current（直流）。ここでは直流電源または直流成分。DCバイアスはコンデンサに重なる直流電圧を指す。
      | 用語5　　　　　　　 ; X7R：セラミックコンデンサの温度特性記号。英語の頭文字ではなく分類コード。X＝下限−55 ℃、7＝上限+125 ℃、R＝その範囲の容量変化±15%。直流バイアスによる容量変化は別に確認する。
      | 用語6　　　　　　　 ; IC：Integrated Circuit（集積回路）。複数の電子素子と機能を小さな半導体チップに集積した部品。
      | 用語7　　　　　　　 ; EMC：Electromagnetic Compatibility（電磁両立性）。他の機器を電磁ノイズで妨害せず、外来ノイズでも必要な動作を保てる性質。
      | 用語8　　　　　　　 ; GND：Ground（回路の基準電位・電流帰路）。この図の共通基準。保護接地や大地への接続を意味するとは限らない。
      settings: AttributesFormatString=|
      | MLCC
      | 2.2 µF
  C43 : fl_lib/Electrical/Electrical Elements/Capacitor  Description=|  c=2.2e-06 F  r=1e-6 Ohm  g=0 1/Ohm  i_specify=off  i_priority=None  i=0 A  i_nominal_specify=off  i_nominal_value=1  i_nominal_unit=A  v_specify=off  v_priority=None  v=0 V  v_nominal_specify=off  v_nominal_value=1  v_nominal_unit=V  vc_specify=off  vc_priority=High  vc=0 V  vc_nominal_specify=off  vc_nominal_value=1  vc_nominal_unit=V
      | この回路での名前　　; C43
      | 部品名　　　　　　　; C1210X225K1RACAUTO
      | この回路での役割　　; バッテリーから12 Vを作る補助電源U11の入力を支え、電流の脈動を近くで受け止めるためのコンデンサ。
      | ここでの動き　　　　; U11へ入るバッテリー側電源BAT_AUXと共通GNDの間に、2.2 µFを5個並列に置いて入力電荷を補う。5個が必要最小数かどうかはまだ確定していない。
      | 
      | 【詳しい働き・仕様・接続・確認の範囲】
      | 部品種別　　　　　　; 積層セラミックコンデンサ（MLCC）
      | 部品分類　　　　　　; 積層セラミックコンデンサ（MLCC）
      | 公称値　　　　　　　; 2.2uF 100V X7R
      | 配置目的　　　　　　; 12V補助電源入力バイパス群。対象ICはU11（TSR 1-48120WI）。
      | 意図する動作　　　　; U11入力端子付近で給電の瞬間的変動を抑える。現構成は2.2 µF×5個=公称11 µF。5個が最小必要数という根拠は未確認であり、実効容量・入力フィルタ・EMCと合わせた削減評価が残る。
      | 端子と接続　　　　　; 1 1 → BAT_AUX、2 2 → GND
      | モデルの範囲　　　　; Simscape標準コンデンサの集中定数表現。材質、DCバイアス、周波数依存ESR/ESL、寿命・温度特性を型番から自動再現するモデルではない。
      | モデル設定　　　　　; c=2.2 µF、r=1 µΩ、g=0 S。これらは保存モデルの設定値であり、すべてが実部品の保証値という意味ではない。
      | 損失の扱い　　　　　; 保存モデルの直列抵抗rと実部品の周波数・温度依存ESRは区別する。容量値が一致しても損失・リプル電流・寿命の成立確認にはならない。
      | 確認の範囲　　　　　; 本説明は保存回路の部品情報・端子割当・既存設計意図を整理したもの。今回の説明更新によって新たな動作試験や実機検証を実施した意味ではない。
      | 設計記録　　　　　　; evaluation\component_annotations_20261022_r01\before_graph.json
      | evaluation\component_annotations_20261022_r01\before_metadata.json
      | evaluation\protection_capacitor_integration_20261021_r01\final_delivery\independent_readback\physical_bom.json
      | evaluation\protection_capacitor_integration_20261021_r01\capacitor_review\capacitor_inventory_after_c04.json
      | evaluation\layout_readability_20261022_r01\capacitor_review\exact_snapshot_capacitor_review.json
      | 
      | 【周波数・ノイズと配置の説明】
      | 周波数面の役割　　　; 12 V補助電源U11の入力端子近くで、入力電流の脈動に必要な電荷を供給する。
      | 対象周波数の目安　　; U11の12 V出力モデルはメーカー資料で263～438 kHzのスイッチング。この成分と高調波、負荷変化による遅い変動を対象にする。
      | ノイズの発生源　　　; U11内部の降圧スイッチングがバッテリー側から電流を脈動的に取り出すため。バッテリーまでの配線インダクタンスも局所的な電圧変動を生む。
      | 他のコンデンサとの差; 本品群は2.2 µF×5個の入力側容量。C45/C46は12 V出力側で別ノード。5個が最小必要数、またはこの構成だけで電磁ノイズ規格を満たすとは確認していない。
      | 周波数説明の範囲　　; 狙うノイズの周波数と、この部品が実装後に有効な周波数範囲は別である。実効容量、等価直列抵抗、等価直列インダクタンス、配線を含む自己共振で変わるため、型番名や公称容量だけから有効帯域の上限を断定しない。
      | 周波数説明の根拠　　; TRACO POWER：TSR 1WI datasheet
      | https://www.tracopower.com/tsr1wi-datasheet
      | 村田製作所：コンデンサを使いこなす
      | https://www.murata.com/en-GB/products/emc/emifil/library/knowhow/basic/chapter06-p8
      | TDK：電解コンデンサからMLCCへの置換ガイド
      | https://product.tdk.com/en/techlibrary/solutionguide/mlcc_replace-guide.html
      | 
      | 【この説明欄の略語・記号】
      | 用語1　　　　　　　 ; MLCC：Multilayer Ceramic Capacitor（積層セラミックコンデンサ）。薄いセラミック誘電体と電極を重ねたコンデンサ。対象周波数は容量・実装・寄生成分で変わるため、MLCCという分類だけでは決めない。
      | 用語2　　　　　　　 ; ESR：Equivalent Series Resistance（等価直列抵抗）。コンデンサの損失を直列抵抗で表した量。周波数・温度で変わり、損失とリプル電圧に関係する。
      | 用語3　　　　　　　 ; ESL：Equivalent Series Inductance（等価直列インダクタンス）。端子や電極などの寄生インダクタンスを表す。高い周波数ではバイパス効果を制限する。
      | 用語4　　　　　　　 ; DC：Direct Current（直流）。ここでは直流電源または直流成分。DCバイアスはコンデンサに重なる直流電圧を指す。
      | 用語5　　　　　　　 ; X7R：セラミックコンデンサの温度特性記号。英語の頭文字ではなく分類コード。X＝下限−55 ℃、7＝上限+125 ℃、R＝その範囲の容量変化±15%。直流バイアスによる容量変化は別に確認する。
      | 用語6　　　　　　　 ; IC：Integrated Circuit（集積回路）。複数の電子素子と機能を小さな半導体チップに集積した部品。
      | 用語7　　　　　　　 ; EMC：Electromagnetic Compatibility（電磁両立性）。他の機器を電磁ノイズで妨害せず、外来ノイズでも必要な動作を保てる性質。
      | 用語8　　　　　　　 ; GND：Ground（回路の基準電位・電流帰路）。この図の共通基準。保護接地や大地への接続を意味するとは限らない。
      settings: AttributesFormatString=|
      | MLCC
      | 2.2 µF
  C44 : fl_lib/Electrical/Electrical Elements/Capacitor  Description=|  c=2.2e-06 F  r=1e-6 Ohm  g=0 1/Ohm  i_specify=off  i_priority=None  i=0 A  i_nominal_specify=off  i_nominal_value=1  i_nominal_unit=A  v_specify=off  v_priority=None  v=0 V  v_nominal_specify=off  v_nominal_value=1  v_nominal_unit=V  vc_specify=off  vc_priority=High  vc=0 V  vc_nominal_specify=off  vc_nominal_value=1  vc_nominal_unit=V
      | この回路での名前　　; C44
      | 部品名　　　　　　　; C1210X225K1RACAUTO
      | この回路での役割　　; バッテリーから12 Vを作る補助電源U11の入力を支え、電流の脈動を近くで受け止めるためのコンデンサ。
      | ここでの動き　　　　; U11へ入るバッテリー側電源BAT_AUXと共通GNDの間に、2.2 µFを5個並列に置いて入力電荷を補う。5個が必要最小数かどうかはまだ確定していない。
      | 
      | 【詳しい働き・仕様・接続・確認の範囲】
      | 部品種別　　　　　　; 積層セラミックコンデンサ（MLCC）
      | 部品分類　　　　　　; 積層セラミックコンデンサ（MLCC）
      | 公称値　　　　　　　; 2.2uF 100V X7R
      | 配置目的　　　　　　; 12V補助電源入力バイパス群。対象ICはU11（TSR 1-48120WI）。
      | 意図する動作　　　　; U11入力端子付近で給電の瞬間的変動を抑える。現構成は2.2 µF×5個=公称11 µF。5個が最小必要数という根拠は未確認であり、実効容量・入力フィルタ・EMCと合わせた削減評価が残る。
      | 端子と接続　　　　　; 1 1 → BAT_AUX、2 2 → GND
      | モデルの範囲　　　　; Simscape標準コンデンサの集中定数表現。材質、DCバイアス、周波数依存ESR/ESL、寿命・温度特性を型番から自動再現するモデルではない。
      | モデル設定　　　　　; c=2.2 µF、r=1 µΩ、g=0 S。これらは保存モデルの設定値であり、すべてが実部品の保証値という意味ではない。
      | 損失の扱い　　　　　; 保存モデルの直列抵抗rと実部品の周波数・温度依存ESRは区別する。容量値が一致しても損失・リプル電流・寿命の成立確認にはならない。
      | 確認の範囲　　　　　; 本説明は保存回路の部品情報・端子割当・既存設計意図を整理したもの。今回の説明更新によって新たな動作試験や実機検証を実施した意味ではない。
      | 設計記録　　　　　　; evaluation\component_annotations_20261022_r01\before_graph.json
      | evaluation\component_annotations_20261022_r01\before_metadata.json
      | evaluation\protection_capacitor_integration_20261021_r01\final_delivery\independent_readback\physical_bom.json
      | evaluation\protection_capacitor_integration_20261021_r01\capacitor_review\capacitor_inventory_after_c04.json
      | evaluation\layout_readability_20261022_r01\capacitor_review\exact_snapshot_capacitor_review.json
      | 
      | 【周波数・ノイズと配置の説明】
      | 周波数面の役割　　　; 12 V補助電源U11の入力端子近くで、入力電流の脈動に必要な電荷を供給する。
      | 対象周波数の目安　　; U11の12 V出力モデルはメーカー資料で263～438 kHzのスイッチング。この成分と高調波、負荷変化による遅い変動を対象にする。
      | ノイズの発生源　　　; U11内部の降圧スイッチングがバッテリー側から電流を脈動的に取り出すため。バッテリーまでの配線インダクタンスも局所的な電圧変動を生む。
      | 他のコンデンサとの差; 本品群は2.2 µF×5個の入力側容量。C45/C46は12 V出力側で別ノード。5個が最小必要数、またはこの構成だけで電磁ノイズ規格を満たすとは確認していない。
      | 周波数説明の範囲　　; 狙うノイズの周波数と、この部品が実装後に有効な周波数範囲は別である。実効容量、等価直列抵抗、等価直列インダクタンス、配線を含む自己共振で変わるため、型番名や公称容量だけから有効帯域の上限を断定しない。
      | 周波数説明の根拠　　; TRACO POWER：TSR 1WI datasheet
      | https://www.tracopower.com/tsr1wi-datasheet
      | 村田製作所：コンデンサを使いこなす
      | https://www.murata.com/en-GB/products/emc/emifil/library/knowhow/basic/chapter06-p8
      | TDK：電解コンデンサからMLCCへの置換ガイド
      | https://product.tdk.com/en/techlibrary/solutionguide/mlcc_replace-guide.html
      | 
      | 【この説明欄の略語・記号】
      | 用語1　　　　　　　 ; MLCC：Multilayer Ceramic Capacitor（積層セラミックコンデンサ）。薄いセラミック誘電体と電極を重ねたコンデンサ。対象周波数は容量・実装・寄生成分で変わるため、MLCCという分類だけでは決めない。
      | 用語2　　　　　　　 ; ESR：Equivalent Series Resistance（等価直列抵抗）。コンデンサの損失を直列抵抗で表した量。周波数・温度で変わり、損失とリプル電圧に関係する。
      | 用語3　　　　　　　 ; ESL：Equivalent Series Inductance（等価直列インダクタンス）。端子や電極などの寄生インダクタンスを表す。高い周波数ではバイパス効果を制限する。
      | 用語4　　　　　　　 ; DC：Direct Current（直流）。ここでは直流電源または直流成分。DCバイアスはコンデンサに重なる直流電圧を指す。
      | 用語5　　　　　　　 ; X7R：セラミックコンデンサの温度特性記号。英語の頭文字ではなく分類コード。X＝下限−55 ℃、7＝上限+125 ℃、R＝その範囲の容量変化±15%。直流バイアスによる容量変化は別に確認する。
      | 用語6　　　　　　　 ; IC：Integrated Circuit（集積回路）。複数の電子素子と機能を小さな半導体チップに集積した部品。
      | 用語7　　　　　　　 ; EMC：Electromagnetic Compatibility（電磁両立性）。他の機器を電磁ノイズで妨害せず、外来ノイズでも必要な動作を保てる性質。
      | 用語8　　　　　　　 ; GND：Ground（回路の基準電位・電流帰路）。この図の共通基準。保護接地や大地への接続を意味するとは限らない。
      settings: AttributesFormatString=|
      | MLCC
      | 2.2 µF
  C45 : fl_lib/Electrical/Electrical Elements/Capacitor  Description=|  c=2.2e-05 F  r=1e-6 Ohm  g=0 1/Ohm  i_specify=off  i_priority=None  i=0 A  i_nominal_specify=off  i_nominal_value=1  i_nominal_unit=A  v_specify=off  v_priority=None  v=0 V  v_nominal_specify=off  v_nominal_value=1  v_nominal_unit=V  vc_specify=off  vc_priority=High  vc=0 V  vc_nominal_specify=off  vc_nominal_value=1  vc_nominal_unit=V
      | この回路での名前　　; C45
      | 部品名　　　　　　　; GRM32ER71E226KE15L
      | この回路での役割　　; 補助電源U11が作る12 Vの細かな変動を抑え、下流へ給電しやすくするためのコンデンサ。
      | ここでの動き　　　　; U11の出力P12と共通GNDの間に22 µFを置き、電源変換の脈動や負荷電流の変化を出力端子の近くで受け止める。大きな電荷を蓄えるC46と併用する設計。
      | 
      | 【詳しい働き・仕様・接続・確認の範囲】
      | 部品種別　　　　　　; 積層セラミックコンデンサ（MLCC）
      | 部品分類　　　　　　; 積層セラミックコンデンサ（MLCC）
      | 公称値　　　　　　　; 22uF 25V X7R
      | 配置目的　　　　　　; 12Vレギュレータ出力局所バイパス。対象ICはU11（TSR 1-48120WI）。
      | 意図する動作　　　　; U11出力ピン直近、C46との役割を区別。 メーカーの10µF X7R条件と同じ機能。22µF公称の12V実効値は別に確認し、C46削除候補でも残す。
      | 端子と接続　　　　　; 1 1 → P12、2 2 → GND
      | モデルの範囲　　　　; Simscape標準コンデンサの集中定数表現。材質、DCバイアス、周波数依存ESR/ESL、寿命・温度特性を型番から自動再現するモデルではない。
      | モデル設定　　　　　; c=22 µF、r=1 µΩ、g=0 S。これらは保存モデルの設定値であり、すべてが実部品の保証値という意味ではない。
      | 損失の扱い　　　　　; 保存モデルの直列抵抗rと実部品の周波数・温度依存ESRは区別する。容量値が一致しても損失・リプル電流・寿命の成立確認にはならない。
      | 確認の範囲　　　　　; 本説明は保存回路の部品情報・端子割当・既存設計意図を整理したもの。今回の説明更新によって新たな動作試験や実機検証を実施した意味ではない。
      | 設計記録　　　　　　; evaluation\component_annotations_20261022_r01\before_graph.json
      | evaluation\component_annotations_20261022_r01\before_metadata.json
      | evaluation\protection_capacitor_integration_20261021_r01\final_delivery\independent_readback\physical_bom.json
      | evaluation\protection_capacitor_integration_20261021_r01\capacitor_review\capacitor_inventory_after_c04.json
      | evaluation\layout_readability_20261022_r01\capacitor_review\exact_snapshot_capacitor_review.json
      | 
      | 【周波数・ノイズと配置の説明】
      | 周波数面の役割　　　; U11の12 V出力端子近くでリプルと負荷変化を受け止める局所容量。
      | 対象周波数の目安　　; U11の263～438 kHzの変換成分とその高調波、下流の負荷変動を対象とする。
      | ノイズの発生源　　　; U11内部のスイッチングと、U10・U12・低側ゲートドライバU9が12 Vから取り出す電流の変化。
      | 他のコンデンサとの差; C46の470 µFハイブリッド電解より容量は小さい22 µFのMLCC。大きな電荷蓄積と高速帰路の分担を狙うが、周波数の境界や分流は未測定。
      | 周波数説明の範囲　　; 狙うノイズの周波数と、この部品が実装後に有効な周波数範囲は別である。実効容量、等価直列抵抗、等価直列インダクタンス、配線を含む自己共振で変わるため、型番名や公称容量だけから有効帯域の上限を断定しない。
      | 周波数説明の根拠　　; TRACO POWER：TSR 1WI datasheet
      | https://www.tracopower.com/tsr1wi-datasheet
      | 村田製作所：コンデンサのインピーダンス・ESRと周波数の関係
      | https://article.murata.com/en-global/article/impedance-esr-frequency-characteristics-in-capacitors
      | 村田製作所：コンデンサを使いこなす
      | https://www.murata.com/en-GB/products/emc/emifil/library/knowhow/basic/chapter06-p8
      | 
      | 【この説明欄の略語・記号】
      | 用語1　　　　　　　 ; MLCC：Multilayer Ceramic Capacitor（積層セラミックコンデンサ）。薄いセラミック誘電体と電極を重ねたコンデンサ。対象周波数は容量・実装・寄生成分で変わるため、MLCCという分類だけでは決めない。
      | 用語2　　　　　　　 ; ESR：Equivalent Series Resistance（等価直列抵抗）。コンデンサの損失を直列抵抗で表した量。周波数・温度で変わり、損失とリプル電圧に関係する。
      | 用語3　　　　　　　 ; ESL：Equivalent Series Inductance（等価直列インダクタンス）。端子や電極などの寄生インダクタンスを表す。高い周波数ではバイパス効果を制限する。
      | 用語4　　　　　　　 ; DC：Direct Current（直流）。ここでは直流電源または直流成分。DCバイアスはコンデンサに重なる直流電圧を指す。
      | 用語5　　　　　　　 ; X7R：セラミックコンデンサの温度特性記号。英語の頭文字ではなく分類コード。X＝下限−55 ℃、7＝上限+125 ℃、R＝その範囲の容量変化±15%。直流バイアスによる容量変化は別に確認する。
      | 用語6　　　　　　　 ; IC：Integrated Circuit（集積回路）。複数の電子素子と機能を小さな半導体チップに集積した部品。
      | 用語7　　　　　　　 ; GND：Ground（回路の基準電位・電流帰路）。この図の共通基準。保護接地や大地への接続を意味するとは限らない。
      settings: AttributesFormatString=|
      | MLCC
      | 22 µF
  C46 : fl_lib/Electrical/Electrical Elements/Capacitor  Description=|  c=0.00047 F  r=1e-6 Ohm  g=0 1/Ohm  i_specify=off  i_priority=None  i=0 A  i_nominal_specify=off  i_nominal_value=1  i_nominal_unit=A  v_specify=off  v_priority=None  v=0 V  v_nominal_specify=off  v_nominal_value=1  v_nominal_unit=V  vc_specify=off  vc_priority=High  vc=0 V  vc_nominal_specify=off  vc_nominal_value=1  vc_nominal_unit=V
      | この回路での名前　　; C46
      | 部品名　　　　　　　; EEHZK1E471P
      | この回路での役割　　; 共通12 V電源に電荷を多めに蓄え、接続された回路の消費電流が増えたときに補うためのコンデンサ。
      | ここでの動き　　　　; 12 V電源P12と共通GNDの間に470 µFを置き、起動や負荷の切替えに伴う変動を受け止める。以前のリレー負荷から引き継いだ容量であり、現回路での必要最小値は未確定。
      | 
      | 【詳しい働き・仕様・接続・確認の範囲】
      | 部品種別　　　　　　; ハイブリッド電解コンデンサ（有極性）
      | 部品分類　　　　　　; ハイブリッド電解コンデンサ（有極性）
      | 公称値　　　　　　　; 470uF 25V hybrid
      | 配置目的　　　　　　; 共通12Vバルク/過渡蓄積。対象ICはU11（TSR 1-48120WI）。
      | 意図する動作　　　　; P12の瞬間的な負荷変動へ電荷を供給する。旧K1コイル負荷から継承された470 µFで、現回路での必要最小容量は未確定。起動・負荷変動・保持時間の比較が残る。
      | 端子と接続　　　　　; 1 1 → P12、2 2 → GND
